simulink model "Controller_torque_cbf_m22"  (R2022b)
settings: Solver=ode4  StartTime=0.0  StopTime=Inf  FixedStep=1e-3  RelTol=1e-3
values from neighbouring files (symbols this model uses):
  Dn = 20 * ones(7,1)    [init_torque_cbf.m]
  H_0_cy = H_0_pr * H_pr_cy    [init_torque_cbf.m]
  H_home = getTransform(Franka_robot, q_home, 'panda_link8', 'panda_link0')    [init_torque_cbf.m]
  Kn = 0 * ones(7,1)    [init_torque_cbf.m]
  q_home = q_init    [init_torque_cbf.m]
  q_init = [0 0  0  -(2/4)*pi  0  pi/2  -pi/4]'    [init_torque_cbf.m]
undefined symbols (not defined in the file or in its folder): cbf_torque_params, DiscIntNeverNeededParam, Fext_mag, T_final, X, Y, Z
libraries: sm_lib x162, nesl_utility x44, matrix_library x3, Robotics_lib x1
(part 11 of 12)

== matlab function Controller_torque_cbf_m22/Dynamic Parameters/Coriolis Matrix1 ==
  data: q_state input; C output; q_state_dot input
function C = Franka_CoriolisMatrix(q_state, q_state_dot)
% Author: TU Wien, ACIN Robotics group
% Optimized and generated from Maple
  C = zeros(7,7);

  t1877 = q_state(2);
  t1856 = sin(t1877);
  t3747 = 0.1e1 * t1856;
  t1878 = q_state(1);
  t1864 = cos(t1878);
  t2794 = 0.1225946e1 * t1864;
  t1875 = q_state(4);
  t1861 = cos(t1875);
  t1801 = 0.345563e0 * t1861;
  t1874 = q_state(5);
  t1853 = sin(t1874);
  t1860 = cos(t1874);
  t2249 = 0.41065e-1 * t1853 + 0.11953e-1 * t1860;
  t1522 = t2249 + 0.825e-1;
  t1854 = sin(t1875);
  t3244 = t1522 * t1854;
  t1128 = t1801 - t3244;
  t1101 = 0.316e0 + t1128;
  t1863 = cos(t1877);
  t2864 = 0.41065e-1 * t1860;
  t1538 = 0.11953e-1 * t1853 - t2864;
  t1876 = q_state(3);
  t1855 = sin(t1876);
  t1370 = t1538 * t1855;
  t1797 = 0.345563e0 * t1854;
  t2889 = -t1797 + 0.825e-1;
  t3243 = t1522 * t1861;
  t1104 = -t3243 + t2889;
  t1862 = cos(t1876);
  t3688 = t1104 * t1862;
  t3541 = t3688 + t1370;
  t3413 = t1856 * t3541;
  t604 = -t1101 * t1863 + t3413;
  t3746 = t2794 * t604;
  t1857 = sin(t1878);
  t1873 = q_state(6);
  t1852 = sin(t1873);
  t1859 = cos(t1873);
  t1312 = 0.60149000000000000000e-1 * t1859 + 0.14117000000000000000e-1 * t1852;
  t1010 = -t1312 * t1853 - 0.10517000000000000000e-1 * t1860;
  t1537 = 0.60149e-1 * t1852 - 0.14117e-1 * t1859;
  t1520 = t1537 + 0.384e0;
  t1329 = t1520 * t1854;
  t3484 = 0.825e-1 - t1329;
  t1541 = 0.60149e-1 * t1859 + 0.14117e-1 * t1852;
  t1809 = 0.10517e-1 * t1853;
  t2802 = -t1541 * t1860 + t1809;
  t3647 = t2802 + 0.825e-1;
  t3678 = t3647 * t1861;
  t847 = -t3678 + t3484;
  t3731 = t847 * t1862;
  t577 = t1010 * t1855 + t3731;
  t3745 = t1857 * t577;
  t1872 = q_state(7);
  t1858 = cos(t1872);
  t2521 = 0.12763550042100000000e-2 * t1858;
  t1851 = sin(t1872);
  t2596 = 0.51602752476000000000e-3 * t1851;
  t3101 = -t2596 - t2521;
  t2339 = -0.27219646194675000000e-1 + t3101;
  t2578 = 0.48418875570424600020e-2 * t1851;
  t1377 = 0.55042935974400000000e-3 + t2578;
  t2589 = 0.13614453378240000000e-2 * t1851;
  t1410 = 0.5826996021941340000e-3 - t2589;
  t1844 = t1858 ^ 2;
  t1622 = 0.15804348732630079999e-2 * t1844;
  t2146 = t1622 - t1410;
  t888 = t1377 * t1858 - t2146;
  t685 = t1853 * t888 - t2339;
  t3397 = t685 * t1852;
  t658 = t685 * t1859;
  t2866 = 0.10517e-1 * t1860;
  t2331 = t1541 * t1853 + t2866;
  t3627 = t2331 * t1855;
  t3637 = -t3731 + t3627;
  t3744 = t1856 * t3637;
  t3628 = t1863 * t3637;
  t1845 = t1859 ^ 2;
  t2577 = 0.66899306471351120000e-2 * t1851;
  t3094 = -0.21934364256329279998e-2 * t1858 - t2577;
  t1201 = t3094 * t1845;
  t2582 = 0.33449653235675560000e-2 * t1851;
  t3096 = -0.10967182128164639999e-2 * t1858 - t2582;
  t2101 = t1201 - t3096;
  t1646 = 0.59408523832320000000e-2 * t1851;
  t1729 = 0.24018735697920000000e-2 * t1858;
  t1283 = t1646 - t1729;
  t2587 = 0.15804348732630079999e-2 * t1851;
  t1383 = -0.27228906756480000000e-2 + t2587;
  t2524 = 0.11008587194880000000e-2 * t1858;
  t2576 = 0.96837751140849200040e-2 * t1851;
  t3136 = t1858 * t2576 - t1622;
  t826 = t1383 * t1851 + t2524 + t3136;
  t3718 = t1852 * t826 - t1283;
  t3398 = t1859 * t3718;
  t3743 = (t2101 - t3398) * t1860;
  t1846 = t1860 ^ 2;
  t2603 = 0.24890000000000000000e-2 * t1844;
  t3212 = t1851 * t1858;
  t2104 = t2603 + 0.85600000000000000000e-3 * t3212;
  t1041 = 0.27050000000000000000e-2 - t2104;
  t1040 = t2104 + 0.28220000000000000000e-2;
  t3353 = t1040 * t1845;
  t2282 = -t3353 + t1041;
  t2588 = 0.14820000000000000000e-2 * t1851;
  t1384 = -0.21800000000000000000e-3 + t2588;
  t1730 = 0.23920000000000000000e-2 * t1858;
  t1142 = t1384 - t1730;
  t3208 = t1852 * t1859;
  t3002 = t1142 * t3208;
  t560 = t3002 - t2282;
  t3401 = t560 * t1846;
  t3604 = t2603 + 0.85599999999999999997e-3 * t3212;
  t1042 = 0.28220000000000000000e-2 + t3604;
  t2382 = 0.17120000000000000000e-2 * t3212;
  t2601 = 0.49780000000000000000e-2 * t1844;
  t2102 = t2382 + t2601;
  t2346 = 0.33106000000000000000e-1 - t2102;
  t2007 = -t3002 - t2346;
  t562 = -t1042 * t1845 + t2007;
  t3570 = t562 - t3401;
  t3732 = t1855 * t847;
  t3736 = t1010 * t1862 - t3732;
  t3742 = t1864 * t3736;
  t3153 = t1864 * t1863;
  t3741 = t3153 * t3736;
  t3168 = t1860 * t1853;
  t3075 = -0.2e1 * t3168;
  t3739 = t3075 * t560;
  t3197 = t1854 * t1862;
  t2987 = t1853 * t3197;
  t2772 = t1860 * t2987;
  t3738 = t560 * t2772;
  t3193 = t1855 * t1854;
  t3010 = t1846 * t3193;
  t3737 = t560 * t3010;
  t3375 = t888 * t1859;
  t680 = -t1853 * t2339 + t888;
  t1620 = 0.17120000000000000000e-2 * t1844;
  t1837 = t1851 ^ 2;
  t2379 = 0.99560000000000000000e-2 * t3212;
  t2107 = 0.17120000000000000000e-2 * t1837 + t2379;
  t2898 = t1620 - t2107;
  t2520 = 0.14820000000000000000e-2 * t1858;
  t2585 = 0.23920000000000000000e-2 * t1851;
  t1308 = t2520 + t2585;
  t2998 = t1308 * t3208;
  t2754 = -t2998 + t2898;
  t1445 = 0.49780000000000000000e-2 * t3212;
  t994 = -t1445 - 0.85599999999999999997e-3 * t1837 + 0.85599999999999999997e-3 * t1844;
  t2330 = -t1845 * t994 + t2754;
  t1476 = t1852 * t1730;
  t1096 = t1852 * t2588 - t1476;
  t2106 = 0.49780000000000000000e-2 * t1837 - 0.34240000000000000000e-2 * t3212;
  t997 = -t2106 + t2601;
  t3638 = t1859 * t997 + t1096;
  t2605 = 0.85600000000000000000e-3 * t1844;
  t999 = -t1445 - 0.85600000000000000000e-3 * t1837 + t2605;
  t3366 = t999 * t1845;
  t548 = t999 + t2998 + t3366;
  t3700 = t548 * t1846;
  t3427 = -t3168 * t3638 - t3700;
  t3735 = -t3427 - t2330;
  t1162 = -t3096 + 0.18713819462921000000e-3;
  t3311 = t1162 * t1859;
  t1407 = 0.4841887557042460002e-2 * t1851 + 0.55042935974400000000e-3;
  t890 = -t1407 * t1858 + t2146;
  t3733 = -t1852 * t890 + t3311;
  t3726 = t826 * t1845;
  t991 = 0.15804348732630079999e-2 * t1837 + t3136;
  t3578 = t3726 + t991;
  t1657 = 0.12763550042100000000e-2 * t1851;
  t1311 = -t1657 + 0.51602752476000000000e-3 * t1858;
  t2336 = 0.11198654185125000000e-1 + t1311;
  t1056 = t2336 * t1853;
  t1700 = 0.11357396418885000000e-1 * t1852;
  t1393 = t1700 - 0.24178658687700000000e-2;
  t3305 = t2339 * t1859;
  t899 = t1393 - t3305;
  t859 = t899 * t1860;
  t3730 = t859 - t1056;
  t2328 = t1857 * t3541;
  t820 = t1863 * t3541;
  t3706 = t1329 + t3678;
  t3729 = t3706 * t1856;
  t1286 = 0.10967182128164640000e-2 * t1858 + t2582;
  t1192 = 0.187138194629210e-3 + t1286;
  t2579 = 0.48418875570424600000e-2 * t1851;
  t1378 = 0.55042935974400000000e-3 + t2579;
  t3257 = t1378 * t1858;
  t1621 = 0.15804348732630080000e-2 * t1844;
  t3705 = t1410 - t1621;
  t889 = t3257 + t3705;
  t3727 = t1852 * t889;
  t3728 = t1192 * t1859 + t3727;
  t1161 = t1286 + 0.18713819462921000000e-3;
  t3314 = t1161 * t1852;
  t3725 = t889 * t1859;
  t628 = t3725 - t3314 - 0.54375110533459400000e-2;
  t3480 = t3314 + 0.5437511053345940e-2;
  t633 = t3725 - t3480;
  t2592 = 0.79021743663150400000e-3 * t1851;
  t1385 = -0.13614453378240000000e-2 + t2592;
  t1734 = 0.55042935974400000000e-3 * t1858;
  t1447 = t1858 * t2579;
  t1623 = 0.79021743663150400000e-3 * t1844;
  t3130 = -t1447 + t1623;
  t2903 = t1734 - t3130;
  t828 = t1385 * t1851 + t2903;
  t779 = t828 * t1852;
  t2103 = t1445 - t1620;
  t1044 = 0.14600000000000000000e-2 - t2103;
  t3724 = t1044 * t1852;
  t3723 = t1044 * t1859;
  t3162 = t1861 * t1862;
  t1260 = t1538 * t3162;
  t2199 = t2249 * t1855;
  t2157 = t1260 + t2199;
  t3722 = t1856 * t2157;
  t3671 = -t1520 * t1861 + t1854 * t3647;
  t3721 = t1863 * t3671;
  t3720 = t3671 * t1856;
  t1648 = 0.29704261916160000000e-2 * t1851;
  t1379 = t1648 - 0.23898270415101870000e-1;
  t2522 = 0.12009367848960000000e-2 * t1858;
  t1160 = t2522 - t1379;
  t2532 = 0.54835910640823200000e-3 * t1858;
  t2586 = 0.16724826617837780000e-2 * t1851;
  t3097 = -t2586 - t2532;
  t1185 = -t3097 + 0.9356909731460500000e-4;
  t1089 = t1185 * t1859;
  t1380 = 0.24209437785212300000e-2 * t1851 + 0.27521467987200000000e-3;
  t1263 = t1380 * t1858;
  t1663 = 0.68072266891200000000e-3 * t1851;
  t1403 = 0.29134980109706700000e-3 - t1663;
  t882 = t1623 - t1403 - t1263;
  t3698 = t882 * t1852;
  t3707 = -t1089 + t3698;
  t2091 = t1160 - t3707;
  t1534 = -t2588 + 0.21800e-3;
  t1248 = t1730 + t1534;
  t2999 = t1248 * t3208;
  t575 = t2282 + t2999;
  t1658 = 0.12009367848960000000e-2 * t1851;
  t1727 = 0.29704261916160000000e-2 * t1858;
  t1295 = t1658 + t1727;
  t2518 = 0.15804348732630080000e-2 * t1858;
  t1449 = t1851 * t2518;
  t1617 = 0.24209437785212300000e-2 * t1844;
  t2530 = 0.68072266891200000000e-3 * t1858;
  t2135 = t2530 - t1617;
  t3256 = t1380 * t1851;
  t830 = t1449 - t3256 - t2135;
  t3699 = t830 * t1852;
  t2848 = t1295 - t3699;
  t1732 = 0.16724826617837780000e-2 * t1858;
  t2595 = 0.54835910640823200000e-3 * t1851;
  t3100 = -t2595 + t1732;
  t3269 = t3100 * t1859;
  t3596 = t2848 - t3269;
  t2863 = 0.61597e-1 * t1860;
  t1562 = t1852 * t2863;
  t2887 = 0.4252e-2 * t1851;
  t1544 = 0.10517e-1 * t1858 + t2887;
  t1524 = t1544 + 0.88e-1;
  t3173 = t1859 * t1860;
  t3031 = t1524 * t3173;
  t3116 = -t1562 - t3031;
  t1543 = 0.10517e-1 * t1851 - 0.4252e-2 * t1858;
  t3230 = t1543 * t1853;
  t844 = -0.825e-1 + t3230 - t3116;
  t3385 = t844 * t1854;
  t3241 = t1524 * t1852;
  t2867 = 0.61597e-1 * t1859;
  t3646 = 0.384e0 - t2867;
  t3620 = t3241 + t3646;
  t3682 = t3620 * t1861;
  t3719 = t3682 + t3385;
  t1660 = 0.10967182128164640000e-2 * t1851;
  t2512 = 0.33449653235675560000e-2 * t1858;
  t2127 = t2512 - t1660;
  t1154 = t2127 + 0.11022068765350630000e-1;
  t3166 = t1860 * t1861;
  t1598 = 0.13297872941088000000e-4 * t1837;
  t1733 = 0.13614453378240000000e-2 * t1858;
  t1664 = 0.55042935974400000000e-3 * t1851;
  t2465 = t1664 + 0.69751885789075550000e-2;
  t2258 = t1733 + 0.81354094419858e-4 * t1844 + t2465;
  t911 = t1598 + t2258;
  t609 = t1154 * t3166 - t1854 * t911;
  t3036 = t1286 * t3208;
  t3358 = t1845 * t828 - t3036;
  t1376 = 0.11008587194880000000e-2 + t2576;
  t1270 = t1376 * t1858;
  t1615 = 0.31608697465260159998e-2 * t1844;
  t1650 = 0.27228906756480000000e-2 * t1851;
  t3108 = t1615 + t1650;
  t881 = t3108 - t1270 - 0.11653992043882680000e-2;
  t3377 = t881 * t1859;
  t3717 = t3377 + 0.10875022106691880000e-1;
  t1085 = t2339 * t1852;
  t3716 = 0.1e1 * t1085;
  t3715 = 0.1e1 * t3162;
  t3714 = 0.1e1 * t3723;
  t3713 = t1852 * t881;
  t2885 = 0.5317e-1 * t1854;
  t1790 = -0.316e0 + t2885;
  t2837 = 0.104419e0 * t1861;
  t2845 = 0.104419e0 * t1854;
  t2248 = 0.5317e-1 * t1861 + t2845;
  t1523 = t2248 - 0.825e-1;
  t2870 = 0.27454e-1 * t1855;
  t1134 = t1523 * t1862 - t2870;
  t3635 = t1134 * t1863;
  t824 = t3635 + t1856 * (t1790 - t2837);
  t3712 = t1857 * t824;
  t3711 = t1864 * t824;
  t3384 = t844 * t1861;
  t2048 = t2867 - t3241;
  t2014 = 0.384e0 - t2048;
  t3710 = t1854 * t2014;
  t3709 = t1863 * t3682;
  t3237 = t1538 * t1862;
  t3689 = t1104 * t1855;
  t2652 = t3237 - t3689;
  t2326 = t2652 * t1864;
  t1088 = t1185 * t1852;
  t3696 = t882 * t1859;
  t3708 = -t1088 - t3696;
  t1194 = t1286 * t1845;
  t2806 = -t3097 - t1194;
  t1302 = -t1648 + t2522;
  t668 = t1302 + t779;
  t480 = t1859 * t668 - t2806;
  t3271 = t3100 * t1852;
  t3575 = t1859 * t830;
  t3567 = t3271 - t3575;
  t1303 = -0.41065000000000000000e-1 * t1860 + 0.11953000000000000000e-1 * t1853;
  t787 = t1303 * t1855 + t3688;
  t2381 = 0.24890000000000000000e-2 * t3212;
  t2105 = t2381 - t2605;
  t3642 = t2105 - 0.73000000000000000000e-3;
  t3355 = t3642 * t1852;
  t3704 = 0.22900e-3 - t3355;
  t1832 = 0.316e0 * t1856;
  t3703 = t1856 * t3682 + t1832;
  t3702 = 0.1e1 * t3698;
  t1736 = 0.25801376238000000000e-3 * t1858;
  t2594 = 0.63817750210500000000e-3 * t1851;
  t3099 = t1736 - t2594;
  t1197 = t3099 * t1854;
  t3701 = 0.1e1 * t1197;
  t3379 = t1860 * t882;
  t1503 = t1859 * t2520;
  t1532 = 0.68200e-3 + t2585;
  t3123 = t1532 * t1859 + t1503;
  t725 = t3123 - t3724;
  t688 = t725 * t3168;
  t3381 = t882 * t1853;
  t3697 = t882 * t1855;
  t3695 = t882 * t1862;
  t3169 = t1860 * t1852;
  t3694 = t882 * t3169;
  t3172 = t1859 * t1861;
  t3693 = t882 * t3172;
  t3207 = t1852 * t1861;
  t3692 = t882 * t3207;
  t1806 = 0.61597e-1 * t1852;
  t1554 = t1853 * t1806;
  t3229 = t1543 * t1860;
  t3140 = t3229 - t1554;
  t3202 = t1853 * t1859;
  t2441 = -t1524 * t3202 + t3140;
  t3662 = t2441 * t1855;
  t1280 = 0.10517000000000000000e-1 * t1851 - 0.42520000000000000000e-2 * t1858;
  t1202 = t1280 * t1853;
  t1306 = 0.10517000000000000000e-1 * t1858 + 0.42520000000000000000e-2 * t1851;
  t1173 = t1306 + 0.88000000000000000000e-1;
  t3046 = t1173 * t3173;
  t3150 = -t3046 - t1202;
  t2333 = 0.82500000000000000000e-1 + t3150;
  t2265 = -t1562 + t2333;
  t663 = t2265 * t1861;
  t1082 = t1173 * t1852;
  t2466 = t1082 + 0.38400000000000000000e0;
  t918 = -t2867 + t2466;
  t879 = t918 * t1854;
  t871 = -0.825e-1 + t879;
  t469 = t663 + t871;
  t377 = t1862 * t469 - t3662;
  t2737 = t1082 + t3646;
  t482 = t1854 * t2737 + t663 - 0.825e-1;
  t384 = t1862 * t482 - t3662;
  t3157 = t1863 * t1862;
  t3687 = t1128 * t3157;
  t3183 = t1856 * t1862;
  t3686 = t1128 * t3183;
  t3260 = t1311 * t1852;
  t1035 = t1854 * t3620;
  t2591 = 0.98827089590400000000e-3 * t1851;
  t1404 = -0.52129746651620000000e-1 - t2591;
  t2515 = 0.24444132201840000000e-2 * t1858;
  t3615 = t1404 - t2515;
  t3649 = -0.56786982094425000000e-2 * t1860 + t3615;
  t3685 = t1854 * t3649;
  t3194 = t1855 * t1853;
  t3191 = t1855 * t1860;
  t3240 = t1524 * t1859;
  t3516 = t1806 + t3240;
  t1972 = t1853 * t3516 - t3229;
  t3684 = t1972 * t1855;
  t3683 = t1972 * t1862;
  t3187 = t1856 * t1854;
  t3681 = t3620 * t3187;
  t3679 = t3642 * t1859;
  t1843 = t1857 ^ 2;
  t1850 = t1864 ^ 2;
  t3515 = t1850 + t1843;
  t2529 = 0.74100000000000000000e-3 * t1858;
  t2590 = 0.11960000000000000000e-2 * t1851;
  t2132 = t2529 + t2590;
  t3677 = -t3208 * t999 - t2132;
  t1596 = 0.81354094419858000000e-4 * t1837;
  t1838 = t1852 ^ 2;
  t1607 = 0.11947109539798930000e-2 * t1838;
  t3608 = t1607 - t1596;
  t2344 = 0.25565950283854690000e-2 + t3608;
  t1451 = t1858 * t2592;
  t3526 = t1451 + 0.25022978729410880000e-2 * t1844;
  t858 = t2344 - t3526;
  t2598 = 0.25801376238000000000e-3 * t1851;
  t1402 = 0.13609823097337500000e-1 + t2598;
  t2531 = 0.63817750210500000000e-3 * t1858;
  t2340 = -t2531 - t1402;
  t2583 = 0.31608697465260159998e-2 * t1851;
  t1448 = t1858 * t2583;
  t3134 = t1448 - t1733;
  t3676 = -0.4841887557042460002e-2 * t1844 - t3134;
  t1611 = 0.48418875570424600020e-2 * t1844;
  t2439 = -t1377 * t1851 + t1611 + t3134;
  t1540 = 0.39252e-1 * t1862 + 0.27518e-1 * t1855;
  t3236 = t1540 * t1857;
  t2247 = 0.39252e-1 * t1855 - 0.27518e-1 * t1862;
  t3583 = -t1863 * t2247 + 0.249498e0 * t1856;
  t3346 = t3583 * t1864;
  t3675 = -t3236 + t3346;
  t1156 = 0.47796540830203740000e-1 - t1283;
  t1065 = t1156 * t1853;
  t2467 = t1065 + 0.27752814537092170000e0;
  t965 = -t1162 * t1853 + 0.11357396418885000000e-1;
  t3409 = t1859 * t965;
  t3674 = t3409 - t2467;
  t3661 = t2441 * t1862;
  t383 = t1855 * t482 + t3661;
  t376 = t1855 * t469 + t3661;
  t3673 = (-0.1e1 * t2605 + t2381) * t1862;
  t3672 = -0.1e1 * t1850 - 0.1e1 * t1843;
  t2593 = 0.79021743663150399997e-3 * t1851;
  t1386 = -0.13614453378240000000e-2 + t2593;
  t3035 = t3096 * t3208;
  t1446 = t1858 * t2578;
  t1624 = 0.79021743663150399997e-3 * t1844;
  t3135 = t1446 - t1624;
  t3362 = -(t1386 * t1851 + t1734 + t3135) * t1845 - t3035;
  t2345 = -0.48082828567067140000e-2 - t3608;
  t3670 = 0.1e1 * t2898;
  t3669 = t1861 - 0.1e1;
  t2511 = 0.47840000000000000000e-2 * t1858;
  t2584 = 0.29640000000000000000e-2 * t1851;
  t2125 = t2511 - t2584;
  t1247 = t2125 + 0.43600e-3;
  t1125 = t1247 * t1845;
  t1530 = -0.829200e-2 + t2588;
  t1045 = t2102 + 0.5644000000000000000e-2;
  t3003 = t1045 * t3208;
  t631 = t1530 - t1730 + t1125 + t3003;
  t3668 = t631 * t1853;
  t3666 = t965 * t1852;
  t3091 = -0.60149000000000000000e-1 * t1852 + 0.14117000000000000000e-1 * t1859;
  t2335 = -0.38400000000000000000e0 + t3091;
  t1208 = t1312 * t1860;
  t2562 = 0.10517000000000000000e-1 * t1853;
  t2229 = t2562 - t1208;
  t2348 = -0.82500000000000000000e-1 - t2229;
  t673 = t1854 * t2335 + t1861 * t2348 + 0.825e-1;
  t519 = t1862 * t673 - t3627;
  t2736 = -0.384e0 + t3091;
  t971 = -0.825e-1 - t2229;
  t3369 = t971 * t1861;
  t718 = t1854 * t2736 + t3369 + 0.825e-1;
  t540 = t1862 * t718 - t3627;
  t3190 = t1855 * t1861;
  t3007 = t1846 * t3190;
  t3343 = t1855 * t2802;
  t3665 = t1856 * t2248;
  t1390 = -t1658 - 0.63347540234880000000e-1;
  t3616 = t1390 - t1727;
  t3664 = t1860 * t3616;
  t3663 = t2048 * t3194;
  t2170 = 0.56786982094425000000e-2 * t1852 - 0.12089329343850000000e-2;
  t3248 = t2170 * t1854;
  t2198 = t2249 * t1862;
  t2470 = 0.16143020000000000000e1 * t1864;
  t3585 = t1856 * t2247 + 0.249498e0 * t1863;
  t3660 = t2470 * t3585;
  t1839 = t1853 ^ 2;
  t2611 = 0.79021743663150400000e-3 * t1837;
  t2306 = -t1623 + t2611;
  t993 = t1447 + t2306;
  t3498 = -t1845 * t993 + t3036;
  t3659 = t3498 * t1839;
  t3658 = (t1543 * t1855 + t3162 * t3516) * t1853;
  t3560 = t3583 * t1857;
  t937 = t3585 * t1857;
  t3001 = t1154 * t3208;
  t2722 = t858 + t3001;
  t1619 = 0.24076459055801420000e-2 * t1844;
  t3113 = t1598 - t1619;
  t3251 = t1385 * t1858;
  t801 = -t3251 + t2465 + t3113;
  t3598 = t1845 * t801 + t2722;
  t3657 = t3598 * t1853;
  t1652 = 0.24444132201840000000e-2 * t1851;
  t2527 = 0.98827089590400000000e-3 * t1858;
  t3600 = -t2527 + t1652;
  t2088 = t3600 * t1854;
  t3137 = t3600 * t1855;
  t3281 = t3600 * t1861;
  t1198 = t3099 * t1861;
  t3655 = -t1198 + t1311;
  t1300 = t2531 + t2598;
  t490 = t993 + t3358;
  t3654 = t1853 * t490 + t1300;
  t1482 = 0.23894219079597860000e-2 * t3208;
  t3222 = t1845 * t1154;
  t3228 = t1838 * t1154;
  t2815 = t3222 - t3228;
  t2679 = -t1482 - t2815;
  t1381 = 0.68200000000000000000e-3 + t2585;
  t3255 = t1381 * t1859;
  t3653 = t1503 + t3255;
  t1369 = -0.24972970685027959000e-1 - t1596;
  t1788 = 0.13297872941088e-4 * t1844;
  t1132 = t1788 - t1369;
  t1189 = 0.11022068765350630e-1 + t2127;
  t1699 = 0.26431758938496000000e-1 * t1852;
  t3650 = t1189 * t1845 - 0.4484246605646421e-2 - t1699 - t3100;
  t3626 = t2331 * t1862;
  t541 = t1855 * t718 + t3626;
  t520 = t1855 * t673 + t3626;
  t3648 = -0.1e1 * t1837 + t1844;
  t1477 = t1852 * t2520;
  t3239 = t1532 * t1852;
  t3126 = -t1477 - t3239;
  t3645 = t3126 - 0.15700e-2;
  t3204 = t1853 * t1852;
  t2377 = 0.17120000000000000000e-2 * t3204;
  t1337 = t1844 * t2377;
  t2375 = 0.49780000000000000000e-2 * t3204;
  t3144 = -t2375 * t3212 + t1337;
  t3644 = 0.155920e-1 - t3144;
  t1046 = t2102 - 0.5410000000000000000e-2;
  t3643 = 0.13611244295754000000e-3 * t1851;
  t2503 = 0.52863517876992000000e-1 * t1859;
  t1157 = 0.44842466056464210000e-2 + t3100;
  t1075 = t1157 * t1861;
  t2556 = 0.12089329343850000000e-2 * t1854;
  t3088 = -t2556 - t1075;
  t897 = -0.46305794820080000000e-2 - t3088;
  t1293 = -t1730 + t2588;
  t1176 = 0.82920000000000000000e-2 - t1293;
  t2341 = -0.21447119530300000000e-1 + t3600;
  t3641 = -0.2e1 * t1860;
  t3639 = t631 * t1860;
  t3636 = t1134 * t1856;
  t2385 = t1858 * t3643;
  t3634 = t1854 * t3516;
  t3192 = t1855 * t1859;
  t3633 = t1855 * t3516;
  t2056 = t1856 * t2802;
  t1662 = 0.74100000000000000000e-3 * t1851;
  t2523 = 0.11960000000000000000e-2 * t1858;
  t2131 = -t2523 + t1662;
  t3630 = t1859 * t2131;
  t3160 = t1863 * t1854;
  t3625 = t2331 * t3160;
  t3624 = t2331 * t3162;
  t3041 = t2331 * t3187;
  t1526 = 0.825e-1 - t1562;
  t707 = t1526 + t3150;
  t3408 = t1861 * t707;
  t3622 = (t871 + t3408) * t1862;
  t1661 = 0.10967182128164639999e-2 * t1851;
  t2612 = -t2512 - 0.8968493211292842000e-2;
  t1186 = t1661 + t2612;
  t1697 = 0.52863517876992000000e-1 * t1852;
  t3621 = t1186 - t1697;
  t1653 = 0.24018735697920000000e-2 * t1851;
  t1725 = 0.59408523832320000000e-2 * t1858;
  t1289 = t1653 + t1725;
  t2128 = t2512 - t1661;
  t3619 = -t1859 * t2128 + t1289;
  t1822 = 0.27454e-1 * t1862;
  t1559 = t1857 * t1822;
  t2485 = 0.53170000000000000000e-1 * t1861;
  t3181 = t1857 * t1855;
  t3618 = t2485 * t3181 + t1559;
  t2550 = 0.82500000000000000000e-1 * t1854;
  t1399 = 0.38400000000000000000e0 - t2550;
  t2747 = 0.7735484874e-2 * t1858;
  t3617 = -t1399 * t2747 + t1390;
  t1450 = t1858 * t2587;
  t3614 = -t1450 - t1611;
  t3613 = 0.81354094419858e-4 * t1837 - t3001 + t3526 - 0.25565950283854690000e-2;
  t1153 = t2128 + 0.11022068765350630000e-1;
  t1021 = t1153 * t3208;
  t1452 = t1858 * t2593;
  t3612 = -t1452 - 0.25022978729410880010e-2 * t1844 + t1021;
  t3611 = t1452 + 0.24209437785212300010e-2 * t1844;
  t3610 = -t3724 + t3653;
  t2477 = 0.53170000000000000000e-1 * t1864;
  t2890 = 0.825e-1 * t1864;
  t3609 = t1862 * t2890 - t2477 * t3162;
  t3102 = t1664 + t1733;
  t1612 = 0.48418875570424600000e-2 * t1844;
  t3607 = t1733 - t1612;
  t1777 = 0.12089329343850000000e-2 * t1861;
  t2554 = 0.46305794820080000000e-2 * t1854;
  t3606 = -t1777 - t2554;
  t1272 = t1402 * t1854;
  t1396 = -0.31600000000000000000e0 + t2550;
  t2040 = -t1396 * t2747 - t1404;
  t3605 = t2040 - t1272;
  t3128 = -0.96837751140849200000e-2 * t3212 + t1621;
  t2471 = 0.83327750000000000000e0 * t1864;
  t2537 = 0.83327750000000000000e0 * t1857;
  t594 = -t3626 - t3732;
  t3412 = t1857 * t594;
  t3184 = t1856 * t1861;
  t3146 = t1520 * t3184 + t1832;
  t2911 = -t3187 * t3647 + t3146;
  t421 = t2911 - t3628;
  t294 = t1864 * t421 + t3412;
  t3406 = t1864 * t594;
  t422 = -t1832 + t3628 + t3720;
  t297 = t1857 * t422 + t3406;
  t3603 = t2471 * t297 + t2537 * t294;
  t1588 = t1855 * t2890;
  t3180 = t1857 * t1856;
  t2251 = -t3662 + t3622;
  t357 = t2251 * t1857;
  t3156 = t1864 * t1855;
  t502 = t3156 * t707 - t3180 * t3620;
  t3395 = t707 * t1854;
  t664 = -0.316e0 + t3395;
  t169 = t664 * t3180 + t1861 * t502 + t1863 * t357 - t1588 + (t3193 * t918 + t3661) * t1864;
  t2895 = 0.825e-1 * t1855;
  t1582 = t1857 * t2895;
  t2985 = t1854 * t3181;
  t3155 = t1864 * t1856;
  t2888 = 0.825e-1 - t1035;
  t3047 = t1173 * t3202;
  t748 = -t3047 + t3140;
  t730 = t748 * t1855;
  t2733 = t1862 * t2888 + t3162 * t844 + t730;
  t395 = t2733 * t1864;
  t568 = t3155 * t3620 - t3181 * t844;
  t3179 = t1857 * t1862;
  t714 = t748 * t3179;
  t770 = 0.316e0 + t3385;
  t181 = t1861 * t568 + t1863 * t395 + t2985 * t3620 + t3155 * t770 - t1582 + t714;
  t2475 = 0.36776100000000000000e0 * t1864;
  t2541 = 0.36776100000000000000e0 * t1857;
  t3602 = t169 * t2475 + t181 * t2541;
  t1002 = -t1162 + 0.11357396418885000000e-1 * t1853;
  t2566 = 0.24178658687700000000e-2 * t1853;
  t823 = -t2566 + t1002 * t1852 - 0.13248221105898140000e-1;
  t3098 = -t2589 + t1734;
  t1301 = -t2591 - t2515;
  t2749 = 0.7735484874e-2 * t1851;
  t3599 = t1396 * t2749 + t2527;
  t1834 = 0.316e0 * t1863;
  t2833 = 0.345563e0 * t1863;
  t3117 = t1861 * t2833 + t1834;
  t1971 = t1860 * t3516 + t3230;
  t1966 = 0.825e-1 - t1971;
  t1938 = t1854 * t1966 - t1861 * t2014;
  t2876 = -0.735522e0 * t1834 + 0.735522e0 * t1938 * t1863 + 0.735522e0 * (-t3684 + (0.825e-1 - t3710 + (-0.825e-1 + t1971) * t1861) * t1862) * t1856;
  t3506 = t3515 * t2876;
  t3323 = t1153 * t1845;
  t2812 = t1153 * t1838 - t3323;
  t3597 = t2812 - t1482;
  t2508 = 0.66899306471351120000e-2 * t1858;
  t1290 = 0.21934364256329279998e-2 * t1851 - t2508;
  t1150 = -t1290 + 0.22044137530701260000e-1;
  t3326 = t1150 * t1845;
  t3593 = t3326 - t1697;
  t3333 = t1142 * t1845;
  t3494 = t1142 * t1838 - t3333;
  t1776 = 0.46305794820080000000e-2 * t1861;
  t3592 = t1776 - 0.44842466056464210000e-2 - t2556;
  t3591 = -t1797 - 0.1e1 * t3243;
  t3590 = t3673 * t1853;
  t3221 = t1845 * t1853;
  t3354 = t1040 * t1838;
  t3589 = t1040 * t3221 - 0.1e1 * t1853 * t3354;
  t3588 = -0.1e1 * t971 * t1854 + t2736 * t1861;
  t3090 = -0.41065000000000000000e-1 * t1853 - 0.11953000000000000000e-1 * t1860;
  t2738 = -0.825e-1 + t3090;
  t3587 = -0.1e1 * t2738 * t1854 - 0.1e1 * t1801;
  t2894 = 0.825e-1 * t1861;
  t1792 = 0.825e-1 - t2894;
  t2210 = 0.41065e-1 * t3162 - 0.11953e-1 * t1855;
  t2842 = 0.345563e0 * t1856;
  t2693 = t1862 * t2842;
  t2727 = 0.11953e-1 * t3162;
  t2892 = 0.825e-1 * t1863;
  t2741 = t1854 * t2892;
  t3185 = t1856 * t1860;
  t3186 = t1856 * t1855;
  t3203 = t1853 * t1856;
  t418 = -t1792 * t3183 + t1854 * t2693 + t2210 * t3203 - t2249 * t3160 + t2727 * t3185 + t2864 * t3186 - t2741 + t3117;
  t3487 = 0.1225946e1 * t3672 * t418;
  t276 = -t1834 + t3721 - t3744;
  t3486 = 0.1666555e1 * t3672 * t276;
  t3586 = t1450 + 0.16270818883971600000e-3 * t1837 - 0.23894219079597860000e-2 * t1838;
  t2803 = t1523 * t1855 + t1822;
  t2417 = t1134 * t1857 + t2803 * t3153;
  t2413 = t1543 * t3173 - t1544 * t1853;
  t3209 = t1852 * t1854;
  t3022 = t1543 * t3209;
  t3584 = t1861 * t2413 - t3022;
  t3581 = 0.9457555763200000000e-3 - t1451;
  t1539 = -t2837 + t2885;
  t3023 = t1539 * t3157;
  t3580 = (-0.1e1 * t3665 + t3023) * t1864 - 0.1e1 * t1539 * t3181;
  t3463 = 0.2e1 * t1852;
  t3579 = t1845 / 0.2e1;
  t3312 = t1162 * t1852;
  t2664 = t3312 - t3375;
  t627 = t2664 + 0.54375110533459400000e-2;
  t3577 = t1846 * t627;
  t850 = t1280 * t3173 - t1306 * t1853;
  t3576 = t1854 * t850;
  t2469 = 0.17939475000000000000e1 * t1864;
  t1521 = t1539 - 0.316e0;
  t868 = t1521 * t1863 - t3636;
  t2395 = t868 * t2469;
  t3092 = -t1700 + t3305;
  t900 = 0.24178658687700000000e-2 + t3092;
  t3574 = t900 * t1853;
  t1992 = t997 * t1852;
  t998 = -0.24890000000000000000e-2 * t1837 + t2382 + t2603;
  t3573 = t998 * t1852;
  t3572 = t1648 - t779;
  t3072 = t575 * t3168;
  t2854 = t1477 + 0.42340e-2;
  t996 = t3239 + t2854;
  t716 = t3723 + t996;
  t696 = t716 * t1846;
  t3571 = -t3072 + t696;
  t976 = t1088 + 0.6624110552949070e-2;
  t3569 = t1846 * t633 + t976;
  t1166 = -0.12669508046976000000e0 - t1289;
  t1656 = 0.15804348732630080000e-2 * t1851;
  t1382 = t1656 - 0.27228906756480000000e-2;
  t1597 = 0.26595745882176000000e-4 * t1837;
  t1659 = 0.11008587194880000000e-2 * t1851;
  t3110 = -t1597 - t1659;
  t796 = 0.48152918111602840000e-2 * t1844 + t1382 * t1858 - 0.11560955249855324000e-1 + t3110;
  t636 = t1852 * t796 + t1166;
  t3568 = t1859 * t636 - t1697;
  t2373 = t1852 * t2529;
  t3562 = t3679 - t2373;
  t3084 = t1839 - t1846;
  t3561 = t1044 * t3084;
  t1716 = 0.56786982094425000000e-2 * t1854;
  t2461 = t1716 - 0.21751134959804000000e-1;
  t2486 = 0.26431758938496000000e-1 * t1861;
  t1168 = t2486 - t2461;
  t3559 = t1168 * t1852;
  t2147 = t1524 * t1854;
  t2883 = 0.4252e-2 * t1860;
  t3557 = t1851 * (t1809 * t1859 + t2883);
  t2862 = 0.14117e-1 * t1861;
  t2873 = 0.60149e-1 * t1854;
  t3556 = t1852 * (t1860 * t2873 - t2862);
  t3199 = t1854 * t1853;
  t3555 = t1855 * t2248;
  t2886 = 0.4252e-2 * t1853;
  t3554 = t1858 * (t1859 * t2886 - t2866);
  t3174 = t1859 * t1854;
  t2861 = 0.60149e-1 * t1861;
  t2874 = 0.14117e-1 * t1854;
  t3553 = t1859 * (t1860 * t2874 + t2861);
  t1987 = t1851 * (t1859 * t2866 - t2886) - t1858 * (t1859 * t2883 + t1809);
  t3552 = t1861 * t1987;
  t2238 = -0.825e-1 + t2485;
  t2117 = t2238 + t2845;
  t3551 = t1862 * t2117;
  t1545 = 0.2872e-1 * t1856 - 0.3141e-2 * t1863;
  t1939 = t1861 * t1966 + t3710;
  t165 = -t1832 + t1938 * t1856 + (t3684 + (-0.825e-1 + t1939) * t1862) * t1863;
  t1870 = q_state_dot(2);
  t2800 = 0.3228604e1 * t3583;
  t2826 = 0.3587895e1 * t1539 * t1856 - 0.3587895e1 * t1832 + 0.3587895e1 * t3635;
  t2041 = t1797 + t3243;
  t2242 = t1128 * t1856;
  t2829 = -0.1225946e1 * t1832 - 0.1225946e1 * t2242 + 0.1225946e1 * (-0.1e1 * t1370 + (-0.825e-1 + t2041) * t1862) * t1863;
  t2831 = -0.1666555e1 * t1832 + 0.1666555e1 * t3720 + 0.1666555e1 * (t3627 + (t3678 - 0.1e1 * t3484) * t1862) * t1863;
  t2834 = 0.104419e0 * t1863;
  t1552 = t1861 * t2834;
  t2881 = 0.5317e-1 * t1863;
  t689 = t1854 * t2881 - t1552 - t1834 - t3636;
  t3550 = (t3585 * t2800 + 0.646926e0 * t1545 * (0.2872e-1 * t1863 + 0.3141e-2 * t1856) + t165 * t2876 + t276 * t2831 + t2826 * t689 - t2829 * t418) * t1870;
  t2067 = t2103 * t1852;
  t2137 = t2170 * t1862;
  t1408 = 0.9356909731460500000e-4 + t2586;
  t2308 = t1408 + t2532;
  t3548 = t2308 * t1859;
  t3167 = t1860 * t1854;
  t3029 = t1537 * t3167;
  t3233 = t1541 * t1861;
  t2414 = t3029 - t3233;
  t3545 = t2414 * t1856;
  t3028 = t1537 * t3166;
  t3235 = t1541 * t1854;
  t2415 = t3028 + t3235;
  t3544 = t2415 * t1862;
  t1049 = t2803 * t1864;
  t3523 = t1699 + t1157;
  t2818 = t3523 - t3222;
  t1145 = t1300 + 0.13609823097337500000e-1;
  t2495 = 0.26431758938496000000e-1 * t1860;
  t1003 = t1145 + t2495;
  t1004 = 0.21751134959804000000e-1 * t1860 + t2340;
  t3542 = t1004 * t1861 + t1003;
  t1057 = t2336 * t1860;
  t3372 = t899 * t1853;
  t3540 = -t1057 - t3372;
  t1060 = t3616 * t1854;
  t3330 = t1145 * t1861;
  t3539 = -t1060 + t3330;
  t1112 = t1311 * t3173;
  t1205 = t3101 * t1853;
  t3538 = t1112 - t1205;
  t1070 = t1145 * t1854;
  t1155 = -t1301 + 0.52129746651620000000e-1;
  t3536 = -t1155 + t1070;
  t1207 = t1302 * t1854;
  t3535 = -t1198 - t1207;
  t2908 = -t1198 + t3099;
  t2570 = 0.61597000000000000000e-1 * t1852;
  t1510 = t1860 * t2570;
  t3534 = t1510 - t3150;
  t3531 = -t1852 * t2439 + t3619;
  t2334 = -0.82500000000000000000e-1 + t3090;
  t952 = t1861 * t2334 + t2889;
  t760 = t1862 * t952 + t1370;
  t1411 = -0.2913498010970670000e-3 + t1663;
  t2641 = 0.7902174366315040000e-3 * t1844;
  t3528 = -t1411 - t2641;
  t3121 = t1393 * t1860;
  t3524 = t1619 + t3251;
  t3104 = 0.25527100084200000000e-2 * t1851 - 0.10320550495200000000e-2 * t1858;
  t1359 = 0.2444413220184e-2 * t1862 - 0.54835910640823200000e-3 * t1855;
  t1771 = 0.11357396418885000000e-1 * t1859;
  t3520 = t1771 + t1085;
  t1782 = 0.21751134959804000000e-1 * t1862;
  t3519 = -t1782 + t3697;
  t1361 = -0.16724826617837780000e-2 * t1862 - 0.988270895904e-3 * t1855;
  t2090 = t1853 * t3091;
  t2255 = t2415 * t1855;
  t3514 = -t1862 * t2090 + t2255;
  t2600 = 0.50045957458821760020e-2 * t1844;
  t2126 = -0.21934364256329279999e-2 * t1851 + t2508;
  t1151 = t2126 + 0.22044137530701260000e-1;
  t3051 = t1151 * t3208;
  t1613 = 0.48152918111602840020e-2 * t1844;
  t3114 = t1597 - t1613;
  t3253 = t1383 * t1858;
  t2753 = t1659 - t3253 + t3114;
  t805 = 0.13950377157815110002e-1 + t2753;
  t3513 = t1845 * t805 - t2600 + t3051 - t3586;
  t2484 = 0.49096519673609460000e-2 * t1862;
  t2350 = t1861 * t2484;
  t2565 = 0.49096519673609460000e-2 * t1853;
  t3512 = t1855 * t2565 - t1860 * t2350;
  t3510 = -0.51131900567709380000e-2 + t3586;
  t3078 = -0.2e1 * t3208;
  t2297 = -t1042 * t3078 + t3494;
  t3005 = t1040 * t3208;
  t935 = 0.2e1 * t3005;
  t2716 = t935 + t3494;
  t3509 = t1846 * t2716 + t2297;
  t3507 = 0.3587895e1 * t3515 * t689;
  t2750 = 0.3127439544e-2 * t1851;
  t3505 = t2747 + t2750;
  t3504 = t3269 / 0.2e1 + t3699 / 0.2e1;
  t1374 = t1544 * t1860;
  t3501 = -t1543 * t3202 - t1374;
  t3500 = t3031 + t3230;
  t3497 = 0.1644487577369270e-2 * t1854 + t3693;
  t2660 = -t1855 * t952 + t3237;
  t1146 = 0.55993270925625000000e-2 + t3099;
  t1059 = t1146 * t1861;
  t3303 = t2341 * t1854;
  t3496 = -t3303 + t1059;
  t3315 = t1160 * t1861;
  t3329 = t1146 * t1854;
  t3495 = t3315 - t3329;
  t1387 = t1662 - 0.41460000000000000000e-2;
  t3493 = t1387 - 0.1e1 * t3333;
  t1388 = -0.55993270925625000000e-2 + t2594;
  t3492 = t1388 - 0.1e1 * t1736;
  t2285 = t1730 - 0.1e1 * t1530;
  t3491 = -0.15637197720000000000e-2 * t1858 + 0.38677424370000000000e-2 * t1851;
  t3490 = t2522 - 0.1e1 * t1379;
  t1847 = t1861 ^ 2;
  t665 = t716 * t3168;
  t284 = t665 + t3570;
  t3000 = t1247 * t3208;
  t3198 = t1854 * t1861;
  t1249 = t1308 + 0.68200e-3;
  t2575 = 0.14600000000000000000e-2 * t1852;
  t1535 = 0.45800e-3 + t2575;
  t2442 = -t1535 * t1853 + t3644;
  t388 = t1249 * t3202 + t2442 + t3639;
  t987 = t1045 * t1845;
  t3489 = -0.1e1 * t3000 + t575 * t1846 + t284 * t1847 + t3198 * t388 + t665 + t987 + 0.31784000000000000000e-1 - t3604;
  t3488 = 0.1e1 * t3732 + t3626;
  t3485 = t1308 * t3221 - t1853 * t2132;
  t3483 = t3573 - t3630;
  t3482 = -t1146 + t3657;
  t2528 = 0.83624133089188900000e-3 * t1858;
  t2597 = 0.27417955320411600000e-3 * t1851;
  t3481 = (t2528 - t2597) * t1859 + 0.50000000000000000000e0 * t3699;
  t2175 = t1623 - 0.1e1 * t1263 - 0.1e1 * t1403;
  t1769 = 0.26431758938496000000e-1 * t1859;
  t3107 = -t1619 + t1664;
  t2259 = 0.57804776249276620000e-2 - t3251 + t3107;
  t802 = t1598 + t2259;
  t757 = t802 * t1845;
  t3361 = t1769 + t757;
  t756 = t802 * t1852;
  t638 = t756 + 0.63347540234880000000e-1 + t1295;
  t2322 = (-t1852 * t638 + 0.2e1 * t3001 + t3361) * t1853;
  t2504 = 0.56786982094425000000e-2 * t1859;
  t3331 = t1145 * t1852;
  t2809 = -t2504 + t3331;
  t3440 = t1860 / 0.2e1;
  t3446 = t1854 / 0.2e1;
  t452 = t3078 * t801 - t2679;
  t3313 = t1161 * t1859;
  t657 = -t3313 - t3727;
  t3479 = ((t1860 * t452 + t2809) * t1853 + t657 * t1846 - t3707) * t3446 + (t2322 / 0.2e1 + t3708 * t3440) * t1861;
  t3478 = t1853 * (0.41065e-1 * t1855 + t2727) - t1860 * t2210;
  t3476 = 0.50000000000000000000e0 * t1860;
  t3475 = 0.50000000000000000000e0 * t3198;
  t3473 = t1729 + 0.47796540830203740000e-1;
  t931 = t3113 + t3581;
  t2246 = t931 * t1845 + t3001 - 0.22516878283212450000e-2;
  t2195 = t2246 * t1839;
  t3471 = t2195 - 0.65338343552314821500e0;
  t1698 = 0.43502269919608000000e-1 * t1852;
  t3468 = 0.92611589640160000000e-2 - t1698;
  t3105 = 0.11881704766464000000e-1 * t1858 + 0.48037471395840000000e-2 * t1851;
  t1179 = -0.25339016093952000000e0 - t3105;
  t3467 = -t1860 * t3483 - t3485;
  t3321 = t1155 * t1852;
  t3466 = -0.1e1 * t3321 - 0.50330438027992300000e0;
  t632 = -0.31476782229750000000e-1 + t3730;
  t2288 = t1736 - 0.1e1 * t1388;
  t1401 = 0.21447119530300000000e-1 - t1652;
  t2310 = t1401 + t2527;
  t3465 = t1854 * t2310 + t1861 * t2288 - t2336;
  t3462 = -0.2e1 * t1859;
  t3461 = -t1295 / 0.2e1;
  t1840 = t1854 ^ 2;
  t3460 = -t1840 / 0.2e1;
  t3459 = t1840 / 0.2e1;
  t1841 = t1855 ^ 2;
  t3458 = -t1841 / 0.2e1;
  t3457 = t1841 / 0.2e1;
  t1842 = t1856 ^ 2;
  t3456 = t1842 / 0.2e1;
  t3454 = t1846 / 0.2e1;
  t3453 = t1847 / 0.2e1;
  t1848 = t1862 ^ 2;
  t3452 = t1848 / 0.2e1;
  t1849 = t1863 ^ 2;
  t3451 = t1849 / 0.2e1;
  t3450 = -t1852 / 0.2e1;
  t3449 = -t1853 / 0.2e1;
  t3448 = t1853 / 0.2e1;
  t3447 = -t1854 / 0.2e1;
  t3445 = -t1855 / 0.2e1;
  t3444 = t1855 / 0.2e1;
  t3443 = -t1856 / 0.2e1;
  t3442 = t1856 / 0.2e1;
  t3441 = t1859 / 0.2e1;
  t3439 = t1861 / 0.2e1;
  t3438 = -t1862 / 0.2e1;
  t3437 = t1862 / 0.2e1;
  t3436 = -t1863 / 0.2e1;
  t3435 = t1863 / 0.2e1;
  t1871 = q_state_dot(1);
  t1284 = 0.48888264403680000000e-2 * t1851 - 0.19765417918080000000e-2 * t1858;
  t1141 = t1284 - 0.42894239060600000000e-1;
  t1054 = t1141 * t1853;
  t1148 = 0.22397308370250000000e-1 - t3104;
  t1728 = 0.27228906756480000000e-2 * t1858;
  t1178 = -0.12058866005175110000e-1 - t1728 - t1659;
  t1610 = 0.96837751140849200040e-2 * t1844;
  t440 = 0.96165657134134280000e-2 + t3513;
  t933 = -t1450 - 0.4979107553197859979e-3 + t3114;
  t2435 = t933 * t1845 + t440 * t1846 + t1178 * t1838 + t1179 * t1852 + 0.45033756566424900000e-2 * t1839 + t1148 * t1853 + t1610 + t1448 - 0.10872259100413549980e1;
  t1307 = 0.48888264403680000000e-2 * t1858 + 0.19765417918080000000e-2 * t1851;
  t1172 = t1307 + 0.10425949330324000000e0;
  t3086 = -0.25527100084200000000e-2 * t1858 - 0.10320550495200000000e-2 * t1851;
  t2337 = -0.54439292389350000000e-1 + t3086;
  t1409 = -0.9683775114084920003e-2 * t1851 - 0.11008587194880000000e-2;
  t2343 = -0.11653992043882679999e-2 + t3108;
  t885 = t1409 * t1858 + t2343;
  t682 = t1853 * t885 + t2337;
  t532 = t1854 * t682 + t1172;
  t1281 = 0.21934364256329279999e-2 * t1858 + t2577;
  t1183 = t1281 + 0.3742763892584200000e-3;
  t968 = t1183 * t1853 - 0.22714792837770000000e-1;
  t807 = t968 * t1852 + 0.10875022106691880e-1 * t1853 + 0.48357317375400000000e-2;
  t379 = t1854 * t807 + t1859 * t532 - t3468;
  t962 = t1151 * t1852 + 0.10572703575398400000e0;
  t876 = t962 * t1854 - 0.11357396418885000000e-1;
  t155 = t379 * t1860 + t876 * t1859 - t1085 + t1054 - 0.25817947234305000000e-1 + t2435 * t1854;
  t1768 = 0.43502269919608000000e-1 * t1859;
  t3149 = -t1056 - 0.22516878283212450000e-2 * t1839;
  t1266 = t1386 * t1858;
  t1618 = 0.24076459055801420010e-2 * t1844;
  t3111 = -t1598 - t1664;
  t2756 = t1266 + t1618 + t3111;
  t797 = -0.57804776249276620010e-2 + t2756;
  t3359 = t1845 * t797 - t1021;
  t798 = -0.69751885789075550010e-2 + t2756;
  t436 = t1845 * t798 + t2345 - t3612;
  t2564 = 0.54375110533459400000e-2 * t1853;
  t455 = -t2564 + t658 - 0.24178658687700000000e-2 + t3666;
  t194 = t436 * t1846 + t455 * t1860 + 0.37693495392476464200e0 + t3149 + t3359 + t3614;
  t1079 = t1166 * t1852;
  t1163 = -0.60294330025875550000e-2 - t3102;
  t3112 = t1598 - t1618;
  t803 = t1664 + t3112 + 0.69751885789075550010e-2 - t1266;
  t439 = t1845 * t803 + t2344 + t3612;
  t433 = t439 * t1846;
  t3430 = t3168 * t627 + t433;
  t932 = -t1452 - 0.2489553776598929990e-3 + t3112;
  t963 = t1153 * t1852 + 0.52863517876992000000e-1;
  t204 = -0.55383746372816285700e0 + t932 * t1845 + t963 * t1859 + t1163 * t1838 + t1079 + t3430 - t3614;
  t2108 = 0.51131900567709380000e-2 + t3513;
  t381 = t1853 * t2108 - t2336;
  t1164 = -0.37427638925842000000e-3 + t3094;
  t624 = t1164 * t1852 - t3717;
  t207 = t1846 * t624 - t1859 * t680 + t1860 * t381 - t823;
  t2488 = 0.56786982094425000000e-2 * t1861;
  t2353 = t1859 * t2488;
  t2423 = t899 * t3166;
  t2237 = t1186 + t3593;
  t1642 = 0.4815291811160284002e-2 * t1844;
  t2907 = t3253 + t3110;
  t2263 = -0.11560955249855324002e-1 + t2907;
  t808 = t1642 + t2263;
  t640 = t1852 * t808 + t1166;
  t3399 = t640 * t1859;
  t429 = t2237 + t3399;
  t687 = -t1853 * t890 - t2339;
  t2433 = t1852 * t687 + t1860 * t429 - t3674;
  t804 = 0.11560955249855324002e-1 + t2753;
  t639 = t1852 * t804 - t1166;
  t427 = t639 * t1859 + t2128 - t3593 + 0.8968493211292842000e-2;
  t2434 = t1860 * t427 - t3397 + t3674;
  t250 = 0.49386463087500000000e-1 + t2434 * t1854;
  t251 = -0.67903019910400000000e0 + t2433 * t1854;
  t2510 = 0.48037471395840000000e-2 * t1858;
  t3106 = 0.11881704766464000000e-1 * t1851 - t2510;
  t1165 = -0.95593081660407480000e-1 + t3106;
  t1167 = -0.13379861294270224000e-1 * t1858 + 0.43868728512658559996e-2 * t1851 - 0.44088275061402520000e-1;
  t1391 = -t2583 + 0.54457813512960000000e-2;
  t810 = -0.9630583622320568004e-2 * t1844 + t1391 * t1858 + 0.53191491764352000000e-4 * t1837 + 0.22017174389760000000e-2 * t1851 + 0.23121910499710648004e-1;
  t641 = t1852 * t810 - t1179;
  t428 = t1167 * t1845 + t641 * t1859 + 0.10572703575398400000e0 * t1852 + 0.17936986422585684000e-1 - t1290;
  t880 = -t1270 + t2343;
  t676 = t1853 * t880 + t2337;
  t1184 = -t3094 + 0.3742763892584200000e-3;
  t3298 = t1184 * t1853;
  t969 = 0.22714792837770000000e-1 - t3298;
  t255 = t428 * t1860 + t969 * t1859 + t676 * t1852 + t1165 * t1853 - 0.55505629074184340000e0;
  t2665 = t3326 + t3399;
  t3148 = t3621 * t1853;
  t534 = -t1156 - t3733;
  t281 = t534 * t1860 + 0.3288975154738540e-2 + t2665 * t1853 + t3148;
  t3182 = t1856 * t1863;
  t2930 = t3182 / 0.2e1;
  t2976 = t1855 * t3166;
  t3076 = 0.2e1 * t3198;
  t3077 = -0.2e1 * t3198;
  t3189 = t1855 * t1862;
  t2262 = -0.13950377157815110002e-1 + t2907;
  t809 = t1642 + t2262;
  t3425 = t1845 * t809;
  t3299 = t1184 * t1852;
  t625 = t3299 + t3717;
  t794 = t1613 + t2263;
  t635 = t1852 * t794 + t1166;
  t2319 = 0.5004595745882176002e-2 * t1844 + t3510;
  t650 = t1853 * t2319 + t2336;
  t3376 = t888 * t1852;
  t683 = -t1156 - t3376;
  t3308 = t1172 * t1852;
  t727 = -t3308 - t1056 - 0.11683352511943460000e1;
  t2896 = -t1079 + t3102;
  t822 = 0.17270743409850041200e0 + t2896;
  t745 = -t2503 + t822;
  t866 = 0.3288975154738540000e-2 + t3148;
  t2808 = t1768 - t3308;
  t895 = 0.40844180677309600000e0 - t2808;
  t1081 = t1172 * t1859;
  t898 = t1081 - t3468;
  t960 = t1054 - 0.12056561435880000000e0;
  t961 = -t1056 - 0.12476196535806603000e-1;
  t967 = t1085 - 0.10663433246449500000e0;
  t21 = ((-0.1e1 * t250 * t1854 + (-0.2e1 * t194 * t1854 + 0.17727845388000000000e0 + t2434 * t1861) * t1861) * t1848 + (-t207 * t1854 + ((t683 - t3311) * t1860 + t866 + (t1859 * t635 + t3326) * t1853) * t1861) * t3189 - t895 * t1854 + t898 * t3166 + t960 * t1861) * t3456 + ((t255 * t3077 + ((t1859 * t682 + t807) * t1860 + t962 * t1859 + t2435) * t1847 - t155 * t1854 + t2423 + (t1768 + t727) * t1861) * t1862 - t281 * t3193 + t625 * t3007 + (t650 + (-t3051 + t3425) * t1853) * t2976 + t1855 * t680 * t3172 + t823 * t3190) * t2930 + ((t967 * t1861 + t822 * t3076 + 0.11357396418885000000e-1 * t3172) * t1848 + t204 * t3077 + t2433 * t1847 + t961 * t3076 + 0.18916511922000000000e0 * t1861 + ((-0.1e1 * t632 - 0.10572703575398400000e0 * t3172) * t1848 - 0.1e1 * t251 + 0.2e1 * t2423) * t1854) * t3451 - t745 * t1848 * t3198 + (0.62964373601650000000e0 + t632 * t1841) * t3447 + t1841 * t2353 + (-0.36644357310000000000e0 + (t3716 - 0.10663433246449500000e0) * t1841) * t3439;
  t3434 = t21 * t1871;
  t1066 = t1156 * t1860;
  t2290 = -0.1e1 * t3299 - 0.10875022106691880000e-1;
  t2986 = t1853 * t3193;
  t2773 = t1860 * t2986;
  t2684 = -0.2e1 * t2773;
  t3070 = t439 * t3168;
  t2735 = -t1839 * t627 - 0.2e1 * t3070 + t3577;
  t2971 = t1859 * t3167;
  t2777 = t1852 * t2971;
  t2819 = t1854 * t3075;
  t2950 = t1841 * t3439;
  t3163 = t1861 * t1853;
  t2989 = t1854 * t3163;
  t3013 = t1845 * t3167;
  t3120 = t3621 * t1860;
  t3297 = t1184 * t1859;
  t3306 = t2339 * t1854;
  t340 = (t650 + (-0.1e1 * t3051 + t3425) * t1853) * t1854 + t1141;
  t505 = t640 - t3306;
  t351 = t1393 * t1854 + t1859 * t505 + t2237;
  t655 = -t1840 * t2339 - t1853 * t881;
  t432 = t1393 * t1840 + t1853 * t2290 + t1859 * t655;
  t3052 = t1150 * t3208;
  t795 = t1613 + t2262;
  t435 = t1845 * t795 + t2600 - t3052 + t3510;
  t451 = (-0.1e1 * t3311 + t683) * t1854 + t2336;
  t501 = t1854 * t635 - t2339;
  t3223 = t1841 * t1853;
  t659 = -t3223 * t888 + t2339;
  t928 = t1162 * t3223 - 0.11357396418885000000e-1;
  t23 = (((-0.1e1 * t455 * t1853 - t1057) * t1847 - 0.1e1 * t427 * t2989 + ((-0.1e1 * t3311 - t3376 - 0.1e1 * t1156) * t3198 + ((t3375 - 0.1e1 * t3312 - 0.54375110533459400000e-2) * t1860 + (-0.2e1 * t436 - 0.45033756566424900000e-2) * t1853) * t1847) * t1860) * t1848 + ((0.1e1 * t2339 * t3173 + t1846 * t2108 - 0.1e1 * t381 * t1853 + t3075 * t624 - 0.1e1 * t3121) * t1861 - 0.1e1 * t451 * t1853 + t1150 * t3013 + t501 * t3173 + t3120 * t1854 + t3121) * t3189 - 0.1e1 * t898 * t3199 + t1141 * t3167) * t3456 + ((t1861 * t3540 + t2735) * t1848 + t2735 * t1847 + (-0.1e1 * t429 * t1853 + t1066 + t3733 * t1860) * t3198 + t435 * t3075 + (t2290 - t3377) * t1846 - 0.1e1 * t432 * t1853 - t1840 * t1057) * t3451 + t3540 * t2950 - 0.1e1 * t1841 * t3070 + t3457 * t3577 + (t1841 * t2564 + t928 * t1852 + t659 * t1859 + 0.24178658687700000000e-2) * t3449 + 0.50000000000000000000e0 * t1057 + (((-0.1e1 * t1853 * t428 + (t1852 * t880 + t1165 - 0.1e1 * t3297) * t1860) * t1847 + (t440 * t2819 - 0.1e1 * t379 * t1853 + (0.90067513132849800000e-2 * t1853 + t1148) * t3167 + (t885 * t2971 + (t1183 * t1852 + 0.10875022106691880e-1) * t3167 + t1141) * t1860) * t1861 - 0.1e1 * t351 * t1853 + t1162 * t3173 - t2336 * t3167 + t888 * t3169 + t1066) * t1862 + (-0.1e1 * t1853 * t534 + t1860 * t2665 + t3120) * t3190 + t625 * t2684 - 0.1e1 * t340 * t3194 + t1855 * (-0.1e1 * t1172 - t3306) * t3173 + t3121 * t3193 + (-0.1e1 * t1151 * t2777 + t2319 * t3167 + t3013 * t809 - 0.1e1 * t1698 + 0.92611589640160000000e-2) * t3191) * t2930;
  t3433 = t23 * t1871;
  t1080 = t1166 * t1859;
  t1715 = 0.11357396418885000000e-1 * t1854;
  t1278 = t1715 - 0.52863517876992000000e-1 * t1840;
  t1397 = t1715 - 0.52863517876992000000e-1;
  t3080 = t1845 - 0.1e1 * t1838;
  t2094 = (-0.2e1 * t805 + 0.47788438159195720000e-2) * t3208 + t3080 * t1151;
  t2994 = t1852 * t3174;
  t2775 = t1853 * t2994;
  t2685 = -0.2e1 * t2775;
  t2715 = t3078 * t797 + t2812;
  t3062 = t3520 * t3166;
  t2785 = t3062 / 0.2e1;
  t2820 = -0.2e1 * t2994;
  t2928 = -t3174 / 0.2e1;
  t2945 = t1847 * t3452;
  t2951 = t1841 * t3450;
  t2952 = t1841 * t3454;
  t2978 = t1855 * t3174;
  t3014 = t1845 * t3199;
  t762 = t808 * t1845;
  t3058 = -0.2e1 * t3052 - t2503 + t762;
  t3079 = -0.1e1 * t1845 + t1838;
  t3093 = t1697 - t1080;
  t3195 = t1855 * t1852;
  t3217 = t1846 * t1854;
  t3220 = t1845 * t1854;
  t3325 = t1150 * t1859;
  t3327 = t1150 * t1838;
  t453 = t3078 * t803 - t3597;
  t3429 = t453 * t1846 + (t3311 + t3376) * t3168;
  t518 = -t1172 * t1853 + t1854 * t680;
  t758 = t804 * t1845;
  t894 = 0.43502269919608000000e-1 * t1854 - t965;
  t25 = ((((t3078 * t798 + t3597) * t1846 + (-0.1e1 * t3397 + t3409) * t1860 + t2715) * t1847 + ((t758 + t2503) * t1860 - t658 + ((0.2e1 * t3325 - 0.1e1 * t639) * t1860 - 0.1e1 * t965) * t1852) * t3198 + t804 * t3078 + t3326 - 0.1e1 * t3327) * t1848 + (((t1164 * t1859 + 0.1e1 * t3713) * t1846 + 0.1e1 * t680 * t1852 - 0.1e1 * t1002 * t1859 + t2094 * t3168) * t1861 + t2664 * t3167 + t1150 * t2685 + t794 * t3014 - 0.1e1 * t501 * t3204 - 0.1e1 * t2503 * t3199 + t1853 * t1771) * t3189 + (t1698 + t1081) * t1861 + t2808 * t3167 + t2715) * t3456 + ((((t810 * t1845 + 0.10572703575398400000e0 * t1859) * t1860 + t676 * t1859 + ((-0.2e1 * t1167 * t1859 - 0.1e1 * t641) * t1860 - 0.1e1 * t969) * t1852) * t1847 + (t2094 * t3217 + (-0.1e1 * t1852 * t532 + t3174 * t968 + t1768) * t1860 + t933 * t2820 + t1151 * t3220 - 0.1e1 * t876 * t1852 + (t1178 * t3463 + t1179) * t3174 - t3305) * t1861 + (t1771 * t1854 - 0.1e1 * t505 * t1852 + t3058) * t1860 - 0.1e1 * t894 * t1852 - 0.1e1 * t1172 * t3174 + t658) * t1862 + ((t1859 * t890 + t3312) * t1860 + (t762 - 0.1e1 * t2503 + (-0.2e1 * t3325 - 0.1e1 * t640) * t1852) * t1853) * t3190 + (-0.1e1 * t3713 + t3297) * t3010 + ((-0.2e1 * t809 - 0.47788438159195720000e-2) * t3208 + t3079 * t1151) * t2773 - 0.1e1 * t518 * t3195 + t1002 * t2978 - 0.1e1 * t1768 * t3194) * t2930 + ((t3062 - 0.1e1 * t1278 * t1852 + (-0.1e1 * t1166 * t1840 + 0.1e1 * t3306) * t1859 + t3429) * t1848 + (t1080 + t3323 + (-0.1e1 * t963 + 0.2e1 * (t1163 - 0.1e1 * t932) * t1859) * t1852 + t3429) * t1847 + ((-0.1e1 * t1852 * t640 + t3058) * t1860 + t3666 + t687 * t1859) * t3198 + (t3327 - 0.1e1 * t3326 + (-0.2e1 * t795 - 0.47788438159195720000e-2) * t3208) * t1846 + (-0.1e1 * t655 * t1852 + (0.11357396418885000000e-1 * t1840 - 0.1e1 * t3298) * t1859) * t1860) * t3451 + t3093 * t2945 + t453 * t2952 + (-0.1e1 * t1852 * t659 + t1859 * t928) * t3440 + t1397 * t2951 + t1080 * t3458 + (-t2339 * t2928 + t2785) * t1841;
  t3432 = t25 * t1871;
  t1196 = t3098 * t1838;
  t1200 = t1289 * t1853;
  t1204 = t1283 * t1852;
  t2507 = 0.19367550228169840008e-1 * t1858;
  t2850 = t1852 * t2128 - t1859 * t2439;
  t1594 = 0.79021743663150399997e-3 * t1837;
  t3109 = -t1594 + t1624;
  t2900 = -t1446 + t3109;
  t2904 = t1594 + t3135;
  t2942 = -t3209 / 0.2e1;
  t2995 = t1852 * t3193;
  t3033 = t2128 * t3202;
  t3034 = t2128 * t3204;
  t3037 = t3094 * t3208;
  t3038 = t1281 * t3208;
  t2509 = 0.63217394930520319996e-2 * t1858;
  t3129 = -t1851 * t2509 + t1728;
  t3224 = t1840 * t1853;
  t3246 = t1407 * t1851;
  t3280 = t1290 * t1852;
  t489 = t2904 - t3362;
  t3428 = t1846 * t489 + t2850 * t3168;
  t670 = t1853 * t2439 + t1311;
  t827 = t1610 - t1728 + (t2509 - 0.1e1 * t1376) * t1851;
  t835 = t1376 * t1851 - t1610 + t3129;
  t916 = -t1204 + t3098;
  t28 = ((((t2900 + t3362) * t1846 + (t1859 * t670 - t3034) * t1860 - t1205 + t991 + t3362) * t1847 + (t1853 * t3531 - t3260 - t3743) * t3198 + t3726 + 0.1e1 * t3037 + t2900) * t1848 + (((t1859 * t827 + t3280) * t1846 - t3101 * t1860 + ((-0.1e1 * t3038 + t3578) * t1860 - 0.1e1 * t1311 * t1859) * t1853 + t2850) * t1861 + (t1854 * t3531 + t3101) * t1860 + 0.1e1 * t3094 * t3014 + (-t1854 * t3718 + t1311) * t3202 - t3096 * t3199) * t3189 + t1307 * t3199 + t3362 + (-0.1e1 * t3207 - 0.1e1 * t2971) * t1284) * t3456 + (((((0.13379861294270224000e-1 * t1851 + 0.43868728512658559996e-2 * t1858) * t1845 + ((-t1615 + 0.22017174389760000000e-2 * t1858) * t1852 + t2510 + ((t2507 - 0.1e1 * t1391) * t1852 - 0.11881704766464000000e-1) * t1851) * t1859 + t3094) * t1860 + t1290 * t3202 + (t1853 * t835 + t3104) * t1852 + t3105 * t1853) * t1847 + (-t1284 * t3173 + t3260 + t1307 * t1853 + (t3578 * t1846 + ((-0.9683775114084920003e-2 * t1844 - 0.1e1 * t1409 * t1851 + t3129) * t1853 + t3104) * t3173 + t991 * t1845 + (t1650 - t2524) * t1838 + t3086 * t1853 - t1851 * t2507 + t1615 - 0.31608697465260159998e-2 * t1837 + (t2126 * t3168 + (-0.1e1 * t1846 - 0.1e1) * t1859 * t1281 + t3106) * t1852) * t1854) * t1861 + ((t1311 * t1854 - t3718) * t1859 + t2101) * t1860 + t3033 + (t1284 * t1852 - t1205) * t1854 + t670 * t1852 - t1200) * t1862 + (((t3246 + t3676) * t1852 + t3619) * t1860 + (0.1e1 * t1201 - t3398 - t3096) * t1853) * t3190 + (t1859 * t835 - t3280) * t3010 + (((-t3726 + t3038 - 0.1e1 * t991) * t1853 + t3101) * t1854 + t1307) * t3191 + ((t1311 * t1853 + t2439) * t1854 + t1284 * t1853) * t3192 - t2128 * t2995) * t2930 + ((-t1311 * t3209 + t1840 * t916 + t1861 * t3538 + t3428) * t1848 + (t1845 * t2904 - t1196 + t1204 + t3035 + t3428 - t991) * t1847 + (t3743 + 0.1e1 * t3033 + ((-0.1e1 * t3246 - t3676) * t1853 + t1311) * t1852 - t1200) * t3198 + (-t3037 - t3578) * t1846 + ((t1311 * t1840 + t1853 * t827) * t1859 + t1290 * t3204) * t1860 - t3101 * t3224 + t2904) * t3451 + t916 * t2945 + t3538 * t2950 + t489 * t2952 + ((-t2439 * t3223 - t1311) * t1859 + t1841 * t3034) * t3440 + t1311 * t1841 * t2942 + t1283 * t2951 + t1205 / 0.2e1 - t3098 * t3458;
  t3431 = t28 * t1871;
  t2666 = t1035 - t3384;
  t607 = t2666 - 0.825e-1;
  t399 = t3181 * t607 + t714;
  t3154 = t1864 * t1862;
  t715 = t748 * t3154;
  t3426 = t3156 * t607 + t715;
  t3422 = t1847 * t388;
  t3264 = t1303 * t1862;
  t759 = t3264 - t3689;
  t3411 = t1857 * t759;
  t3405 = t1864 * t759;
  t1126 = t1845 * t1248;
  t1531 = t1662 - 0.414600e-2;
  t2190 = -t2523 + t3005;
  t2097 = t1531 + t2190 + t1126;
  t1250 = t2132 + 0.34100e-3;
  t3284 = t1250 * t1859;
  t711 = -0.1e1 * t3284 + t3704;
  t387 = t1853 * t2097 + t711 * t1860 - 0.86410e-2;
  t3404 = t387 * t1861;
  t3400 = t638 * t1859;
  t686 = t1853 * t889 - t2339;
  t3396 = t686 * t1859;
  t3394 = t748 * t1862;
  t2790 = 0.8676525e-3 * t1853;
  t1643 = -0.374176e-3 + t2790;
  t2844 = 0.735522e0 * t1854;
  t2702 = t1643 * t2844;
  t2703 = 0.2970426191616e-2 * t1862;
  t771 = t1862 * t2702 + (-t1861 * t2703 - 0.1e1 * t1359) * t1853;
  t3393 = t771 * t1859;
  t2548 = 0.16724826617837780000e-2 * t1855;
  t2156 = -0.988270895904e-3 * t1862 + t2548;
  t1246 = t2156 * t1853;
  t1795 = 0.3507900e-3 * t1853;
  t1644 = -0.925496e-3 - t1795;
  t2701 = t1644 * t2844;
  t2708 = 0.1200936784896e-2 * t1861;
  t772 = -t1246 + (t1853 * t2708 + t2701) * t1862;
  t3392 = t772 * t1859;
  t2261 = -t2465 + t3524;
  t799 = -t1598 + t2261;
  t3391 = t799 * t1845;
  t2757 = t3111 + t3524;
  t800 = -0.57804776249276620000e-2 + t2757;
  t3390 = t800 * t1845;
  t755 = t800 * t1852;
  t2513 = 0.31608697465260160000e-2 * t1858;
  t3388 = ((t1378 - t2513) * t1851 + t3607) * t1859;
  t3378 = t882 * t1861;
  t2502 = 0.61597000000000000000e-1 * t1859;
  t896 = t2466 - t2502;
  t3374 = t896 * t1854;
  t3373 = t896 * t1861;
  t3371 = t918 * t1861;
  t989 = t1861 * t2738 + t2889;
  t3368 = t989 * t1862;
  t3365 = t999 * t1846;
  t3364 = t3209 * t800 + t1060;
  t1061 = t3616 * t1861;
  t3363 = t3207 * t800 + t1061;
  t614 = t638 * t1861;
  t3360 = t614 - t1070;
  t2545 = 0.21751134959804000000e-1 * t1855;
  t751 = -t3695 - t2545;
  t3352 = t1040 * t1846;
  t3351 = t1041 * t1846;
  t1052 = t1451 + 0.1194710953979893e-2 + t2603;
  t3348 = t1052 * t1838;
  t3342 = t2802 * t1862;
  t3338 = t2803 * t1857;
  t1144 = t2132 + 0.34100000000000000000e-3;
  t3332 = t1144 * t1852;
  t3328 = t3616 * t1853;
  t3322 = t1154 * t1852;
  t3320 = t1155 * t1854;
  t3319 = t1155 * t1860;
  t1087 = t1155 * t1861;
  t3318 = t1157 * t1854;
  t1158 = t1308 + 0.68200000000000000000e-3;
  t3317 = t1158 * t1852;
  t3316 = t1158 * t1859;
  t1398 = -t2488 + 0.56786982094425000000e-2;
  t2551 = 0.26431758938496000000e-1 * t1854;
  t1169 = t1398 - t2551;
  t3310 = t1169 * t1852;
  t3309 = t1169 * t1859;
  t1083 = t1173 * t1859;
  t3304 = t2341 * t1853;
  t3302 = t2341 * t1861;
  t1177 = 0.43600000000000000000e-3 + t2125;
  t3301 = t1177 * t1845;
  t2549 = 0.82500000000000000002e-1 * t1854;
  t1180 = -0.31600000000000000000e0 * t1861 + t2549 - 0.38400000000000000000e0;
  t3300 = t1180 * t1860;
  t3296 = t1185 * t1853;
  t3295 = t1185 * t1854;
  t3294 = t1185 * t1855;
  t1091 = t1185 * t1862;
  t3293 = t1189 * t1859;
  t1190 = 0.6029433002587555e-2 + t3102;
  t3292 = t1190 * t1838;
  t3291 = t1190 * t1845;
  t3290 = t1192 * t1852;
  t3287 = t1249 * t1852;
  t3286 = t1249 * t1859;
  t3285 = t1250 * t1852;
  t1251 = t1537 * t1853;
  t3283 = t1251 * t1855;
  t1203 = t1280 * t1860;
  t2514 = 0.29640000000000000000e-2 * t1858;
  t2580 = 0.47840000000000000000e-2 * t1851;
  t1285 = t2514 + t2580;
  t3282 = t1285 * t1845;
  t3279 = t3097 * t1860;
  t3278 = t1293 * t1859;
  t3277 = t3098 * t1845;
  t3276 = t2127 * t1852;
  t3274 = t3099 * t1852;
  t3273 = t3099 * t1855;
  t3272 = t3099 * t1859;
  t3270 = t3100 * t1853;
  t3268 = t3100 * t1860;
  t3267 = t3100 * t1862;
  t3266 = t1301 * t1861;
  t3263 = t1308 * t1845;
  t3262 = t1308 * t1846;
  t1274 = t1381 * t1852;
  t3249 = t1388 * t1854;
  t3247 = t1398 * t1852;
  t1372 = t1540 * t1864;
  t3231 = t2247 * t1857;
  t3227 = t1838 * t1854;
  t3226 = t1838 * t1861;
  t3225 = t1839 * t1855;
  t3219 = t1845 * t1860;
  t3218 = t1845 * t1861;
  t3216 = t1846 * t1861;
  t3215 = t1846 * t1862;
  t3214 = t1847 * t1862;
  t3213 = t1848 * t1856;
  t3211 = t1851 * t1862;
  t3210 = t1851 * t1863;
  t3206 = t1852 * t1862;
  t3205 = t1852 * t1863;
  t3201 = t1853 * t1862;
  t3200 = t1853 * t1863;
  t3196 = t1855 * t1838;
  t3188 = t1856 * t1852;
  t3178 = t1857 * t1863;
  t3176 = t1858 * t1856;
  t3175 = t1858 * t1863;
  t3171 = t1859 * t1862;
  t3170 = t1859 * t1863;
  t3165 = t1860 * t1862;
  t3164 = t1860 * t1863;
  t3161 = t1862 * t1838;
  t3159 = t1863 * t1855;
  t3158 = t1863 * t1861;
  t3145 = t1520 * t3158 + t1834;
  t1275 = t1404 * t1855;
  t1495 = t1855 * t2515;
  t3143 = t1275 - t1495;
  t3142 = t3615 * t1862;
  t2478 = 0.39252000000000000000e-1 * t1863;
  t2479 = 0.27518000000000000000e-1 * t1863;
  t3141 = -t2478 * t3179 - t2479 * t3181;
  t1584 = t1855 * t2892;
  t2740 = t1861 * t2892;
  t3139 = -t1855 * t2740 + t1584;
  t1580 = t1856 * t2894;
  t3138 = -t1862 * t2741 + t1580;
  t2546 = 0.56786982094425000000e-2 * t1855;
  t1488 = t1852 * t2546;
  t1720 = 0.12089329343850000000e-2 * t1855;
  t3125 = -t1488 + t1720;
  t1273 = t1402 * t1861;
  t3124 = t1861 * t2531 + t1273;
  t3119 = t1643 * t1861 - t2790;
  t3118 = t1644 * t1861 + t1795;
  t2857 = 0.39252e-1 * t1864;
  t2858 = 0.27518e-1 * t1864;
  t3115 = -t1855 * t2857 + t1862 * t2858;
  t3089 = t1716 - t2486;
  t3083 = -t1845 + t1838;
  t3082 = t1847 - t1840;
  t3081 = -0.1e1 * t1839 + t1846;
  t3074 = t2898 * t3208;
  t3071 = t997 * t3168;
  t2682 = -t1203 + t3047;
  t719 = t1554 + t2682;
  t3069 = t719 * t3190;
  t3068 = t748 * t3181;
  t3067 = t802 * t3207;
  t3066 = t882 * t3174;
  t2991 = t1280 * t3202;
  t901 = t1374 + t2991;
  t3064 = t901 * t3179;
  t1558 = t1853 * t2867;
  t902 = t1173 * t3204 - t1558;
  t3063 = t902 * t3179;
  t3061 = t480 * t3448;
  t992 = t1445 + t2306;
  t3059 = -t992 * t1838 / 0.2e1;
  t3057 = -t3330 + t3364;
  t3056 = t1041 * t3168;
  t3055 = t1044 * t3168;
  t3054 = t1052 * t3227;
  t3053 = t2803 * t3178;
  t3050 = t1154 * t3220;
  t3049 = t1154 * t3209;
  t3048 = t1154 * t3167;
  t1018 = t1154 * t3218;
  t1017 = t1154 * t3207;
  t3045 = t1177 * t3208;
  t3044 = t1185 * t3199;
  t1024 = t1185 * t3163;
  t3043 = t1189 * t3208;
  t3042 = t1190 * t3208;
  t3039 = t2331 * t3190;
  t1226 = t1522 * t3160;
  t3030 = t1537 * t3194;
  t3027 = t1538 * t3160;
  t3026 = t1538 * t3190;
  t3025 = t1538 * t3187;
  t3021 = t1543 * t3188;
  t3020 = t1543 * t3207;
  t3017 = t1838 * t3199;
  t3016 = t1854 * t3161;
  t3012 = t1845 * t3197;
  t3011 = t1845 * t3162;
  t3009 = t1846 * t3197;
  t3008 = t1846 * t3160;
  t3006 = t1848 * t3168;
  t1043 = 0.56440000000000000000e-2 + t2102;
  t3004 = t1043 * t3208;
  t2997 = t1852 * t3202;
  t2996 = t1852 * t3168;
  t2993 = t1852 * t3160;
  t2992 = t1096 * t3168;
  t2988 = t1286 * t3209;
  t2984 = t1854 * t3179;
  t2983 = t1854 * t3158;
  t2982 = t1854 * t3156;
  t2981 = t1855 * t3333;
  t2980 = t1852 * t3192;
  t2979 = t1853 * t3192;
  t2977 = t1855 * t3171;
  t2975 = t1853 * t3186;
  t2974 = t1854 * t3180;
  t2973 = t1857 * t3159;
  t2972 = t1852 * t3172;
  t2970 = t1853 * t3171;
  t2969 = t1859 * t3162;
  t2968 = t1859 * t3160;
  t2967 = t1854 * t3166;
  t2966 = t1860 * t3162;
  t2965 = t1860 * t3160;
  t2964 = t1052 * t3226;
  t2963 = t1185 * t3172;
  t2962 = t1861 * t3181;
  t2961 = t1857 * t3162;
  t2960 = t1861 * t3156;
  t2959 = t1144 * t3171;
  t2958 = t1166 * t3206;
  t2957 = t1853 * t3162;
  t2956 = t1854 * t3155;
  t2953 = t1840 * t3436;
  t2949 = -t3221 / 0.2e1;
  t2948 = t1845 * t3435;
  t2947 = t3215 / 0.2e1;
  t2946 = t1847 * t3436;
  t2944 = t3213 / 0.2e1;
  t2943 = t3210 / 0.2e1;
  t2941 = -t3206 / 0.2e1;
  t2940 = -t3205 / 0.2e1;
  t2939 = -t3203 / 0.2e1;
  t2938 = t3201 / 0.2e1;
  t2937 = t3200 / 0.2e1;
  t2936 = t3197 / 0.2e1;
  t2935 = t3189 / 0.2e1;
  t2933 = t1859 * t3443;
  t2932 = -t3185 / 0.2e1;
  t2931 = -t3184 / 0.2e1;
  t2929 = t3175 / 0.2e1;
  t2927 = t3174 / 0.2e1;
  t2926 = -t3173 / 0.2e1;
  t2925 = t3171 / 0.2e1;
  t2924 = t3170 / 0.2e1;
  t2923 = t3169 / 0.2e1;
  t2922 = -t3165 / 0.2e1;
  t2921 = t3165 / 0.2e1;
  t2920 = -t3164 / 0.2e1;
  t2919 = t3164 / 0.2e1;
  t2918 = t3163 / 0.2e1;
  t2917 = t3162 / 0.2e1;
  t2916 = -t3160 / 0.2e1;
  t2915 = t3160 / 0.2e1;
  t2914 = -t3159 / 0.2e1;
  t2913 = t3159 / 0.2e1;
  t2910 = -t3160 * t3647 + t3145;
  t2891 = 0.384e0 * t1863;
  t2906 = -t2891 * t3193 + t3139;
  t2901 = -t2611 + t3130;
  t2897 = -t1522 * t3187 + t1801 * t1856 + t1832;
  t2893 = 0.825e-1 * t1862;
  t2884 = 0.5317e-1 * t1856;
  t2880 = -t1839 * t716 + t696;
  t667 = t2333 - t1510;
  t2878 = t1861 * t667 + t3374 - 0.82500000000000000000e-1;
  t2877 = 0.735522e0 * t165;
  t2872 = 0.61597e-1 * t1854;
  t2869 = 0.27518e-1 * t1857;
  t2868 = 0.39252e-1 * t1857;
  t2860 = 0.61597e-1 * t1861;
  t2859 = 0.27454e-1 * t1864;
  t2856 = (t1845 * t796 - t2503) * t1860;
  t2855 = t799 * t3078;
  t2853 = -0.73000000000000000000e-3 * t1852 - 0.22900e-3;
  t2852 = t664 - t3682;
  t2851 = t770 + t3682;
  t2849 = (t2901 - t3358) * t1846 - t1204;
  t2847 = 0.735522e0 * t1851;
  t2846 = 0.735522e0 * t1852;
  t2841 = 0.735522e0 * t1858;
  t2840 = 0.735522e0 * t1859;
  t2839 = 0.735522e0 * t1860;
  t2838 = t1860 * t3091;
  t2836 = 0.735522e0 * t1861;
  t2835 = 0.104419e0 * t1862;
  t2816 = -t1521 * t1856 - t3635;
  t643 = t1864 * t2816 + t3338;
  t2828 = 0.3587895e1 * t643;
  t734 = -t1134 * t1864 + t3053;
  t2825 = 0.3587895e1 * t734;
  t767 = t1372 + t3560;
  t2824 = 0.3228604e1 * t767;
  t2154 = t1864 * t2478 + t2869;
  t2155 = t1864 * t2479 - t2868;
  t788 = t1855 * t2155 + t1862 * t2154;
  t2823 = 0.3228604e1 * t788;
  t2822 = 0.2e1 * t3042;
  t2821 = -0.2e1 * t2996;
  t2354 = t1859 * t2529;
  t2817 = -t2354 - t3355;
  t2814 = t1160 * t1854 + t1059;
  t2810 = t1142 * t1846 + t1384;
  t2807 = t1248 * t1846 + t2584 - 0.43600e-3;
  t2801 = -t1562 - t3230;
  t2799 = 0.1632768e-2 * t1854;
  t2798 = 0.4038528e-2 * t1854;
  t2797 = 0.1225946e1 * t1857;
  t2796 = 0.1666555e1 * t1857;
  t2795 = 0.3587895e1 * t1857;
  t2793 = 0.1666555e1 * t1864;
  t2792 = 0.3228604e1 * t1864;
  t2791 = 0.3587895e1 * t1864;
  t2789 = t3657 - 0.1e1 * t1146;
  t2788 = t3699 - 0.1e1 * t1295;
  t699 = t2854 + t3723 + t1274;
  t2787 = t699 * t3009;
  t2786 = t882 * t2942;
  t2784 = t1861 * t3059;
  t2783 = -0.1e1 * t3316 + t1535;
  t2782 = t1052 * t2972;
  t2781 = t1862 * t1017;
  t2780 = t3164 * t3224;
  t2779 = t1852 * t2979;
  t2778 = t1852 * t2970;
  t2776 = t1040 * t2980;
  t2774 = t1248 * t2997;
  t2771 = t1853 * t2965;
  t2770 = t1855 * t2983;
  t2769 = -t3054 / 0.2e1;
  t2768 = t1846 * t2936;
  t2767 = t1846 * t2915;
  t2766 = t1847 * t2913;
  t2765 = t1852 * t2937;
  t2764 = t1852 * t2916;
  t2763 = t1861 * t2916;
  t2762 = t1853 * t2925;
  t2761 = t1859 * t2915;
  t2760 = t1853 * t2914;
  t2759 = t1860 * t2913;
  t2758 = t1538 * t3159 + t2897;
  t2755 = t2891 * t3162 + t3138 + 0.384e0 * t3187;
  t1794 = 0.88e-1 * t1852 + 0.384e0;
  t2752 = 0.3127439544e-2 * t1794;
  t2751 = 0.7735484874e-2 * t1794;
  t2748 = 0.3127439544e-2 * t1858;
  t2746 = 0.3127439544e-2 * t1859;
  t2745 = 0.7735484874e-2 * t1859;
  t2744 = 0.3127439544e-2 * t1861;
  t2743 = 0.7735484874e-2 * t1861;
  t2742 = t1856 * t2895;
  t2739 = -0.7850e-3 + t3562;
  t2734 = t3179 * t607 - t3068;
  t2732 = 0.275214679872e-3 * t1859;
  t2731 = 0.680722668912e-3 * t1859;
  t2728 = t1860 * t2860;
  t2725 = t1863 * t2859;
  t1191 = t1853 * t2853 + 0.19192000000000000000e-1;
  t1257 = -t1306 - 0.88e-1;
  t2296 = t1257 * t3173 - t1202 + t1526;
  t2228 = t2296 * t1856;
  t254 = t1854 * t2228 + t1863 * t384 - t3703;
  t171 = t1857 * t254 + t1864 * t383;
  t2295 = -t1526 + t3500;
  t2227 = t2295 * t1856;
  t606 = t2888 + t3384;
  t409 = t1862 * t606 + t730;
  t282 = t1854 * t2227 + t1863 * t409 + t3703;
  t191 = t1864 * t282 + t399;
  t1977 = -0.1e1 * t1144 * t1859 + t3704;
  t1962 = t1855 * t1977 + t2987 * t699;
  t2364 = t1855 * t2523;
  t1935 = t1387 * t3194 - 0.86410e-2 * t1855 + t1860 * t1962 - t3009 * t560 + t3197 * t562 + (-t2364 + t2776 - t2981) * t1853;
  t2019 = t3004 + t3301 - t1176;
  t1969 = t1158 * t3202 + t1860 * t2019 + t2442;
  t1995 = t560 * t2986 + (t2190 + t3493) * t1862;
  t2073 = 0.10441900000000000000e0 * t1854 + t2238;
  t2123 = 0.39252000000000000000e-1 * t1862 + 0.27518000000000000000e-1 * t1855;
  t2086 = t2123 * t1864;
  t2122 = -t1790 + 0.10441900000000000000e0 * t1861;
  t215 = t1857 * t377 + t3153 * t376;
  t2151 = 0.61297300000000000000e0 * t1856 * t2652;
  t922 = -0.42340000000000000000e-2 - t1477 - t1274;
  t2281 = -t3723 + t922;
  t2188 = t2281 * t3460;
  t2298 = -t1226 + t3117;
  t2360 = t1856 * t2469;
  t2535 = 0.17939475000000000000e1 * t1857;
  t2361 = t1856 * t2535;
  t2536 = 0.16143020000000000000e1 * t1857;
  t2362 = t1856 * t2536;
  t247 = t1863 * t399 + t1864 * t409;
  t2474 = 0.61297300000000000000e0 * t1864;
  t2540 = 0.61297300000000000000e0 * t1857;
  t2543 = 0.36776100000000000000e0 * t1856;
  t390 = t1863 * t540 + t3187 * t971 + t3146;
  t272 = t1857 * t390 + t1864 * t541;
  t407 = t1863 * t577 + t2911;
  t291 = t1857 * t3736 + t1864 * t407;
  t324 = t1857 * t519 + t3153 * t520;
  t349 = t1864 * t577 + t3178 * t3736;
  t2092 = -0.1e1 * t3301 - 0.1e1 * t3004 + t1176;
  t370 = t1853 * t2783 + t1860 * t2092 - t3644;
  t2659 = -t1855 * t989 + t3237;
  t539 = t3157 * t989 + t2758;
  t398 = t1857 * t539 - t1864 * t2659;
  t2085 = t2122 * t1856;
  t410 = (-t1855 * t2117 - t1822) * t1864 + (t2085 + (t2870 - t3551) * t1863) * t1857;
  t2327 = t2652 * t1857;
  t571 = t1104 * t3157 + t2758;
  t413 = t1864 * t571 + t2327;
  t445 = t1857 * t760 - t2660 * t3153;
  t474 = (-t1857 * t2073 - t2725) * t1862 + (-t2073 * t3153 + 0.27454e-1 * t1857) * t1855;
  t493 = t1863 * t2327 + t1864 * t3541;
  t561 = t2007 - t3353;
  t2457 = -0.34100000000000000000e-3 - t2590;
  t701 = t1852 * t2457 + t2739;
  t769 = -t1857 * t2123 + t3346;
  t840 = -t1864 * t2247 + t3141;
  t1882 = ((-0.1e1 * t3368 - 0.1e1 * t1370) * t1856 + t2298) * t445 * t2540 + t1854 * t1969 * t2931 + t474 * (t2122 * t1863 + (t3551 - 0.1e1 * t2870) * t1856) * t2535 + (-0.1e1 * t384 * t1856 - t3709 + t2296 * t3160 - 0.1e1 * t1834) * t215 * t2541 - 0.1e1 * t734 * t2395 + 0.12445000000000000000e-2 * t1844 * t1856 - 0.1e1 * t413 * t1857 * t2151 - 0.1e1 * t643 * t2803 * t2361 + t840 * t3660 + (t1191 * t1862 + t1852 * t3590 + t1853 * t2959 - 0.12805000000000000000e-1 * t1855 + t1860 * t1995 + t1861 * t1935 + t3010 * t699 + t3193 * t701 + t3214 * t370) * t3435 - 0.42053000000000000000e-1 * t1856 + t769 * t2123 * t2362 + t1856 * t2188 * t3168 + (t1855 * t2073 + t1822) * t410 * t2360 - 0.1e1 * t399 * t191 * t2543 + 0.42800000000000000000e-3 * t1851 * t3176 + (t1840 * t3401 + t1847 * t561) * t3443 + (-0.1e1 * t291 * t3736 * t1856 + (-0.1e1 * t1856 * t540 + t3160 * t971 + t3145) * t324) * t2537 + (-0.1e1 * t171 * t376 * t1856 + t247 * (-0.1e1 * t409 * t1856 + t3709 + t2295 * t3160 + t1834)) * t2475 + (t398 * t2660 * t1856 + ((-0.1e1 * t3688 - 0.1e1 * t1370) * t1856 + t2298) * t493) * t2474 + (-0.1e1 * t272 * t520 * t1856 + (-0.1e1 * t1856 * t577 + t2910) * t349) * t2471 - 0.16143020000000000000e1 * t767 * t1856 * t2086 + 0.16143020000000000000e1 * t937 * t788;
  t712 = -0.1e1 * t3286 + 0.45800e-3 + t3724;
  t2020 = t712 * t1860 + t3668 - 0.172820e-1;
  t582 = t3000 - t987 - t1046;
  t1038 = t2379 - 0.29200000000000000000e-2 - 0.34240000000000000000e-2 * t1844;
  t1529 = t2580 + 0.136400e-2;
  t2284 = -t2514 - 0.1e1 * t1529;
  t713 = t1038 * t1859 + t1852 * t2284 - 0.84680e-2;
  t306 = t1846 * t713 + t3168 * t582 - t3645 + t3723;
  t190 = 0.95220000000000000000e-2 + t306 * t1861 + t2020 * t1854;
  t1979 = 0.83327750000000000000e0 * t1856 * t3488;
  t1985 = t1855 * t3489;
  t1533 = -t2590 - 0.34100e-3;
  t1365 = t1533 * t1852;
  t1277 = -0.7850e-3 + t1365;
  t2034 = t1277 + t3562 + t3571;
  t706 = t1853 * t2570 + t2682;
  t2081 = (-t1855 * t2878 + t1862 * t706) * t2543;
  t2318 = t1853 * t3704 - 0.19192000000000000000e-1;
  t2396 = t604 * t2474;
  t846 = 0.316e0 - t3671;
  t414 = t1863 * t846 + t3744;
  t2397 = t414 * t2471;
  t2252 = t1855 * t706 + t1862 * t2878;
  t666 = -0.82500000000000000000e-1 + t3534;
  t449 = t666 * t1854 + t3373 + 0.31600000000000000000e0;
  t225 = t1856 * t2252 + t1863 * t449;
  t2401 = t225 * t2475;
  t2402 = t868 * t2535;
  t2403 = t604 * t2540;
  t2404 = t414 * t2537;
  t550 = t1863 * t787 + t2897;
  t394 = t1864 * t550 + t3411;
  t2405 = t394 * t2540;
  t2408 = t225 * t2541;
  t717 = -t3723 - 0.42340e-2 + t3126;
  t285 = t3168 * t717 - t3570;
  t591 = -t820 - t1832 - t2242;
  t404 = t1857 * t591 + t3405;
  t595 = t1523 * t3181 + t1559 - t3711;
  t615 = t1049 + t3712;
  t629 = -t1126 - t2131 + 0.414600e-2 - t3005;
  t1883 = t1863 * t1250 * t2762 + t1862 * t285 * t2763 - t3585 * (-0.1e1 * t1540 * t3153 + t3231) * t2536 - 0.1e1 * ((t1863 * t2868 - 0.1e1 * t2858) * t1862 + (t1863 * t2869 + t2857) * t1855) * t3660 - 0.1e1 * t1857 * t181 * t2081 - 0.1e1 * t294 * t1857 * t1979 - 0.1e1 * t1540 * t3675 * t2362 + t2417 * t2402 + (t1854 * t2034 + t3404 - 0.12805000000000000000e-1) * t1863 * t3444 - 0.1e1 * t3053 * t2395 + ((t3264 - 0.1e1 * t3689) * t3153 - t787 * t1857) * t2403 - 0.50000000000000000000e0 * t3489 * t3213 - 0.1e1 * ((-0.1e1 * t3626 - 0.1e1 * t3732) * t3153 + t3637 * t1857) * t2404 - 0.1e1 * ((t3394 + (-0.1e1 * t3384 - 0.825e-1 + 0.1e1 * t1035) * t1855) * t3153 - t844 * t2961 - 0.1e1 * t3068 + t3620 * t2984 - 0.1e1 * t1857 * t2893) * t2408 + t190 * t1855 * t3183 + (-t2652 * t2396 - 0.1e1 * t3488 * t2397 - 0.1e1 * (-t3661 + (-0.1e1 * t3408 - 0.1e1 * t871) * t1855) * t2401) * t3178 + (-0.1e1 * t787 * t2396 + t404 * t2151 + t1134 * t2395 - 0.1e1 * t169 * t2081 - 0.1e1 * t297 * t1979 - 0.1e1 * t3637 * t2397 - 0.1e1 * (-0.1e1 * t3662 + t3622) * t2401) * t1864 + (t1985 * t3444 + (-0.1e1 * t3689 + t3237) * t2405 + t767 * t1540 * t2470) * t1856 + (t2360 * t615 + t2361 * t595) * t2803 - (t1860 * t629 + t2318 + t3422) * t3157 / 0.2e1;
  t1 = t1882 + t1883;
  t1253 = t1540 * t1863;
  t2055 = t2802 * t1861;
  t906 = -t1535 + t2067;
  t2668 = t906 * t1860 + 0.172820e-1;
  t527 = t1852 * t2810 - t1476 - t3055;
  t2286 = -t2520 - 0.1e1 * t1381;
  t693 = -0.1e1 * t1043 * t3169 + t2286 * t1853;
  t360 = t1847 * t527 + t3198 * t693;
  t556 = -t1038 * t1846 - t1247 * t2996 - t1044;
  t1339 = t1844 * t2375;
  t660 = t1249 * t1860 - t1339 + (-0.5644000000000000000e-2 - t2382) * t3204;
  t372 = t1854 * t660 + t1861 * t556;
  t500 = t3168 * t922 + t2346 - t3351;
  t1475 = t1852 * t2514;
  t988 = t1529 * t1852 + t1475 + 0.84680e-2;
  t514 = t1046 * t3168 + t1846 * t988 + t3645;
  t731 = t1042 + t3352;
  t526 = -t1177 * t2967 + t1847 * t731;
  t1481 = t1852 * t2511;
  t549 = t1852 * t2807 - t1481 + t3055;
  t564 = -0.15592000000000000000e-1 + t1176 * t1860 + (0.45800000000000000000e-3 + t2575) * t1853 + t3144;
  t729 = t1045 * t3166 - t1247 * t1854;
  t733 = t1045 - t3352;
  t14 = -0.1e1 * t1253 * t2800 + (t1584 + (-0.1e1 * t3555 - 0.1e1 * t1822) * t1863) * t2826 + ((-0.1e1 * t3237 + (-0.1e1 * t2249 * t1861 - 0.1e1 * t1797) * t1855) * t1863 + t3139) * t2829 + ((t3626 + (-0.1e1 * t1537 * t1854 - t2055) * t1855) * t1863 + t2906) * t2831 + ((t3683 + (t1854 * t2048 + t1861 * t1971) * t1855) * t1863 + t2906) * t2877 - 0.1e1 * t549 * t2977 + t3507 * (-t2742 + (t1822 + t3555) * t1856) + t3487 * (-t2742 + (t1855 * t2041 + t3237) * t1856) + t3486 * (-t1855 * t1580 + t2742 + (t3626 + (-t2055 - t1329) * t1855) * t1856) + 0.3228604e1 * t3515 * t3585 * t1540 * t1856 + t3506 * (-t2742 + (t1855 * t1939 - t3683) * t1856) + (t3458 + t3452) * (t729 * t3221 + t372 * t1859 + t514 * t1861 - 0.95220e-2 + (t1853 * t2285 + t2668) * t1854) + (t500 * t1847 + t360 * t1859 + t3198 * t564 + t2104 - 0.1e1 * t3168 * t996 - 0.1e1 * t3351 - 0.31784000000000000000e-1 + (t526 - 0.1e1 * t733) * t1845) * t3189;
  t2723 = -t1 * t1871 + t14 * t1870;
  t2721 = -t1185 * t3207 - t3693;
  t1547 = t1854 * t2842;
  t2054 = t2802 * t1863;
  t2440 = -t3023 + t3665;
  t17 = t2440 * t2826 + (t1547 - 0.1e1 * t2249 * t1854 * t3157 + (t1856 * t2249 + t1862 * t2833) * t1861 + t3138) * t2829 + ((t1537 * t3157 + t2056) * t1861 + (t1537 * t1856 - t1862 * t2054) * t1854 + t2755) * t2831 + ((-t1856 * t1971 - t2048 * t3157) * t1861 + (-t1856 * t2048 + t1971 * t3157) * t1854 + t2755) * t2877 + ((-0.1e1 * t1177 * t1860 * t3082 + t3077 * t731) * t1845 + (t3077 * t527 + t3082 * t693) * t1859 + t500 * t3077 + t3082 * t564) * t3457 + ((-0.1e1 * t556 * t1859 - 0.1e1 * t514) * t1854 + (t1859 * t660 + t2668) * t1861 + (-0.1e1 * t1045 * t3013 + (-0.1e1 * t1125 + t2285) * t1861) * t1853) * t2935 + t3507 * ((-t1856 * t2835 + t2881) * t1861 + (t1862 * t2884 + t2834) * t1854) + t3487 * ((t1522 * t1863 - t2693) * t1861 + (t1522 * t3183 + t2833) * t1854) + t3486 * (-t2893 * t3187 - t2740 + (t1520 * t3183 - t2054) * t1861 + (-t1520 * t1863 - t1862 * t2056) * t1854) + t3506 * ((t1863 * t1966 - t2014 * t3183) * t1861 + (t1863 * t2014 + t1966 * t3183) * t1854);
  t2186 = t2523 - 0.1e1 * t3005;
  t2110 = -0.1e1 * t1126 + t2186;
  t710 = t1852 * t2105 + t2853 + t3284;
  t2011 = t710 * t1860 + 0.86410e-2 + (-t1531 + t2110) * t1853;
  t2329 = t1862 * t3671;
  t2031 = (t1863 * t2329 - t3729) * t1864;
  t2233 = t3591 * t1856;
  t2074 = (t2233 - t3687) * t1864;
  t2234 = t1855 * (-0.1e1 * t3244 + t1801);
  t2390 = t1862 * t3719;
  t2278 = t1863 * t2390;
  t2325 = t3671 * t1855;
  t2398 = t404 * t2474;
  t307 = t1365 + t2739 + t3571;
  t1888 = (t3620 * t2962 - 0.1e1 * t568 * t1854 + (t3184 * t844 - t2278) * t1864) * t2408 + (t918 * t2960 - 0.1e1 * t502 * t1854 + (t707 * t3184 + (t3371 - 0.1e1 * t3395) * t3157) * t1857) * t2401 + (t1863 * t3591 + t3686) * t2398 + ((-t3157 * t3671 + t3729) * t1857 - t1864 * t2325) * t2397 + (-t1857 * t2325 + t2031) * t2404 - ((t1522 * t3184 + t1547 + t3687) * t1857 + t1864 * t2234) * t2396 - 0.1e1 * t388 * t2770 + (-0.1e1 * t307 * t1854 + t2011 * t1861) * t3442 + ((-0.2e1 * t284 * t3198 + (t1847 - 0.1e1 * t1840) * t388) * t3186 + (-0.1e1 * t387 * t1854 + t2034 * t1861) * t1863) * t3437 + (-0.1e1 * t306 * t1854 + t2020 * t1861) * t2944 - 0.1e1 * (t1863 * t2041 - t3686) * t2405 - 0.1e1 * (t1857 * t2234 + t2074) * t2403 - 0.1e1 * t3580 * t2402 - 0.1e1 * (-0.1e1 * t1539 * t3156 + t1857 * t2440) * t2395 + (-0.1e1 * t595 * t2535 - 0.1e1 * t615 * t2469) * (t1539 * t3183 + t1863 * t2248) + t3603 * (-t1863 * t3706 - t3183 * t3671) + (t1840 * t2914 + t2766) * t285 + t3602 * ((t1861 * t666 - t3374) * t1863 + (-t1854 * t667 + t3373) * t3183);
  t1415 = 0.4841887557042460e-2 * t1851 + 0.55042935974400000000e-3;
  t2189 = t1415 * t1858 + t3705;
  t2033 = -0.1e1 * t2781 + t2189 * t1855;
  t1952 = -t1192 * t3195 + t1859 * t2033 + t3011 * t799 - t3162 * t858 - 0.5437511053345940e-2 * t1855;
  t2547 = 0.46305794820080000000e-2 * t1855;
  t2153 = t1160 * t1862 + t1852 * t751 + t2547;
  t1400 = 0.27219646194675000000e-1 + t2596;
  t1490 = t1855 * t2521;
  t737 = t3143 + t1091;
  t2206 = t1854 * t737 + t1490 + (t1400 - t3330) * t1855;
  t1930 = t1952 * t1853 + t2206 * t1859 + (t1146 * t1862 + t3125) * t1861 + t2153 * t1854 + t1393 * t1855;
  t488 = t1854 * t638 + t3330;
  t1936 = -t1154 * t3012 + t1855 * t3465 + t1861 * t2137 + t3171 * t488 + t3197 * t3523;
  t1976 = -0.1e1 * t3291 + 0.2502297872941088000e-2 * t1844 + 0.790217436631504e-3 * t3212 + t2345;
  t1953 = t1855 * t1976 - t3162 * t633;
  t1983 = t1854 * t2789 + t1861 * t2091;
  t2313 = 0.29682175996164750000e0 + t3331;
  t2059 = t1855 * t2313 - 0.16444875773692700000e-2 * t1862;
  t750 = -t3695 + t2545;
  t2061 = t750 * t1861 + (0.52863517876992000000e-1 - t1716) * t1855;
  t738 = -t1091 + t3143;
  t2069 = t738 * t1852 - 0.50330438027992300000e0 * t1855 - 0.66241105529490700000e-2 * t1862;
  t2120 = t1859 * t3360 + t1861 * t2818 - t3248;
  t2599 = 0.11947109539798930000e-2 * t1845;
  t1889 = 0.82224378868463500000e-3 * t3184 + t1983 * t2932 + t2120 * t2939 + t882 * t1856 * t2928 - 0.50000000000000000000e0 * t3569 * t3187 + (t1163 * t3196 + t1166 * t3195 + t1846 * t1953 + t1853 * t1936 + t1854 * t2059 + t1859 * t2061 + t1860 * t1930 + t1861 * t2069 + (-0.1e1 * t2599 + t3471) * t1855) * t3435;
  t3 = t1888 - t1889;
  t2720 = t17 * t1870 + t1871 * t3;
  t1956 = (t1541 * t1855 + 0.10517e-1 * t3162) * t1860 + (t1541 * t3162 - 0.10517e-1 * t1855) * t1853;
  t1968 = t1854 * t1972;
  t2004 = t1045 * t1854;
  t2200 = t1538 * t1854;
  t2203 = t1861 * t1543;
  t20 = (-0.1e1 * t1856 * t2200 - 0.1e1 * t1863 * t3478) * t2829 + (t1863 * t1956 + t3041) * t2831 + (t1856 * t1968 + ((-0.1e1 * t1543 * t3162 + t3633) * t1860 + t3658) * t1863) * t2877 + ((t1040 * t1847 * t3641 + t1177 * t3198) * t3221 + ((t1142 * t2821 + t3561) * t1847 + (t1043 * t3204 + t1860 * t2286) * t3198) * t1859 + (-0.1e1 * t3084 * t922 + 0.2e1 * t3056) * t1847 + (-0.1e1 * t1176 * t1853 + (0.45800000000000000000e-3 + 0.1e1 * t3724) * t1860) * t3198) * t3457 + (t729 * t3219 - 0.1e1 * t1839 * t1045 * t3218 + ((0.2e1 * t1038 * t3166 - 0.1e1 * t1854 * t1249) * t1853 + ((t1839 - 0.1e1 * t1846) * t1861 * t1247 - 0.1e1 * t1860 * t2004) * t1852) * t1859 + (-0.1e1 * t1046 * t3084 + t3075 * t988) * t1861 - 0.1e1 * t906 * t3199 + t2285 * t3167) * t2935 + t3006 * t3353 + (t1248 * t2821 - 0.1e1 * t3561) * t1848 * t3441 + (-0.1e1 * t3084 * t996 - 0.2e1 * t3056) * t3452 + t3487 * (t1856 * t3478 - t1863 * t2200) + t3486 * (t1856 * t1956 - t3625) + t3506 * (t1863 * t1968 + ((t1862 * t2203 - t3633) * t1860 - t3658) * t1856);
  t2143 = (t719 * t3162 + (t1562 + t3500) * t1855) * t1857;
  t2111 = t1863 * t2143;
  t2241 = t2441 * t3190;
  t749 = -t3046 + t2801;
  t2112 = (t1862 * t749 - t2241) * t1857;
  t2432 = t1855 * t749 + t2441 * t3162;
  t2293 = t2432 * t1863;
  t2416 = -t1862 * t3090 - t3026;
  t2418 = t3039 + t3342;
  t2424 = (-t3031 + t2801) * t1862;
  t2656 = t2770 / 0.2e1;
  t2038 = t2067 - 0.1e1 * t1535;
  t392 = -0.1e1 * t3668 + (t2038 + t3286) * t1860;
  t1887 = (t2112 + (t2441 * t3187 + t2293) * t1864) * t2408 + (t1864 * t2424 + t2111 + (t2960 + t2974) * t719) * t2401 + (t3027 - t3722) * t2398 + (((t3624 - t3343) * t1863 + t3041) * t1857 + t2418 * t1864) * t2397 + (((-0.1e1 * t3624 + t3343) * t1863 - 0.1e1 * t3041) * t1864 + t2418 * t1857) * t2404 - ((-t1863 * t2157 - 0.1e1 * t3025) * t1857 + t2416 * t1864) * t2396 + ((-0.2e1 * t665 - t3081 * t575) * t1861 + (-0.1e1 * t710 * t1853 + (-0.1e1 * t1531 + t2110) * t1860) * t1854) * t3442 + (((t2880 - t3739) * t1847 + t392 * t3198 + t575 * t3075 + t2880) * t3186 + (-0.1e1 * t711 * t1853 + t2097 * t1860) * t3158 - 0.2e1 * t716 * t2771 - (t3008 - 0.1e1 * t1839 * t3160) * t575) * t3437 + ((-0.2e1 * t713 * t3168 + t3081 * t582) * t1861 + (-0.1e1 * t712 * t1853 + t3639) * t1854) * t2944 + t392 * t2766 + t629 * t2760 + t3704 * t2759 - 0.1e1 * (t3722 - 0.1e1 * t3027) * t2405 - 0.1e1 * (((-t1855 * t3090 + t1260) * t1863 + t3025) * t1864 + t2416 * t1857) * t2403 + (t3739 - 0.1e1 * t3084 * t717) * t2656 + t1250 * t2914 * t3173 + t3603 * (t3624 * t1856 - 0.1e1 * t3625 - t1855 * t2056) + t3602 * ((t1203 + (-0.1e1 * t1083 - t2570) * t1853) * t3160 + t706 * t1856 * t3162 + t3534 * t3186);
  t1494 = t1855 * t1732;
  t2100 = t2595 + t3592;
  t646 = t2341 - t3495;
  t2008 = t1855 * t2100 + t1862 * t646 - t1494;
  t2057 = t1388 - t1736 + t2814;
  t1493 = t1855 * t2522;
  t618 = t1168 * t1862 + t3697;
  t2077 = t1852 * t618 + t1862 * t897 - t1493 + (t1379 + t3302 + t3329) * t1855;
  t2412 = t2966 - t3194;
  t2141 = -t1154 * t2412 + t3197 * t911;
  t2458 = t1777 - 0.12089329343850000000e-2;
  t2166 = t2458 + t3310 - t3318;
  t2429 = t1861 * t911 + t3048;
  t2280 = t2429 * t1845;
  t1491 = t1855 * t2532;
  t647 = -t1061 - t3536;
  t369 = -t1408 * t1855 - t1491 + (t647 + t3067) * t1862;
  t2185 = -0.1e1 * t1087 + t3616;
  t459 = -0.1e1 * t1185 * t3162 + (t2185 + t1070) * t1855;
  t563 = t1154 * t3197 + t3194 * t800;
  t2294 = t1852 * t563 + t1853 * t459 + t1860 * t369;
  t821 = -t3330 + t1145;
  t434 = t821 + t3364;
  t2303 = t1860 * t434 + t1017 + t3044;
  t1489 = t1854 * t2546;
  t2487 = 0.21751134959804000000e-1 * t1861;
  t2168 = -0.26431758938496000000e-1 - t2487;
  t600 = t1855 * t2168 + t3162 * t882 + t1489;
  t1918 = (t1052 * t3016 + t1132 * t3197 + t1845 * t2141 + t1853 * t2008 + t1859 * t2294 + t1860 * t2077 + t3204 * t600) * t3435 + t2280 * t3443 + t2303 * t2933 + t2166 * t2932 + t2057 * t2939 - t2786 * t3203 + (t1132 + t3348) * t2931;
  t7 = t1887 - t1918;
  t2719 = t1870 * t20 + t1871 * t7;
  t2148 = t1524 * t1861;
  t1950 = (-t1854 * t2863 - t2148) * t1859 + (t1860 * t2147 - t2860) * t1852;
  t1954 = -t3030 + ((-t1860 * t2862 + t2873) * t1859 + (t1860 * t2861 + t2874) * t1852) * t1862;
  t24 = ((t3556 - 0.1e1 * t3553) * t1856 + t1954 * t1863) * t2831 + (t1950 * t1856 + (t3663 + ((t2147 - 0.1e1 * t2728) * t1859 + (t1524 * t3166 + t2872) * t1852) * t1862) * t1863) * t2877 + (t526 * t3078 + ((-0.1e1 * t1730 + t2810) * t1847 - 0.1e1 * t1043 * t2967) * t1845 - 0.1e1 * t360 * t1852 + (-t1503 - 0.1e1 * t3255) * t1847 * t3168 + t3723 * t2989) * t3457 + (-0.2e1 * t729 * t2997 + (-0.1e1 * t1247 * t3166 - t2004) * t3221 - 0.1e1 * t372 * t1852 + ((t1529 + t2514) * t1859 * t1846 - t3123) * t1861 - t3723 * t3167) * t2935 - 0.1e1 * (t1848 * t733 - t1040) * t3208 + ((-0.1e1 * t2511 + t2807) * t1848 + t1248) * t3579 + (t1534 * t1852 + t1848 * t549 + t1476) * t3450 + 0.50000000000000000000e0 * t3123 * t3006 + t3486 * ((t3553 - t3556) * t1863 + t1954 * t1856) + t3506 * (t1950 * t1863 + (-t3663 + ((t2728 - t2147) * t1859 + (-t1860 * t2148 - t2872) * t1852) * t1862) * t1856);
  t2321 = -0.1e1 * t3241 + t2867;
  t1011 = t2321 * t1860;
  t2191 = (t1011 * t1861 - t3634) * t1862 + t902 * t1855;
  t2152 = t2191 * t1864;
  t2194 = t2321 * t3194;
  t2214 = -0.1e1 * t1082 + t2502;
  t2425 = (t1524 * t3204 - t1558) * t1862;
  t934 = -0.2e1 * t3005;
  t2717 = t934 - t3494;
  t2431 = t2717 * t1846;
  t2655 = t1859 * t2760;
  t1561 = t1859 * t2863;
  t2681 = t1524 * t3169 - t1561;
  t373 = (-0.2e1 * t3000 - 0.1e1 * t1838 * t1045 + t987) * t1860 + (-0.1e1 * t3287 - t3723) * t1853;
  t601 = t1248 * t1838 - t1126 + t934;
  t903 = t1173 * t3169 - t1561;
  t938 = t1083 + t2570;
  t970 = t1806 + t1083;
  t1884 = (t1863 * t2152 + (t2681 * t3181 + t3155 * t3516) * t1861 + t1011 * t2956 + t3063 + t3516 * t2985) * t2408 + ((t1857 * t2194 + t2961 * t903 + t2984 * t970) * t1863 + (-0.1e1 * t3516 * t3180 + t3156 * t903) * t1861 + t1864 * t2425 + t903 * t2974 + t970 * t2982) * t2401 + (((t3544 - 0.1e1 * t3283) * t1863 + t3545) * t1857 + (t1251 * t1862 + t2255) * t1864) * t2397 + (((-0.1e1 * t3544 + t3283) * t1863 - 0.1e1 * t3545) * t1864 + t1251 * t3179 + t1537 * t1860 * t2962 + t1541 * t2985) * t2404 + ((t1533 * t1859 + t1846 * t725 + t3168 * t601 + t2817) * t1861 + (-0.1e1 * t3285 + t3679) * t3167 + 0.2e1 * t1854 * t2774 + (-0.1e1 * t3014 + t3017) * t1040) * t3442 + (((t688 + t3509) * t1847 + t373 * t3198 + (-0.1e1 * t1248 * t3083 + t935) * t1846 + t688 - 0.2e1 * t3003 + t3083 * t1247) * t3186 + ((-0.1e1 * t3679 + t3285) * t1860 - 0.2e1 * t2774 + t3589) * t3158 + t725 * t3008 + t601 * t2771 - 0.1e1 * t3642 * t2993 - 0.1e1 * t2354 * t3160 + t1533 * t2968) * t3437 + (((-0.1e1 * t1038 * t1852 + t2284 * t1859) * t1846 + (-0.1e1 * t1838 * t1247 + t1125 + 0.2e1 * t3003) * t3168 + t725) * t1861 + (t3714 + t3287) * t3167 + t1247 * t2685 + (t3014 - 0.1e1 * t3017) * t1045) * t2944 + t373 * t2766 + (0.2e1 * t2999 - 0.1e1 * t3353 + t3354) * t2759 + t1250 * t1855 * t2765 + (t2431 - t688 - 0.1e1 * t2297) * t2656 + t3642 * t2655 + t3603 * ((t3544 - t3030) * t1856 - t2414 * t1863) + t3602 * ((t1861 * t938 + t2214 * t3167) * t1863 + (-t2502 + t1082) * t1856 * t2966 + t938 * t1854 * t3183 + t2214 * t2975);
  t919 = -t1860 * t2340 - 0.21751134959804000000e-1;
  t2078 = t1855 * t919 - t3695;
  t1412 = 0.935690973146050000e-4 + t2586;
  t920 = t1860 * t3615 - 0.56786982094425000000e-2;
  t2113 = t920 * t1855 + (t1412 + t2532) * t3165;
  t1016 = t1145 * t3197;
  t2204 = t3162 * t3616 + t1016 + t3142 - t3294;
  t921 = 0.56786982094425000000e-2 + t3664;
  t1942 = t1853 * t2204 + t1854 * t2078 + t1855 * t921 + t1861 * t2113;
  t2150 = t1860 * (-0.1e1 * t1263 - t3528);
  t1957 = (t1004 * t1855 + t1862 * t2150) * t1861 + (t1855 * t3649 + t1862 * t2308) * t1854 + t1003 * t1855;
  t2180 = t2340 + t3539;
  t2411 = -0.935690973146050000e-4 + t3097;
  t2253 = t1860 * t2411;
  t1982 = t1853 * t2180 + t1854 * t2253 - t3378;
  t2026 = t1263 + t3528;
  t2006 = t1860 * t2026;
  t1984 = t1185 * t1861 + t1854 * t2006;
  t1487 = t1862 * t1716;
  t2144 = t1862 * t2486 - t1487 - t3519;
  t806 = -0.32797153116247448000e-1 + t2757;
  t2029 = t1859 * t2144 + t3162 * t806;
  t2260 = t1598 + 0.32797153116247448000e-1 + t3107;
  t2230 = -t3251 + t2260;
  t2182 = t2230 * t1854;
  t2098 = t2182 + t3309;
  t1906 = (t1852 * t1942 + t1853 * t2029 + t1859 * t1957 + t3191 * t806) * t3435 + t2098 * t2939 + t1984 * t2933 - t1982 * t3188 / 0.2e1;
  t9 = t1884 - t1906;
  t2718 = t1870 * t24 + t1871 * t9;
  t2714 = 0.2580137623800e-3 * t1854;
  t2713 = 0.6381775021050e-3 * t1854;
  t2712 = 0.2580137623800e-3 * t1855;
  t2711 = 0.6381775021050e-3 * t1855;
  t2710 = 0.2580137623800e-3 * t1861;
  t2709 = 0.6381775021050e-3 * t1861;
  t2707 = 0.2970426191616e-2 * t1861;
  t2706 = 0.2580137623800e-3 * t1862;
  t2705 = 0.6381775021050e-3 * t1862;
  t2694 = 0.104419e0 * t3181;
  t2690 = t1859 * t2839;
  t2688 = t1862 * t2834;
  t2687 = t414 * t2793;
  t2686 = t868 * t2791;
  t2683 = t1024 - t3049;
  t2428 = -t1280 * t3209 + t1861 * t850;
  t2279 = t2428 * t1862;
  t2018 = (t1855 * t3501 + t2279) * t1857;
  t2005 = t1863 * t2018;
  t2089 = t2131 * t1852;
  t2039 = t1859 * t998 + t2089;
  t2043 = t1308 * t3199;
  t2171 = t1855 * t901 - t1862 * t3584;
  t2138 = t2171 * t1864;
  t2426 = t3501 * t1862;
  t2427 = t1285 * t3208 + t1845 * t2898;
  t396 = (-0.1e1 * t3282 + 0.1e1 * t3074 + t1308) * t1860 + (-0.1e1 * t3278 + t1992) * t1853;
  t995 = -0.68480000000000000000e-2 * t3212 - 0.99560000000000000000e-2 * t1844 + 0.99560000000000000000e-2 * t1837;
  t1885 = (t1863 * t2138 + (-t1864 * t3021 + t2413 * t3181) * t1861 - t2413 * t2956 + t3064 - t1543 * t1852 * t2985) * t2408 + (t2005 + (t1857 * t3021 + t3156 * t850) * t1861 - t1864 * t2426 + t850 * t2974 - t1280 * t1852 * t2982) * t2401 + ((-t1846 * t3638 + t3168 * t548 + t2039) * t1861 + t3483 * t3167 - t999 * t2775 + t3485 * t1854) * t3442 + ((-t1847 * t3735 + t3198 * t396 + t2427 + t3427 - t994) * t3186 + (t2997 * t999 + t3467) * t3158 - t3638 * t3008 + t548 * t2771 + t998 * t2968 + t2131 * t2993) * t3437 + (((t1852 * t2584 - t1859 * t995 - t1481) * t1846 + (-t2427 - t2898) * t3168 - t3638) * t1861 + (t3278 - t1992) * t3167 - t1285 * t3014 + t2898 * t2775 + t2043) * t2944 + t396 * t2766 + (t3263 + t3677) * t2759 - t2131 * t2655 + t3735 * t2656 + t2760 * t3573 + t3602 * ((-t1280 * t3207 - t3576) * t1863 + ((-t1306 * t1860 - t2991) * t1855 + t2279) * t1856);
  t1032 = -t1853 * t2799 + t3118;
  t2225 = -0.6381775021050e-3 + t2709;
  t2505 = 0.16724826617837780000e-2 * t1859;
  t1989 = (-t2505 + t2751) * t1854 + t2225;
  t2490 = 0.16724826617837780000e-2 * t1861;
  t2371 = t1852 * t2490;
  t2558 = 0.54835910640823200000e-3 * t1854;
  t2076 = t1853 * t2558 + t2371;
  t1945 = t1032 * t2840 + t1860 * t1989 - t2076;
  t1031 = t1853 * t2798 + t3119;
  t2226 = -0.2580137623800e-3 + t2710;
  t2506 = 0.54835910640823200000e-3 * t1859;
  t1990 = (t2506 + t2752) * t1854 + t2226;
  t2492 = 0.54835910640823200000e-3 * t1861;
  t2372 = t1852 * t2492;
  t2555 = 0.16724826617837780000e-2 * t1854;
  t2075 = t1853 * t2555 - t2372;
  t1946 = t1031 * t2840 + t1860 * t1990 - t2075;
  t2646 = t1794 * t2744;
  t2158 = t2646 - t2714;
  t2072 = -t2158 - 0.988270895904e-3;
  t1360 = 0.2444413220184e-2 * t1855 + 0.54835910640823200000e-3 * t1862;
  t915 = -0.1e1 * t1360 * t1861 + (-0.2970426191616e-2 + t2713) * t1855;
  t1978 = t1859 * t915 + t1862 * t2072 + t2548;
  t1997 = t1360 * t1852 - t1853 * t2712;
  t1998 = t1361 * t1852 - t1853 * t2711;
  t1527 = t1854 * t2705;
  t2448 = t1854 * t2712;
  t917 = -t1361 * t1861 + 0.1200936784896e-2 * t1855 - t2448;
  t2453 = t1859 * t917 - t1359 + t1527;
  t2644 = t1862 * t2751;
  t2115 = -t1861 * t2644 + t2453;
  t2449 = t1852 * t2711;
  t2224 = -t1361 * t1853 + t2449;
  t1244 = t1360 * t1853;
  t2450 = t1852 * t2712;
  t2299 = t1244 - t2450;
  t2553 = 0.49096519673609460000e-2 * t1854;
  t2356 = t1859 * t2553;
  t2544 = 0.24548259836804730000e-2 * t1856;
  t2647 = t1855 * t2751;
  t2648 = t1855 * t2752;
  t1892 = t2544 * t3172 + ((t1853 * t2647 + t1854 * t1998 + t1860 * t2115 + t1861 * t2299 + t2450 + t3392) * t1858 + (t1853 * t2648 + t1854 * t1997 + t1860 * t1978 + t1861 * t2224 - t2449 + t3393) * t1851 - t1862 * t2356) * t3435 + t1946 * t1851 * t3443 - t1945 * t3176 / 0.2e1 + (-t2544 * t3167 + t3435 * t3512) * t1852;
  t18 = t1885 - t1892;
  t1955 = t1852 * t2203 + t1854 * t1987;
  t2068 = t2106 * t1852;
  t29 = (t1955 * t1856 + ((-0.1e1 * t3557 + t3554) * t1855 + (t3552 - 0.1e1 * t3022) * t1862) * t1863) * t2877 + (((t3365 + t994) * t1847 + t1285 * t2967) * t1845 + ((t3071 + t1477 + (t2585 + t3262) * t1852) * t1847 + (-t2898 * t3169 + (-0.1e1 * t1730 + t2588) * t1853) * t3198) * t1859 + (t3365 - t2898 + t2992) * t1847 + (-0.1e1 * t1308 * t1860 - t1339 + t1853 * t2068) * t3198 + t999) * t3457 + ((t1285 * t1854 + t3166 * t3670) * t3221 + ((t1285 * t2996 + t1846 * t995 + t997) * t1861 + t1854 * (-0.1e1 * t1293 * t1860 - t1337 + t2107 * t3204)) * t1859 + (t1846 * t1852 * t2125 + t3168 * t3670 + t1096) * t1861 + t1992 * t3167 - 0.1e1 * t2043) * t2935 + ((-0.1e1 * t3365 + t2898) * t1848 - t999) * t3579 + ((-0.1e1 * t3071 + t1475) * t1848 - t1477 + ((-0.1e1 * t3262 + t2580) * t1848 - 0.1e1 * t2585) * t1852) * t3441 + (-0.1e1 * t3365 - 0.1e1 * t2992) * t3452 + t3506 * (t1955 * t1863 + ((-t3554 + t3557) * t1855 + (t3022 - t3552) * t1862) * t1856);
  t2680 = t18 * t1871 + t1870 * t29;
  t1785 = 0.13297872941088e-4 * t1837;
  t2677 = t3585 * t2792;
  t2673 = t1854 * t970 + t1861 * t903;
  t829 = (t2513 - 0.1e1 * t1378) * t1851 - t3607;
  t651 = t1859 * t829 - t3276;
  t2658 = 0.735522e0 * t3119;
  t2657 = 0.735522e0 * t3118;
  t2654 = t1853 * t2761;
  t1304 = t2488 + t2551;
  t2650 = -t1304 * t1852 - t3318;
  t2645 = t1794 * t2743;
  t2643 = 0.36776100000000000000e0 * t171;
  t2642 = 0.73552200000000000000e0 * t171;
  t2639 = 0.36776100000000000000e0 * t191;
  t2638 = 0.73552200000000000000e0 * t191;
  t2637 = 0.36776100000000000000e0 * t215;
  t2636 = 0.73552200000000000000e0 * t215;
  t2635 = 0.36776100000000000000e0 * t247;
  t2634 = 0.73552200000000000000e0 * t247;
  t2633 = 0.83327750000000000000e0 * t272;
  t2632 = 0.16665550000000000000e1 * t272;
  t2631 = 0.83327750000000000000e0 * t291;
  t2630 = 0.16665550000000000000e1 * t291;
  t2629 = 0.83327750000000000000e0 * t324;
  t2628 = 0.16665550000000000000e1 * t324;
  t2627 = 0.83327750000000000000e0 * t349;
  t2626 = 0.16665550000000000000e1 * t349;
  t2625 = 0.61297300000000000000e0 * t398;
  t2624 = 0.12259460000000000000e1 * t398;
  t2623 = 0.35878950000000000000e1 * t410;
  t2622 = 0.61297300000000000000e0 * t413;
  t2621 = 0.12259460000000000000e1 * t413;
  t2620 = 0.61297300000000000000e0 * t445;
  t2619 = 0.12259460000000000000e1 * t445;
  t2618 = 0.35878950000000000000e1 * t474;
  t2617 = 0.61297300000000000000e0 * t493;
  t2616 = 0.12259460000000000000e1 * t493;
  t2615 = 0.32286040000000000000e1 * t769;
  t2613 = 0.32286040000000000000e1 * t840;
  t2608 = 0.50000000000000000000e0 * t1839;
  t2607 = 0.39510871831575200000e-3 * t1844;
  t2574 = 0.49096519673609460000e-2 * t1852;
  t2572 = 0.21751134959804000000e-1 * t1852;
  t2569 = 0.88000000000000000000e-1 * t1852;
  t2568 = 0.54835910640823200000e-3 * t1853;
  t2567 = 0.16724826617837780000e-2 * t1853;
  t2563 = 0.56786982094425000000e-2 * t1853;
  t2560 = 0.36776100000000000000e0 * t1853;
  t2559 = 0.25801376238000000001e-3 * t1854;
  t2557 = 0.63817750210500000002e-3 * t1854;
  t2552 = 0.21751134959804000000e-1 * t1854;
  t2542 = 0.10441900000000000000e0 * t1857;
  t2538 = 0.73552200000000000000e0 * t1857;
  t2534 = 0.32286040000000000000e1 * t1857;
  t2516 = 0.24209437785212300000e-2 * t1858;
  t2501 = 0.28244044800000000000e0 * t1859;
  t2500 = 0.54835910640823200000e-3 * t1860;
  t2499 = 0.16724826617837780000e-2 * t1860;
  t2494 = 0.36776100000000000000e0 * t1860;
  t2493 = 0.25801376238000000001e-3 * t1861;
  t2491 = 0.63817750210500000002e-3 * t1861;
  t2489 = 0.49096519673609460000e-2 * t1861;
  t2483 = 0.10875567479902000000e-1 * t1862;
  t2482 = 0.53170000000000000000e-1 * t1862;
  t2480 = 0.24548259836804730000e-2 * t1863;
  t2476 = 0.10441900000000000000e0 * t1864;
  t2472 = 0.73552200000000000000e0 * t1864;
  t2468 = 0.32286040000000000000e1 * t1864;
  t2460 = -t2552 + 0.56786982094425000000e-2;
  t2459 = -t2552 + 0.11357396418885000000e-1;
  t2455 = t3281 + t3701;
  t2452 = t1852 * t2706;
  t2451 = t1852 * t2705;
  t2447 = t1854 * t2711;
  t2446 = t1855 * t2710;
  t2445 = t1855 * t2709;
  t1193 = -0.93569097314605e-4 + t3097;
  t2231 = t2345 + t3526;
  t437 = -t3001 + t2231 + t3391;
  t930 = t1452 + 0.2489553776598930000e-3 - t3113;
  t2436 = t930 * t1845 + t437 * t1846 + t3292 - t1079 - t1612 - t1449 + 0.54361295502067749900e0 + t3149;
  t2422 = -t1584 * t1857 + t1855 * t2859 + t1863 * t3618 + t3609;
  t2421 = t1855 * t2725 + t1863 * t3609 - t1582 + t3618;
  t2420 = 0.384e0 * t1859 - 0.61597e-1;
  t2407 = t225 * t2538;
  t2400 = t225 * t2472;
  t2393 = t3698 + t1379;
  t2378 = t1851 * t2500;
  t2376 = 0.24890000000000000000e-2 * t3204;
  t2374 = t1852 * t2558;
  t1473 = t1852 * t2555;
  t2370 = t1852 * t2484;
  t2368 = t1853 * t2532;
  t2366 = t1853 * t2501;
  t2365 = t1854 * t2480;
  t2363 = t1855 * t2488;
  t2359 = t1855 * t2542;
  t2358 = t1854 * t2531;
  t2357 = t1858 * t2499;
  t2355 = t1854 * t2504;
  t2352 = t1860 * t2574;
  t2351 = t1860 * t2489;
  t2349 = t1862 * t2476;
  t1869 = q_state_dot(3);
  t1271 = t2170 * t1861;
  t1993 = -t3330 - t2339 - t3320;
  t1943 = t1852 * t2459 + t633 * t1853 + t1859 * t1993 - t1271 + t2554 - 0.24178658687700000000e-2;
  t1996 = -t1854 * t2091 + t1861 * t3482;
  t1999 = t1166 + t1070;
  t2289 = -t1699 - 0.1e1 * t1157;
  t2012 = t3057 * t1859 - t1271 + (t2289 + t3222) * t1854;
  t2124 = -t2487 + t1716;
  t2035 = -t2124 + 0.52863517876992000000e-1;
  t2179 = -t2336 + t3496;
  t2217 = t1861 * t633;
  t661 = t2231 - t3291;
  t1902 = (t1846 * t2217 + t1853 * t2012 + t1860 * t1996 + t1861 * t976 + t3497) * t3438 + 0.50000000000000000000e0 * t1943 * t3191 + (t2179 * t1853 - 0.1194710953979893e-2 * t1845 + t2035 * t1859 + t3466 * t1861 - 0.1e1 * t3292 + t1999 * t1852 + 0.29682175996164750000e0 * t1854 + t661 * t1846 + t3471) * t3444;
  t533 = t1854 * t686 + t3615;
  t2109 = t533 * t1859 - t2572 + 0.46305794820080000000e-2;
  t975 = t1192 * t1853 - 0.11357396418885000000e-1;
  t812 = -t975 * t1852 - 0.5437511053345940e-2 * t1853 - 0.24178658687700000000e-2;
  t966 = -0.52863517876992000000e-1 - t3322;
  t877 = t966 * t1854 + 0.56786982094425000000e-2;
  t156 = t2109 * t1860 + t877 * t1859 - 0.1e1 * t3331 - t3304 + 0.12908973617152500000e-1 + (t1860 * t812 + t2436) * t1854;
  t2305 = -0.21934364256329280000e-2 * t1851 + t2508;
  t1188 = 0.22044137530701260e-1 + t2305;
  t2167 = t1188 * t1845 - t2127 - 0.8968493211292842e-2 + t3568;
  t257 = t1852 * t686 + t1859 * t975 + t1860 * t2167 + t2467;
  t637 = t755 + t3616;
  t1975 = t1859 * t637 + t3650;
  t2184 = t1193 * t1859 + t2393 - t2522;
  t283 = t1853 * t1975 + t1860 * t2184 + 0.1644487577369270e-2;
  t642 = -t3725 + 0.5437511053345940e-2 + t3290;
  t649 = -t1853 * t858 + t1146;
  t675 = t1145 * t1853 - t882;
  t726 = t3321 + t1146 * t1853 + 0.58416762559717300000e0;
  t1029 = t1193 + t2563;
  t842 = t1029 * t1852 - 0.12089329343850000000e-2 * t1853 - 0.6624110552949070e-2;
  t1932 = (t257 * t3077 + ((t812 + t3396) * t1860 + t966 * t1859 + t2436) * t1847 - t156 * t1854 + (-t1145 * t3172 - t1271) * t1860 - t1859 * t2487 + t726 * t1861) * t3444 - t283 * t3197 / 0.2e1 + (t842 + t1846 * t642 + t675 * t1859 + (t649 + (-t3043 + t3391) * t1853) * t1860) * t2917;
  t30 = t1902 + t1932;
  t2207 = t2265 * t1854;
  t2047 = t1861 * t2737 - t2207;
  t2216 = t1863 * t2281;
  t2277 = t3719 * t3181;
  t1880 = -0.1e1 * t1853 * t2216 * t2967 + (t1853 * t560 * t2976 - 0.1e1 * t1935 * t1854 + t699 * t3007 + t701 * t3190 + (t370 * t3077 + (t3168 * t699 + t3570) * t1847) * t1862) * t3443 - 0.1e1 * ((t1861 * t2227 - 0.1e1 * t3681 - t2278) * t1864 + t2277) * t2635 - 0.1e1 * (t1864 * t2329 - t2973 * t3671) * t2631 - 0.1e1 * t2074 * t2617 - 0.1e1 * ((t3588 * t3157 + (-0.1e1 * t1329 + t3369) * t1856) * t1857 + t3588 * t3156) * t2629 - 0.1e1 * ((t3157 * t3587 + t2233) * t1857 + t3587 * t3156) * t2620 - 0.1e1 * (-t3181 * t3671 + t2031) * t2627 - 0.1e1 * ((t1861 * t2228 + t2047 * t3157 + 0.1e1 * t3681) * t1857 + t2047 * t3156) * t2637 - 0.1e1 * (t1863 * t2277 - t1864 * t2390) * t2639 + (t561 - 0.1e1 * t3401) * t2983 + (-0.50000000000000000000e0 * t1847 + t3459) * t1863 * t1969 + (-0.1e1 * t2643 * (-0.1e1 * t2207 + t3371) - 0.1e1 * t2633 * (-0.1e1 * t1854 * t2348 + t1861 * t2335) - 0.1e1 * t2625 * (-0.1e1 * t1854 * t2334 - 0.1e1 * t1801)) * (t1855 * t3153 + t3179) - 0.17939475000000000000e1 * t474 * ((0.53170000000000000000e-1 * t1854 - 0.1e1 * t2837) * t3156 + ((-0.1e1 * t2688 - 0.1e1 * t2884) * t1861 + (-0.10441900000000000000e0 * t1856 + t1863 * t2482) * t1854) * t1857) - 0.17939475000000000000e1 * t3580 * t734 - 0.17939475000000000000e1 * ((-0.1e1 * t1862 * t2542 - 0.1e1 * t2476 * t3159) * t1861 + (t1857 * t2482 + t2477 * t3159) * t1854) * t410 - 0.17939475000000000000e1 * t643 * (-0.1e1 * t2973 + t3154) * t1539 + (-0.1e1 * (t2973 - 0.1e1 * t3154) * t2622 - 0.1e1 * t3181 * t2617) * t1128;
  t1891 = ((0.1e1 * t3725 - 0.1e1 * t3480) * t3007 + ((t1017 * t3192 - 0.1e1 * t1192 * t3206 + (-0.1e1 * t3391 + t858) * t3190) * t1853 + (-0.1e1 * t1146 * t1855 - 0.1e1 * t2137) * t1861 + ((-0.1e1 * t3294 + t3142) * t1859 - 0.1e1 * t1160 * t1855 + t1852 * t3519) * t1854) * t1860 + (t3125 * t1861 - 0.1e1 * t488 * t3192 + (t1854 * t2289 + t3050) * t1855) * t1853 + ((t1782 + 0.1e1 * t3697) * t1861 - 0.1e1 * t1487) * t1859 + ((t3142 + t3294) * t1852 + 0.66241105529490700000e-2 * t1855) * t1861 + 0.16444875773692700000e-2 * t3193 + t1163 * t3161 + t2958 + (t1976 * t1846 + ((t2189 * t1859 - 0.5437511053345940e-2) * t1853 + (-0.1e1 * t3330 + t2521 + t1400) * t1859 + t2554 + t1393) * t1860 + t2195 + t3465 * t1853 - 0.1e1 * t2599 + t2503 - 0.50330438027992300000e0 * t1861 + t2313 * t1854 - 0.65338343552314821500e0) * t1862) * t3442;
  t6 = t1880 + t1891;
  t1292 = t1656 + 0.51602752476000000000e-3 * t1853;
  t1152 = t2305 + 0.22044137530701260000e-1;
  t426 = t1152 * t1845 + t1660 + t2612 + t3568;
  t1051 = t1378 * t1853 + 0.12763550042100000000e-2;
  t1395 = -0.18509920000000000000e-2 * t1853 + 0.70158000000000000000e-3;
  t634 = t1051 * t1858 + t1395 * t2847 + 0.27219646194675000000e-1 + (0.5826996021941340000e-3 - t1621) * t1853;
  t912 = t1161 * t1853 - 0.11357396418885000000e-1;
  t248 = 0.27752814537092170000e0 + t426 * t1860 + t912 * t1859 + t634 * t1852 + (-t1646 + t3473) * t1853;
  t813 = -t1785 + t2261;
  t443 = t1845 * t813 - t1607 + t3613;
  t814 = t1785 + t2259;
  t68 = t248 * t3460 + (t248 * t1861 + t1771 + t3716 - 0.28391278634449500000e0) * t3439 + (-0.80863245317250000000e-1 + t3730) * t3447 + (t443 * t1846 + t628 * t3168 - t2503 + 0.54739070019494380900e0 + t2896 - 0.1e1 * t900 * t1860 - 0.1e1 * t814 * t1845 - 0.1e1 * t3001 - 0.1e1 * t1612 - 0.1e1 * t1292 * t1858 - 0.1e1 * (0.11198654185125000000e-1 - 0.1e1 * t1657) * t1853) * t3198;
  t2323 = t1869 * t68 + t1870 * t30 - t1871 * t6;
  t2320 = -t1806 - 0.1e1 * t3240;
  t2030 = t1862 * t2673 + t2194;
  t2060 = (t1855 * t2673 + t2425) * t1864;
  t2254 = -t1312 * t1854 + t1861 * t2838;
  t2063 = (-t1537 * t3201 + t1855 * t2254) * t1864;
  t2066 = t1855 * t2090;
  t2095 = t1862 * t2254 + t3030;
  t2165 = (t1861 * t2681 + t3634) * t1855;
  t1881 = (((t1043 * t3079 + 0.2e1 * t3045) * t1860 + (t3714 + t3317) * t1853) * t3214 + ((-0.1e1 * t3724 + t3653) * t2772 + 0.2e1 * t1142 * t2779 + t3509 * t3197 + ((-0.1e1 * t3679 + t3332) * t1860 + t3589) * t1855) * t1861 + t3610 * t3010 + (t2717 * t2986 + (-0.1e1 * t1040 * t3083 + 0.2e1 * t3002) * t1862) * t1860 + t2817 * t3193 - 0.1e1 * t3201 * t3332 - 0.73000000000000000000e-3 * t2970 + (t2457 * t3193 + t3590) * t1859) * t3443 - (t1857 * t2030 + t1863 * t2060) * t2643 + t2716 * t2946 - ((t1011 * t3187 + t1863 * t2191 + t3184 * t3516) * t1864 + t3063 + t1857 * t2165) * t2635 - (t1857 * t2095 + t1863 * t2063) * t2633 - ((-t3544 - t2066) * t1864 + t3514 * t3178) * t2631 - ((t2095 * t1863 + (t1854 * t2838 + t3233) * t1856) * t1857 + t2063) * t2629 - (t2152 + (t1862 * t902 + t2165) * t3178) * t2639 - ((t2030 * t1863 + t2320 * t3184 + (-0.1e1 * t1257 * t1852 - t2867) * t1856 * t3167) * t1857 + t2060) * t2637 - ((((-0.1e1 * t3028 - 0.1e1 * t3235) * t1862 - t2066) * t1863 + (-0.1e1 * t3029 + t3233) * t1856) * t1864 + t3514 * t1857) * t2627 + ((-0.2e1 * t3045 + t3080 * t1043) * t1860 + (-0.1e1 * t3317 - t3723) * t1853) * t2763 + t2431 * t2953 + t3610 * t2780 / 0.2e1;
  t2149 = t1861 * (-t2641 + t1263 - 0.1e1 * t1411);
  t1924 = (((-t1091 - 0.1e1 * t1275 + (-0.1e1 * t1061 - 0.1e1 * t1070 + t2515) * t1855) * t1853 + (t920 * t1862 + (-t2532 - 0.1e1 * t1412) * t3191) * t1861 + (t1862 * t919 + t3697) * t1854 + t921 * t1862) * t1852 + ((-t1855 * t2486 + t1489 + t751) * t1859 - t806 * t3190) * t1853 + (-t1491 * t1854 + (t3542 + t3685) * t1862 + (-0.1e1 * t1408 * t1854 + t1860 * t2149) * t1855) * t1859 + t806 * t3165) * t3442;
  t16 = t1881 + t1924;
  t1974 = -t3381 + t3542;
  t1090 = t1185 * t1860;
  t1980 = (-0.1e1 * t3328 - t1090) * t1861 + t2040 * t1853;
  t2236 = -0.26431758938496000000e-1 * t1853 - t3379;
  t2015 = t1853 * t2461 + t1861 * t2236;
  t2264 = t1272 + t3617;
  t2058 = t1860 * t2264 + t2460;
  t2093 = -0.1e1 * t1402 * t1853 + t2175;
  t2181 = t2230 * t1861;
  t2287 = -t2532 - 0.1e1 * t1408;
  t1909 = (((-0.56786982094425000000e-2 - t3319) * t1861 - t3296 + t2058) * t1852 + (t1974 + t3685) * t1859 + t806 * t1860) * t3445 + (t1980 * t1852 + t2015 * t1859 + t1853 * t2181 + (t1852 * t2093 + t1859 * t2287) * t1854) * t3437;
  t1071 = t1145 * t1859;
  t499 = -t1070 + t638;
  t516 = -t1155 * t1853 + t1854 * t675;
  t677 = t2340 + t3381;
  t905 = t1193 * t1853 + t2460;
  t1913 = ((t2856 + t3396 + ((t1188 * t3462 - t636) * t1860 - t975) * t1852) * t1847 + ((t2679 + t2855) * t3217 + (-0.1e1 * t533 * t1852 + (-t1854 * t975 - 0.21751134959804000000e-1) * t1859) * t1860 + t930 * t2820 - t3050 - t877 * t1852 + (-t1080 + t2822) * t1854 - t1071) * t1861 + (-t2355 + (-t499 + 0.2e1 * t3293) * t1852 + t3361) * t1860 - t905 * t1852 + t1155 * t3174 + t677 * t1859) * t3444 + t516 * t2941 + ((-0.1e1 * t1193 * t1852 + t3696) * t1860 + (t3390 - t1769 + (-0.2e1 * t3293 - 0.1e1 * t637) * t1852) * t1853) * t2917 + t3728 * t2768 - t2483 * t3202 + t1029 * t1854 * t2925 + ((-0.2e1 * t799 - 0.23894219079597860000e-2) * t3208 + t3079 * t1189) * t2772 / 0.2e1;
  t38 = -t1909 + t1913;
  t97 = ((t3078 * t813 + t2679) * t1846 + t657 * t3168 + t3093) * t3459 + ((t2856 + t634 * t1859 + ((t1152 * t3462 - t636) * t1860 - t912) * t1852) * t1861 + t3092) * t3446 + (-t1860 * t3520 + t3078 * t814 + t2815) * t3453 + t2785;
  t2316 = -t16 * t1871 + t1869 * t97 + t1870 * t38;
  t466 = ((-0.21934364256329280000e-2 * t1858 - t2577) * t1845 + ((-t1382 * t1851 - t2524 + t3128) * t1852 + t1283) * t1859 + t1286) * t1860;
  t100 = (t3168 * t651 + t2849 + t3098) * t3459 + ((t466 + t2127 * t3202 + (t1395 * t2841 - 0.1e1 * t1051 * t1851) * t1852 + ((t1851 * t2513 + t1612) * t1852 - 0.1e1 * t1653 - 0.1e1 * t1725) * t1853) * t1861 - t3260) * t3446 + (-t1292 * t1851 - t1853 * t2521 - t1112 + t3128 + t3358) * t3453 + t3538 * t3439 + t1851 * t2516 - t2607 + 0.39510871831575200000e-3 * t1837;
  t2042 = (t1855 * t2428 - t2426) * t1864;
  t2096 = t3584 * t1855;
  t1886 = (((-t3074 + t3282 - 0.1e1 * t1308) * t1860 - 0.1e1 * t1339 + (t2068 + t3278) * t1853) * t3214 + (-t3638 * t2772 + t999 * t2779 + (-t3700 + t2330) * t3197 + t3467 * t1855) * t1861 - t3638 * t3010 + (t548 * t2986 + (-0.1e1 * t3263 - t3677) * t1862) * t1860 + t2039 * t3193 - 0.1e1 * t2131 * t2970 + t1858 * t2377 * t3211 + t3648 * t1862 * t2376) * t3443 - 0.1e1 * (t1863 * t2042 + t2018) * t2643 + (t2754 - 0.1e1 * t3366) * t2946 - 0.1e1 * ((t2171 * t1863 + (-0.1e1 * t1854 * t2413 - 0.1e1 * t3020) * t1856) * t1864 + t3064 + t1857 * t2096) * t2635 - 0.1e1 * (t2138 + (t1862 * t901 + t2096) * t3178) * t2639 - 0.1e1 * (t2005 + t2042 + (t3020 + t3576) * t3180) * t2637 - 0.1e1 * t1863 * t2381 + t396 * t2763 - t3427 * t2953 + 0.42800000000000000000e-3 * t3648 * t1863;
  t2271 = t1853 * t2370;
  t2273 = t1852 * t2351;
  t1900 = ((((-t2156 * t1861 + (0.1200936784896e-2 - t2714) * t1862) * t1859 + t1855 * t2645 - t2447 + t1360) * t1860 + (-t1855 * t2701 + (-t1855 * t2708 + t1361) * t1853) * t1859 + (t1359 * t1853 - t2452) * t1861 + (t1852 * t2156 - t1853 * t2705) * t1854 + t1853 * t2644 + t2452) * t1858 + (((-t1359 * t1861 + t1527 - t2703) * t1859 + t1855 * t2646 - t2448 - t1361) * t1860 + (t1244 + (t1853 * t2707 - t2702) * t1855) * t1859 + (-t1246 + t2451) * t1861 + (t1359 * t1852 - t1853 * t2706) * t1854 + t2752 * t3201 - t2451) * t1851 + t1855 * t2273 + t1855 * t2356 + t2271) * t3442;
  t27 = t1886 + t1900;
  t1195 = t3097 * t1853;
  t2223 = (-0.1e1 * t993 - t3358) * t1853;
  t652 = t3276 + t3388;
  t669 = t1853 * t829 + t1311;
  t671 = -t2522 + t3572;
  t1905 = ((t1852 * t669 - t1200 + t466) * t1847 + (t3173 * t3600 - t3274) * t1861 + ((-t1197 + t668) * t1859 - t2806) * t1860 - t3274 + (t3266 + (0.1e1 * t2127 * t1847 - t3100) * t1859 + t2848) * t1853 + (((t1859 * t669 - t2127 * t3204) * t1860 + (-t1447 + t3109) * t1845 + t3036 + 0.1e1 * t1196 - t1205 + 0.15804348732630080000e-2 * t1837 + t2849 - t3128) * t1861 - 0.1e1 * t3600 * t1852 - 0.1e1 * t1300 * t1853) * t1854) * t3444 + ((t1853 * t3099 + t830) * t1854 + t3600 * t1853) * t2925 + ((t2223 - t1300) * t1854 - t1301) * t2921 + (t3596 * t1860 - t1195 + (t1859 * t671 - t1194) * t1853) * t2917 + t652 * t2768 - t2936 * t3271;
  t1392 = 0.38400000000000000000e0 + t2569;
  t1508 = t1859 * t2490;
  t2024 = t1392 * t2743 - t1508 - t2557 + 0.24444132201840000000e-2;
  t2244 = -t1853 * t2492 + t1473;
  t1171 = 0.38400000000000000000e0 * t1861 - t2549 + 0.31600000000000000000e0;
  t925 = -t1171 * t2886 + 0.92549600000000000000e-3 * t1854;
  t1959 = t1860 * t2024 + t2840 * t925 + t2244;
  t1507 = t1859 * t2492;
  t2025 = t1392 * t2744 + t1507 - t2559 + 0.98827089590400000000e-3;
  t2243 = -t1853 * t2490 - t2374;
  t923 = t1171 * t1809 + 0.37417600000000000000e-3 * t1854;
  t1960 = t1860 * t2025 + t2840 * t923 + t2243;
  t1406 = 0.31600000000000000000e0 * t1854 - 0.82500000000000000002e-1;
  t2161 = 0.7735484874e-2 * t1406 + t2491;
  t2162 = -0.3127439544e-2 * t1406 - t2493;
  t1006 = -t1180 + t2569;
  t2163 = 0.7735484874e-2 * t1006 - t2505;
  t2164 = 0.3127439544e-2 * t1006 + t2506;
  t2177 = t1180 * t2745 + 0.16724826617837780000e-2;
  t2178 = -t1180 * t2746 + 0.54835910640823200000e-3;
  t1907 = ((t1851 * t2177 + t1858 * t2178) * t1860 + (t1851 * t2164 + t1858 * t2163) * t1853 + (t1851 * t2161 + t1858 * t2162 + t2565) * t1852) * t3445 + (t1851 * t1960 + t1858 * t1959 + t2273 + t2356) * t3437;
  t45 = t1905 - t1907;
  t2304 = t100 * t1869 + t1870 * t45 - t1871 * t27;
  t603 = t1846 * t628;
  t105 = (-0.1e1 * t1839 * t628 + t3075 * t443 + t603) * t3459 + (-0.1e1 * t426 * t1853 + t1161 * t3173) * t3475 - 0.1e1 * t3453 * t3574 - 0.1e1 * t3372 * t3439 + (((-0.1e1 * t1621 - 0.1e1 * t2589 + t3257 + 0.5826996021941340000e-3) * t1852 - 0.1e1 * t1646 + t3473) * t3475 - (-0.1e1 * t3453 + t3439) * t2336) * t1860;
  t2183 = t1861 * t1010;
  t1988 = (t1855 * t2183 - t3342) * t1864;
  t2027 = t1862 * t2183 + t3343;
  t2084 = t1303 * t3162 + t2199;
  t2205 = (t1303 * t3190 - t2198) * t1864;
  t2213 = t2562 - 0.1e1 * t1208;
  t1879 = t560 * t2780 + ((t1387 * t3191 + 0.2e1 * t3738 + t2787) * t1861 + t699 * t2684 + t3737 + t2853 * t3165 + t3673 * t3169 + (-0.1e1 * t2092 * t3214 - 0.1e1 * t1962 * t1861 - 0.1e1 * t1995) * t1853 + ((-0.1e1 * t2067 + t2783) * t3214 + (-0.1e1 * t2364 + t2776 - 0.1e1 * t2981) * t1861 + t2959) * t1860) * t3443 - (t2143 + (t2424 + t3069) * t3153) * t2643 - ((t2293 + (t1853 * t2320 + t3229) * t3187) * t1864 + t749 * t3179 - t1857 * t2241) * t2635 - (t1857 * t2027 + t1863 * t1988) * t2633 - ((t1855 * t2229 - t3624) * t1864 + (t1862 * t2229 + t3039) * t3178) * t2631 - (t1857 * t2084 + t1863 * t2205) * t2625 - (t2157 * t1864 + (t2198 - 0.1e1 * t3026) * t3178) * t2622 - (((-0.1e1 * t3624 + t2213 * t1855) * t1863 - 0.1e1 * t3041) * t1864 + (t1862 * t2213 + t3039) * t1857) * t2627 - ((t1010 * t3187 + t1863 * t2027) * t1857 + t1988) * t2629 - ((t1863 * t2084 + t3025) * t1857 + t2205) * t2620 - (t1863 * t2112 + t1864 * t2432) * t2639 - (t2111 + ((-0.1e1 * t3230 + t3116) * t1862 + t3069) * t1864 + (-0.1e1 * t1203 + (-0.1e1 * t1257 * t1859 + t1806) * t1853) * t2974) * t2637 - (t2199 * t3153 + t1857 * t2198 + ((t1861 * t3157 + t3187) * t1864 - 0.1e1 * t2962) * t1538) * t2617 + t1839 * t2216 * t3459 + t1846 * t1863 * t2188 + (-0.1e1 * t2019 * t1853 + (t2038 + t3316) * t1860) * t2763;
  t2036 = t2124 - 0.26431758938496000000e-1;
  t1911 = ((-t911 * t3193 + (t2976 + t3201) * t1154) * t1845 + (t1016 * t1853 + ((-0.1e1 * t3067 - 0.1e1 * t647) * t1860 - 0.1e1 * t3049 + t1024) * t1855 + (t2287 * t1860 + (t2185 + t755) * t1853) * t1862) * t1859 + (t2341 * t3715 + t1146 * t3197 + (-0.1e1 * t3559 - 0.1e1 * t897) * t1855 + (t2175 * t1852 - 0.1e1 * t2522 + t1379) * t1862) * t1860 - t1855 * t3054 + (-0.1e1 * t882 * t3190 + t2036 * t1862) * t3204 + (-0.1e1 * t646 * t1855 + (t2100 - t1732) * t1862) * t1853 - t1132 * t3193) * t3442;
  t12 = t1911 + t1879;
  t2017 = (t649 + (t3391 - 0.1e1 * t3043) * t1853) * t1854 + t2341;
  t2064 = t1859 * t499 - t3248 - t3650;
  t1895 = t2483 * t3169 + t642 * t2772 + ((-0.1e1 * t2167 * t1853 + t1066 + t3728 * t1860) * t1847 + (t437 * t2819 - 0.1e1 * (t1854 * t812 + t2109) * t1853 + (-0.45033756566424900000e-2 * t3168 - t1057) * t1854 + (t889 * t2971 + (-0.1e1 * t3290 - 0.5437511053345940e-2) * t3167 - t2341) * t1860) * t1861 - 0.1e1 * t2064 * t1853 + t1193 * t3173 + t1146 * t3167 + t3694 - 0.1e1 * t1160 * t1860) * t3445 - 0.23152897410040000000e-2 * t3165 + t2017 * t2938 + (-0.1e1 * t1189 * t2777 - t858 * t3167 + t3013 * t799 + t3536 * t1859) * t2922 - 0.50000000000000000000e0 * (-0.1e1 * t2184 * t1853 + t1975 * t1860) * t3162 - 0.50000000000000000000e0 * t2137 * t3167;
  t423 = t3363 - t3605;
  t337 = t1860 * t423 + t2683;
  t430 = t755 - t1087 + t2264;
  t382 = t1853 * t430 - t1090;
  t441 = -t1396 * t2748 + t1401 + t3249 + t3315 - t3692;
  t446 = -t1399 * t2748 + t2393 - t3249 + t3302;
  t691 = -t3559 - t897;
  t1170 = t1716 + t2168;
  t702 = t1170 * t1852 - t3100 + t3592;
  t1947 = (t609 * t1845 + t441 * t1853 + t337 * t1859 + t691 * t1860 + (-0.1e1 * t3348 - t1132) * t1854) * t3437 + (t1853 * t702 + t1860 * t446) * t3445 - t382 * t3192 / 0.2e1 + t1154 * t1855 * t2949;
  t35 = t1895 + t1947;
  t2302 = t105 * t1869 - t12 * t1871 - t1870 * t35;
  t2301 = 0.3507900e-3 * t3669;
  t2300 = 0.8676525e-3 * t3669;
  t2292 = -0.2e1 * t3322 - 0.26431758938496000000e-1;
  t2291 = -0.1e1 * t3319 - 0.56786982094425000000e-2;
  t2283 = t1727 - 0.1e1 * t1390;
  t2272 = t2480 * t3207;
  t2270 = t1854 * t2370;
  t2269 = t1854 * t2385;
  t2268 = t1859 * t2365;
  t2245 = t3596 * t3440;
  t2218 = t1853 * (-t2531 - 0.1e1 * t1402);
  t2215 = t2287 * t1852;
  t2208 = t1860 * t3598 - t1071 - t2170;
  t1868 = q_state_dot(4);
  t949 = t1619 - t1785 - t3581;
  t198 = 0.1e1 * t628 * t2608 + (-0.1e1 * t1607 + (t949 - 0.1e1 * t1190) * t1845 + t3613) * t3168 + (-t1860 * t628 + t2336) * t3476 - 0.50000000000000000000e0 * t3574;
  t2187 = 0.2e1 * t2246 * t1853;
  t1890 = t633 * t2771 + (t1846 * t1952 - t1853 * t1930 + t1860 * t1936 + t1953 * t3075 + t2187 * t3191) * t3443 + t1983 * t2937 + t2120 * t2920 + t3598 * t1846 * t2916;
  t481 = t1070 + t3363;
  t1912 = (((-0.1e1 * t3330 + (t3616 - 0.1e1 * t756) * t1854) * t3165 + t2781 + (t1145 * t3190 + (t1155 * t1855 + t1091) * t1854) * t1853) * t1859 + t3496 * t3191 + (t2363 + (-0.1e1 * t3695 + t2545) * t1854) * t3204 + t3606 * t3194 + t1132 * t3162 + (t2280 + (t1777 + t2650) * t1860 + t2964 + t2814 * t1853) * t1862) * t3442 + t1132 * t2916 + (t1852 * t3089 + t3088) * t2919 + t609 * t2948 + (t1860 * t481 + t2683) * t2924 + t3495 * t2937 + t1863 * t2769 - t2765 * t3378;
  t33 = t1890 + t1912;
  t1916 = t661 * t1853 * t3165 + (-t1853 * t1996 + t1860 * t2012 + t2217 * t3075 + t3216 * t3598) * t3445 - t633 * t3215 / 0.2e1 + t1943 * t2938 + (t2187 + t2179) * t2922;
  t1305 = t2488 + t2552;
  t1501 = t1861 * t1736;
  t1923 = ((-t1388 * t1861 + t1501 - t3303) * t1860 + (t1305 * t1852 + t3606) * t1853) * t3437 + (-0.1e1 * t3048 * t1845 + ((t3124 - 0.1e1 * t3364) * t1860 - 0.1e1 * t3044 - 0.1e1 * t1017) * t1859 + (-t1777 - 0.1e1 * t2650) * t1860 + (t3702 - 0.1e1 * t1160) * t3199 - 0.1e1 * t2964 + (-t911 * t1845 + t3492 * t1853 - 0.1e1 * t1788 + t1369) * t1861) * t3444 + (t3124 + t3320) * t2762;
  t50 = t1916 + t1923;
  t475 = t1853 * t2308 + t1860 * t637;
  t1934 = (t475 * t1859 + (t3222 - 0.1e1 * t3523) * t1860 + (-t3698 + t3490) * t1853) * t3439 + (t1853 * t2288 + t1132) * t3447 + (t1716 * t1852 - t2556) * t3440 + t2769 - t911 * t3220 / 0.2e1 + (t1145 * t1860 - t3322) * t2927;
  t424 = t3400 + t2818;
  t1944 = (-0.1e1 * t3598 * t1839 + t2208 * t1860 + (t3641 * t628 + t1146) * t1853) * t3447 - t424 * t3166 / 0.2e1 + t2091 * t2918;
  t74 = t1934 + t1944;
  t2202 = t1868 * t198 - t1869 * t74 - t1870 * t50 - t1871 * t33;
  t220 = -0.1e1 * t2815 * t2608 + t1699 + (-0.10000000000000000000e1 * t949 * t1839 - 0.1194710953979893e-2) * t3208 + ((t3313 + 0.1e1 * t3727) * t1853 - 0.1e1 * t3520) * t3476 + (-0.10000000000000000000e1 * t1846 + 0.1e1) * t3042 + 0.50000000000000000000e0 * t1482 * t1846 - 0.50000000000000000000e0 * t1080;
  t2145 = t757 + (0.26431758938496000000e-1 + 0.2e1 * t3322) * t1859;
  t524 = t3078 * t931 + t2815;
  t958 = t1154 * t3011;
  t1901 = ((t1161 * t2969 + (t889 * t3715 + (0.2e1 * t1190 - 0.23894219079597860000e-2) * t3192) * t1852) * t1846 + ((-t1192 * t3192 - t1852 * t2033 - t958 + (-t1482 + t2855) * t3162) * t1853 - t2206 * t1852 + t751 * t3174 + (-t2353 + t1771) * t1855) * t1860 + t524 * t3225 + (-0.1e1 * t488 * t1852 + t2353 + t2145 * t1854) * t3201 + t1855 * t1482 - t2061 * t1852 + t738 * t3172 + t1145 * t2978 + 0.2e1 * t1163 * t2980 + t1166 * t3192) * t3442 + (-0.1e1 * t3360 * t1852 - t2355 + t2145 * t1861) * t2937 + (t3199 * t452 + t2721) * t2919 + t1185 * t2761 + t657 * t2767 + t882 * t2764;
  t1910 = ((-t1854 * t2113 + t1861 * t2078 + t3201 * t3539) * t1852 + (-t1304 * t3171 - t3197 * t806) * t1853 + ((-0.1e1 * t1004 * t1854 + t3649 * t1861) * t1855 + (t2308 * t1861 - 0.1e1 * t1854 * t2150) * t1862) * t1859) * t3442 + (t1861 * t2006 - t3295) * t2924 + (t1859 * t3089 + t2181) * t2937 + ((-t1061 - t1070) * t1853 + t882 * t1854 + t1861 * t2253) * t3205 / 0.2e1;
  t36 = t1901 - t1910;
  t1908 = (t524 * t1839 - 0.1e1 * t2035 * t1852 + (-0.1e1 * t1087 + (0.2389421907959786e-2 - 0.2e1 * t1190) * t1852 + t1999) * t1859) * t3437 + (t657 * t3216 + ((t1018 - 0.1e1 * t1154 * t3226) * t1853 + t3066 + (t3295 + (-0.2e1 * t801 + 0.23894219079597860000e-2) * t1859 * t3163) * t1852) * t1860 + (-0.1e1 * t3057 * t1852 - t2353 + (t1859 * t2292 + t3390) * t1854) * t1853 - t3692 + t2963) * t3444 + (-t1852 * t1993 + t1853 * t657 + t1859 * t2459 - t2353) * t2921 + (-t1482 + t2822) * t2947;
  t1920 = ((-0.1e1 * t2291 * t1854 + t3124 * t1860) * t1852 - 0.1e1 * t1004 * t3174) * t3437 + (-0.1e1 * (-0.1e1 * t1090 - 0.1e1 * t3328) * t3209 - 0.1e1 * t2236 * t3174 - 0.1e1 * t1853 * t2182) * t3444 + ((t1859 * t3649 - 0.1e1 * t2572) * t3437 + ((t2218 + t2175) * t1852 + (t2287 + t2563) * t1859) * t3444) * t1861;
  t54 = t1908 - t1920;
  t2082 = t2260 - t1769;
  t2023 = -0.1e1 * t3616 * t1852 - t3251 + t2082;
  t1937 = (t2023 * t1853 + (-0.1e1 * t1088 - t3696) * t1860) * t3439 + ((-t1272 - t2358) * t1852 + t2355) * t3448 + t1185 * t2928 - t2786;
  t93 = -t1937 + t3479;
  t2201 = t1868 * t220 + t1869 * t93 + t1870 * t54 + t1871 * t36;
  t1994 = t1794 * t3505 + t2574 - t3269;
  t1926 = (-0.8676525e-3 * t1858 - 0.3507900e-3 * t1851) * t1854 * t2494 + (t1280 * t2366 - 0.1e1 * t1851 * t2567 + t1860 * t1994 - 0.1e1 * t2368) * t3439 + (-0.1e1 * t1643 * t2847 - 0.1e1 * t1644 * t2841 + 0.49096519673609460000e-2) * t2927 + (t2528 - 0.1e1 * t2597) * t3209;
  t2016 = ((t1860 * t490 - t3272) * t1853 + t651 * t1846 + t1300 * t1860 + t3567) * t3446;
  t101 = -t1861 * t2245 + t2918 * t480 - t1926 + t2016;
  t253 = t3659 / 0.2e1 + (t1860 * t652 + t3101) * t3448 + (t993 + t3277) * t3454 + t1311 * t2926 + t1196 / 0.2e1 - t1204 / 0.2e1;
  t1893 = t2268 + t1860 * t2272 + ((((t1361 * t1854 - t2446) * t1859 + (t1854 * t2751 + t2709) * t1862) * t1860 + (t1644 * t2836 - 0.1200936784896e-2 * t3199) * t3171 - t2299 * t1854 + t1998 * t1861) * t1858 + (((t1360 * t1854 + t2445) * t1859 + (t1854 * t2752 + t2710) * t1862) * t1860 + (t1643 * t2836 + 0.2970426191616e-2 * t3199) * t3171 - t2224 * t1854 + t1997 * t1861) * t1851 + t1860 * t2270 - t1859 * t2350) * t3442 + ((t1507 + t2158) * t1860 + (-t1643 * t1854 + 0.4038528e-2 * t3163) * t2840 + t2243) * t2943 + ((-t1508 + t2645 - t2713) * t1860 + (-t1644 * t1854 - 0.1632768e-2 * t3163) * t2840 + t2244) * t2929;
  t1897 = (((t3388 + 0.1e1 * t3276) * t3162 + (-0.1e1 * t1447 - 0.1e1 * t3277 + 0.790217436631504e-3 * t3648) * t1855) * t1846 + (t3137 * t3174 + ((t3269 + t2788) * t1854 + (t2223 - 0.1e1 * t1300) * t1861) * t1862 + (((0.4841887557042460e-2 * t1844 - 0.1e1 * t1733 + (t2513 - 0.1e1 * t1415) * t1851) * t1859 - t3276) * t1853 + t3655 * t1859) * t1855) * t1860 - t3498 * t3225 + (t1286 * t3012 + (t1854 * t668 + t1198) * t3171 - t1300 * t3190 + (-t1855 * t2591 + t1862 * t3097 - t1495) * t1854 + t1855 * t2596 + t1490) * t1853 + t830 * t2969 + (t3137 - t3267) * t3207 + t3099 * t2995 - t3098 * t3196 + t1283 * t3195) * t3442 + (-t1197 * t1859 + t1861 * t480) * t2937 + (t1854 * t3654 - t1861 * t3596) * t2919 - t3100 * t2764 + t651 * t2767 - t830 * t2761;
  t40 = -t1893 + t1897;
  t1898 = (((0.63817750210500000002e-3 * t1851 - 0.25801376238000000001e-3 * t1858) * t1861 + t2088) * t3173 + ((-0.24444132201840000000e-2 * t1854 - t2491) * t1858 + (-0.98827089590400000000e-3 * t1854 - t2493) * t1851) * t1853 + ((-0.98827089590400000000e-3 * t1861 + t2559) * t1858 + (0.24444132201840000000e-2 * t1861 - t2557) * t1851) * t1852) * t3437 + (((-t2491 + (-0.7735484874e-2 * t1392 + t2505) * t1854) * t1860 + (0.16327680000000000000e-2 * t3199 + (0.35079000000000000001e-3 * t1853 + 0.92549600000000000000e-3) * t1861) * t2840 + t2076) * t1858 + ((-t2493 + (-0.3127439544e-2 * t1392 - t2506) * t1854) * t1860 + (-0.40385280000000000000e-2 * t3199 + (-0.86765250000000000002e-3 * t1853 + 0.37417600000000000000e-3) * t1861) * t2840 + t2075) * t1851 - t1854 * t2352 + t1859 * t2489) * t3444;
  t1206 = t1300 * t1861;
  t747 = t828 * t3209;
  t1922 = (-t3659 + (t1301 * t1854 - t1206 - t3101) * t1853 - t1196 + (t2455 + t1283) * t1852) * t3437 + (t651 * t3216 + (t1854 * t3596 + t1861 * t3654) * t1860 + ((-t747 + t3535) * t1859 + t2806 * t1854) * t1853 - t830 * t3172 + t3100 * t3207) * t3444 + (t651 * t1853 + (t3655 + t2088) * t1859) * t2921 + (t2901 - t3277) * t2947;
  t60 = -t1898 + t1922;
  t2193 = t101 * t1869 + t1868 * t253 + t1870 * t60 + t1871 * t40;
  t1499 = t1854 * t1736;
  t2173 = t1399 * t2749 + t1499 - t2522 + t3281;
  t2159 = 0.735522e0 * t1543;
  t1405 = 0.82500000000000000000e-1 * t3669;
  t2116 = t1405 * t2747 + t1273 - t1402;
  t1940 = (t2023 * t1860 + (t1088 + 0.1e1 * t3696) * t1853) * t3446 + (t1398 * t1859 + t1852 * t2116) * t3440;
  t1948 = t2782 + t1018 / 0.2e1 - t911 * t2972 + (t800 * t3219 - 0.1e1 * t475 * t1852 + (t1860 * t2292 - t3381) * t1859) * t3446 + (t1860 * t821 + t1017) * t3450 + t1398 * t3173 / 0.2e1;
  t103 = -t1940 + t1948;
  t1149 = -t1385 + 0.29704261916160000000e-2 * t1852;
  t1958 = (t1852 * t2308 + t3696) * t3440 + (t1149 * t1858 - t1390 * t1852 + t2082) * t3449;
  t2045 = -t2322 / 0.2e1 + t1185 * t2923 - t882 * t2926;
  t179 = t1958 + t2045;
  t1867 = q_state_dot(5);
  t1903 = ((t2204 * t1860 + ((t2515 - 0.1e1 * t1404) * t3194 - t1862 * t2368 - t1412 * t3201) * t1861 + t2218 * t3193 + t2283 * t3194) * t1852 + t2029 * t1860 + (t1855 * t2036 + t1862 * t2149) * t3202 - t806 * t3194) * t3443 + t2098 * t2920 + (t1860 * t2180 - t2411 * t3199) * t2940 + t2026 * t2654;
  t1929 = -t2429 * t1852 * t3170 + (-t2294 * t1852 + (-0.2e1 * t2141 * t1852 + t618 * t1860 + t1052 * t3197 * t3463 + t600 * t1853 + (t2966 * t802 + t563) * t1859) * t1859) * t3442 + t2303 * t2940 + t2919 * t3309 - t882 * t2654 + (t2782 + (t1154 * t1861 + t3167 * t800) * t3579) * t1863;
  t43 = t1903 + t1929;
  t431 = -t3222 / 0.2e1 + t3228 / 0.2e1 + (t1785 + t2258 - t1052) * t3208;
  t1921 = ((-t1090 + (t1087 - 0.1e1 * t1272 - t3617) * t1853) * t1852 + (t1853 * t2036 - t3379) * t1859 - t806 * t1853) * t3438 + (((t3296 - t3664) * t1861 + t3605 * t1860) * t1852 + ((-t2495 + t3381) * t1861 + t2461 * t1860) * t1859 + t1860 * t2181) * t3445;
  t1941 = -t1154 * t2778 + (-t337 * t1852 + (-t882 * t3163 - t1168 * t1860 + (-t1154 * t1854 + t3166 * t800) * t1859 + (-t1052 * t1854 - t609) * t3463) * t1859) * t3444 + t382 * t2941 + (t1170 * t1853 + t3379) * t2925 + t2938 * t3390;
  t64 = t1921 + t1941;
  t2140 = t103 * t1869 - t179 * t1868 - t1867 * t431 + t1870 * t64 + t1871 * t43;
  t1030 = -t2385 + t3098;
  t1111 = t1286 * t3207;
  t1925 = (t1860 * t2908 - 0.1e1 * t1111) * t3441 + t3439 * t2385 + (-0.1e1 * t1286 * t3219 + (t1860 * t671 + t3270) * t1859 - t3279 + t830 * t3204) * t3446 + 0.50000000000000000000e0 * t1030 * t3218 + t2784 + (0.12900688119000000000e-3 * t1851 + 0.31908875105250000000e-3 * t1858 + (-0.1e1 * t2531 - t2598) * t3439 - 0.1e1 * t1295 * t3446) * t1853;
  t1927 = (t1203 * t2501 - t1851 * t2499 - t1853 * t1994 - t1858 * t2500) * t3446 + t1544 * t1792 * t2560 + (t1851 * t2300 - t1858 * t2301) * t3441 * t2839;
  t133 = t1925 - t1927;
  t1525 = t1794 - t2867;
  t1931 = (-0.1e1 * t1525 * t1544 - 0.128686793e-3 * t1852) * t2494 - t2132 * t3449 + (-0.48150000000000000000e-2 * t1852 - 0.1e1 * t3630) * t3440 - t3491 * t1853 * t2420;
  t208 = t1860 * t3461 + t2923 * t830 - t2926 * t3100 - t1931 + t3061;
  t494 = (-0.136112442957540e-3 * t3212 + t3098) * t3579 - t3036 / 0.2e1 + t3059 + 0.68056221478770e-4 * t3212;
  t1991 = (t1380 - t2518) * t1851 + t2135;
  t1894 = 0.68056221478770000000e-4 * t3158 * t3212 + ((t1030 * t3197 + t1286 * t2412) * t1845 + (-t1493 * t1853 - t1494 * t1860 + ((-t1197 - t3600) * t1860 - 0.1e1 * t2988 + (t1860 * t668 - t3270) * t1861) * t1862 + (t2378 + (t2455 + t3572) * t1853) * t1855) * t1859 + (t1295 * t1855 - t1300 * t3193 - t1301 * t3190 + t1991 * t3195 + t3097 * t3162) * t1860 - t992 * t3016 - t2957 * t3699 + ((t1295 * t1861 - 0.1e1 * t1300 * t1854 - t1301) * t1862 - t3097 * t1855) * t1853 + t1862 * t2269) * t3442 + ((-t747 - t1207 + t2908) * t1860 - t1111 + t3100 * t3199) * t2924 + (t1030 * t1861 - t1286 * t3167) * t2948 + (-t1295 * t1854 - t1206 + t1300) * t2937 - t2915 * t3279 + t1863 * t2784 + t830 * t1854 * t2765;
  t1896 = ((-0.1e1 * t2115 * t1853 + (-t2156 + (t2708 - 0.1e1 * t2714) * t1862) * t3173 + t1360 * t3166) * t1858 + (-0.1e1 * t1978 * t1853 + (-0.1e1 * t1359 + (-0.1e1 * t2707 + t2713) * t1862) * t3173 - 0.1e1 * t1361 * t3166) * t1851 + t1861 * t2271 + t1855 * t2352 + ((-0.1e1 * t2447 + t2647) * t1858 + (-0.1e1 * t2448 + t2648) * t1851) * t1860) * t3442 + (-t1990 * t1853 + (t2300 + t2798) * t2690 - t1854 * t2499) * t2943 + (-t1989 * t1853 + (-t2301 - t2799) * t2690 - t1854 * t2500) * t2929 - t2365 * t3204;
  t51 = t1894 - t1896;
  t1915 = ((t1399 * t2750 + t1727 - t2358 - t3266 - t3699) * t1860 - t1195) * t3437 + ((-0.1e1 * t1286 * t3166 + (t2589 + (-0.55042935974400000000e-3 + t3643) * t1858) * t1854) * t1845 + ((t1499 - t3599) * t1860 + t2988 + ((-t779 - 0.1e1 * t1302) * t1860 + t3270) * t1861) * t1859 - t3097 * t3166 + (t1396 * t2750 + t1861 * t2788 + t2358 - t2515) * t1853 + t992 * t3227 - t2269) * t3444 + (-t3268 + (t2173 - t779) * t1853) * t2925 + t1286 * t1862 * t2949;
  t1917 = ((-0.1e1 * t2024 * t1858 - 0.1e1 * t2025 * t1851 - t1852 * t2489) * t1853 + ((-t1171 * t2746 - t2492) * t1858 + (t1171 * t2745 - t2490) * t1851) * t1860) * t3444 + ((-0.1e1 * t2178 * t1853 + t2163 * t1860) * t1858 + (-0.1e1 * t2177 * t1853 + t2164 * t1860) * t1851 + t2352) * t3437;
  t70 = t1915 - t1917;
  t2139 = t133 * t1869 + t1867 * t494 + t1868 * t208 + t1870 * t70 + t1871 * t51;
  t2087 = (0.39252000000000000000e-1 * t1855 - 0.27518000000000000000e-1 * t1862) * t1857;
  t2070 = 0.680722668912e-3 * t1858 + 0.275214679872e-3 * t1851 + 0.49096519673609460000e-2;
  t1933 = ((-0.28244044800000000000e0 * t1202 + t3268) * t1852 + t2070 * t3173) * t3446 + (t1851 * t2658 + t1858 * t2657 - 0.1e1 * t2489) * t3450 + (t2597 - 0.1e1 * t2528) * t3172;
  t1949 = ((t1302 * t1852 + t828) * t1853 - t3567 * t1860) * t3446 + (-t1405 * t2749 + t1501 - t1736) * t3204 / 0.2e1 + t3504 * t1861;
  t167 = -t1933 + t1949;
  t1866 = q_state_dot(6);
  t1928 = (-0.48150000000000000000e-2 * t1859 + t2089) * t3449 - 0.1e1 * (-0.647815649e-3 * t1852 * t1858 - 0.1e1 * t1806 * t2887 + (-0.374176e-3 * t1851 - 0.925496e-3 * t1858 - 0.128686793e-3) * t1859) * t2560 + t3491 * (0.384e0 * t3169 - 0.825e-1 * t1859);
  t1951 = -t3272 / 0.2e1 + t3567 * t3448 + (-t1149 * t1851 + t1852 * t2522 + t2903) * t3440;
  t242 = t1928 + t1951;
  t2046 = t2070 * t1852;
  t447 = t3481 - 0.50000000000000000000e0 * t2046 + 0.50000000000000000000e0 * t3269;
  t1899 = ((-t3100 * t3194 - 0.1e1 * t1380 * t3211 * t1854 + (t3281 + (t1736 - 0.1e1 * t2594) * t1854 - 0.1e1 * t2522 + t1648) * t3191 + ((-0.1e1 * t1302 * t1861 + t3701 + t3600) * t1853 + (t2357 - 0.1e1 * t2378) * t1861 + (t1449 + t1617 - 0.1e1 * t2530) * t1854) * t1862) * t1852 + (-t3162 * t828 + t3192 * t830) * t1853 + ((t1991 * t3165 - t3273) * t1861 + (t3137 + t3267) * t1854 + t3273) * t1859 - t828 * t3191) * t3443 + ((-t3099 - t3535) * t1853 + t830 * t1861 - t3100 * t3167) * t2940 - (t1861 * t3100 + t3167 * t830) * t3170 / 0.2e1 + t828 * t1853 * t2916;
  t1904 = t2272 + t1860 * t2268 + ((t1854 * t2731 + t1473) * t1860 - t1032 * t2846 - t1508) * t2929 + ((t1854 * t2732 - t2374) * t1860 - t1031 * t2846 + t1507) * t2943 + (((-t1852 * t917 - t2731 * t3162) * t1860 - t772 * t1852 + t1361 * t3174 + t2731 * t3194) * t1858 + ((-t1852 * t915 - t2732 * t3162) * t1860 - t771 * t1852 + t1360 * t3174 + t2732 * t3194) * t1851 + t2270 + ((-t2446 + t2712) * t1858 + (t2445 - t2711) * t1851 + t3512) * t1859) * t3442;
  t57 = t1899 + t1904;
  t815 = -t2607 + 0.27521467987200000000e-3 * t1858 + (0.50000000000000000000e0 * t1385 + t2516) * t1851;
  t1914 = (((t2567 + 0.3127439544e-2 * t3300) * t1858 + (-t2568 - 0.7735484874e-2 * t3300) * t1851) * t1852 + ((0.68072266891200000000e-3 * t1853 + t2162) * t1858 + (0.27521467987200000000e-3 * t1853 + t2161) * t1851 + t2565) * t1859) * t3437 + (((0.16724826617837780000e-2 * t1852 + 0.68072266891200000000e-3 * t1859) * t3166 - t925 * t2846 + t1854 * t2505) * t1858 + ((-0.54835910640823200000e-3 * t1852 + 0.27521467987200000000e-3 * t1859) * t3166 - t923 * t2846 - t1854 * t2506) * t1851 + t1859 * t2351 - t1852 * t2553) * t3444;
  t1919 = (((t1302 * t1853 - t3268) * t1861 + t3599 * t1853) * t1852 + t3166 * t3575 + t828 * t3163 + ((-t1853 * t1736 - 0.1e1 * t1449 - 0.1e1 * t1617 + t3256 + t2530) * t1852 - t3269) * t1854) * t3445 + (-t3100 * t3204 + (t1853 * t830 + t2088 + t2908) * t1859 + (t1852 * t2173 - t828) * t1860) * t3438;
  t90 = t1914 + t1919;
  t2071 = -t167 * t1869 - t1866 * t815 - t1867 * t447 - t1868 * t242 + t1870 * t90 + t1871 * t57;
  t109 = t207 * t1861 + t451 * t1860 + t866 * t1854 - t2566 + 0.2438248419014880000e-3 + (t1150 * t3220 + t1859 * t501 + t1700) * t1853;
  t184 = t632 * t1861 + t1278 * t1859 + t822 * t1840 + t967 * t1854 + 0.2444829139027696e-2 + t3430;
  t1967 = t281 * t1861 + t340 * t1860 + t518 * t1859 - 0.26594038206575168000e-1 + (t1846 * t625 + t823) * t1854 + t3468 * t1853;
  t67 = 0.72089127222315021200e0 + t255 * t1847 + t155 * t1861 + t351 * t1860 + t894 * t1859 + t727 * t1854 + t3397 + t1065;
  t95 = -0.45771590927182000000e0 + t194 * t1847 + t250 * t1861 + t758 + t3052 + 0.17727845388000000000e0 * t1854 + t3611;
  t2010 = t2930 * (-0.1e1 * t67 * t1855 + t1967 * t1862) + t3456 * (-0.1e1 * t1841 + t1848) * t109 + ((-0.2e1 * t184 + 0.18097031967769686000e-1) * t3451 + t3439 * (0.2e1 * t859 - 0.2e1 * t1056 - 0.62953564459500000000e-1) + t3440 * (0.2e1 * t3312 + 0.10875022106691880000e-1 - 0.2e1 * t3375) * t1853 + t3446 * (0.2e1 * t1085 - 0.21326866492899000000e0) - 0.2e1 * t3456 * t95) * t3189;
  t1865 = q_state_dot(7);
  t1261 = t1538 * t3157;
  t1159 = 0.17515226323752810800e0 + t3102;
  t692 = t745 * t1847 + 0.90485159838848430000e-2;
  t448 = -t3269 / 0.2e1 + t2046 / 0.2e1 + t3481;
  t408 = -t1855 * t606 + t3394;
  t243 = -t1928 + t1951;
  t209 = t3061 + (t3461 + t3504) * t1860 + t1931;
  t178 = t1958 - t2045;
  t168 = t1933 + t1949;
  t134 = t1925 + t1927;
  t104 = t1940 + t1948;
  t102 = t2016 + (t3061 - t2245) * t1861 + t1926;
  t94 = t1937 + t3479;
  t89 = t1914 - t1919;
  t73 = t1934 - t1944;
  t71 = t1915 + t1917;
  t65 = -t1921 + t1941;
  t61 = t1898 + t1922;
  t59 = -0.74825343006513819400e0 + t184 * t1848 + t204 * t1847 + t251 * t1861 + t435 * t1846 + t432 * t1860 + t961 * t1840 + 0.18916511922000000000e0 * t1854 + 0.90485159838848430000e-2 * t1841 - t3611;
  t56 = -t1899 + t1904;
  t55 = t1908 + t1920;
  t53 = t95 * t1848 + t109 * t3189 + t895 * t1861 + 0.20151179342388081600e0 + (t1860 * t898 + t960) * t1854 + t3359;
  t52 = t1894 + t1896;
  t49 = -t1916 + t1923;
  t47 = -0.79667177678710400000e-2 + t67 * t1862 + t1967 * t1855;
  t46 = t1905 + t1907;
  t44 = -t1903 + t1929;
  t41 = t1893 + t1897;
  t39 = t1909 + t1913;
  t37 = t1901 + t1910;
  t34 = -t1895 + t1947;
  t32 = -t1890 + t1912;
  t31 = -t1902 + t1932;
  t26 = -t1886 + t1900;
  t22 = (t1397 * t1859 - t1079 + t1159 + t433 - t692) * t3189 + t2010;
  t19 = t1885 + t1892;
  t15 = -t1881 + t1924;
  t13 = (t3451 - t1842 / 0.2e1) * t47 + (t53 - t59) * t3182;
  t11 = t1911 - t1879;
  t10 = t1884 + t1906;
  t8 = t1887 + t1918;
  t5 = -t1880 + t1891;
  t4 = t1888 + t1889;
  t2 = t1882 - t1883;
  C(6,1) = t16 * t1869 - t1865 * t57 - t1867 * t43 - t1868 * t36 - t1870 * t9 - t3432;
  C(4,3) = t101 * t1865 + t1866 * t93 - t1867 * t74 - t2323;
  C(4,5) = t178 * t1866 + t209 * t1865 + t2202 + (-t1853 * t2091 + t1860 * t424) * t1867;
  C(7,2) = t1866 * t90 - t1867 * t70 - t1868 * t60 - t1869 * t45 - t2680;
  C(1,5) = t52 * t1865 + t44 * t1866 + (((t2957 + t3191) * t3222 + (-t1853 * t369 + (t3195 * t800 + t459) * t1860) * t1859 - t2077 * t1853 + t600 * t3169 + t2008 * t1860) * t1856 - t1863 * t1154 * t3014 + (t1185 * t3167 - t1853 * t434) * t3170 - t2166 * t3200 - t2965 * t3698 + t2057 * t3164) * t1867 + t32 * t1868 + t11 * t1869 + t8 * t1870 + t3433;
  C(5,3) = t103 * t1866 + t133 * t1865 + t1868 * t74 - t2302;
  C(2,6) = t89 * t1865 + (((t2291 * t1861 - 0.1e1 * t3296 + t2058) * t1859 - 0.1e1 * t1974 * t1852) * t1862 + (t1980 * t1859 - 0.1e1 * t2015 * t1852) * t1855 + (-0.1e1 * t3649 * t3206 + (t2093 * t1859 - 0.1e1 * t2215) * t1855) * t1854) * t1866 + t65 * t1867 + t55 * t1868 + t39 * t1869 + t2718;
  C(1,3) = t26 * t1865 + t15 * t1866 + t11 * t1867 + t5 * t1868 + ((-t1857 * t520 + t3153 * t519) * t2632 + (t3741 - t3745) * t2626 + (-t3178 * t577 + t3742) * t2630 + (t1864 * t384 - t3178 * t383) * t2636 + (-t1857 * t376 + t3153 * t377) * t2642 + (t1863 * t2734 + t1864 * t408) * t2638 + (t3153 * t408 + t2734) * t2634 + ((-t3159 * t989 + t1261) * t1857 + (t1370 + t3368) * t1864) * t2619 + (t1857 * t2660 + t3153 * t760) * t2624 + ((-t1104 * t3159 + t1261) * t1864 - t2328) * t2616 + (-t1863 * t2328 + t2326) * t2621 + (t1864 * t540 - t3178 * t541) * t2628 + ((-t1863 * t2349 + t2359) * t1854 + t2421) * t2623 + ((t1863 * t2694 - t1864 * t2835) * t1854 + t2422) * t2618 + t2417 * t2825 + (t1134 * t3178 + t1049) * t2828 + (-t1855 * t2154 + t1862 * t2155) * t2824 + (-0.1e1 * t1253 * t1864 + t2087) * t2613 + (t1863 * t2087 - t1372) * t2615 + (-t1863 * t3236 + t3115) * t2823 + ((0.1e1 * t3737 + (-0.1e1 * t699 * t2986 + t1977 * t1862) * t1860 - 0.1e1 * t562 * t3193 + t1040 * t2778 - 0.86410e-2 * t1862 + (-0.1e1 * t2523 + t3493) * t3201) * t1861 + t2787 + t3738 + t701 * t3197 - 0.1e1 * t1144 * t2979 + t1852 * t2605 * t3194 - 0.12805000000000000000e-1 * t1862 + (-0.1e1 * t370 * t1847 + (t3333 - 0.1e1 * t1387 + t2186) * t1860 - 0.1e1 * t2376 * t3212 - 0.1e1 * t1191) * t1855) * t1856) * t1869 + t2 * t1870 + t22 * t1871;
  C(5,2) = t1865 * t70 + t1866 * t64 + t1868 * t50 + t1869 * t35 - t2719;
  C(4,6) = t243 * t1865 + ((t1859 * t2283 + t1699) * t1860 + (-0.1e1 * t3698 + t3548) * t1853 + t2809) * t1866 + t178 * t1867 + t2201;
  C(1,1) = t13 * t1870 + t1865 * t28 + t1866 * t25 + t1867 * t23 + t1868 * t21 + t1869 * t22;
  C(7,3) = -t101 * t1868 - t133 * t1867 - t167 * t1866 - t2304;
  C(7,6) = t2071;
  C(5,7) = (-t3097 * t1852 + (0.680722668912e-3 * t1851 - 0.275214679872e-3 * t1858) * t1859) * t1865 + t448 * t1866 + t2139;
  C(6,3) = -t103 * t1867 + t167 * t1865 - t1868 * t93 - t2316;
  C(3,5) = t104 * t1866 + t134 * t1865 + t73 * t1868 + t2302 + ((-0.1e1 * t1154 * t3221 - 0.1e1 * t637 * t3202 + t3523 * t1853 - t3694) * t1854 - 0.1e1 * t821 * t3202 - 0.1e1 * (t2458 + t3247) * t1853 + t2288 * t3166 + ((t3490 + t3548) * t1854 + t3492) * t1860) * t1867;
  C(2,4) = t61 * t1865 + t55 * t1866 + t49 * t1867 + (((-0.1e1 * t3725 + t3480) * t3217 + (-t1854 * t3482 + t1861 * t3707 - t3315) * t1860 + (-t1852 * t2486 + t1859 * t481 + t1018 - t1075 + t3248) * t1853 - t3066 - t976 * t1854 + 0.1644487577369270e-2 * t1861) * t1855 + ((t1070 - t1087) * t1859 + t3248 - t1852 * t2487 + t1776) * t3165 + (-0.1e1 * t1146 * t3199 - 0.1e1 * t1305 * t1859 - 0.1e1 * t3466 * t1854 + (t2313 - t3304) * t1861) * t1862) * t1868 + t31 * t1869 + t2720;
  C(1,7) = ((-0.1e1 * (t1244 * t1861 + t1860 * t2453 + t3392) * t1851 + (t915 * t3173 + t3393 - 0.1e1 * t1361 * t3163) * t1858 + (-0.1e1 * (-t1860 * t2645 - t1473) * t1851 + (t1860 * t2072 + t2374) * t1858) * t1862 + (t2357 + (-0.1e1 * (-t2713 + t2751) * t1851 + (-t2714 + t2752) * t1858) * t1853 + (-0.1e1 * (-0.988270895904e-3 * t1854 - t2226) * t1851 + (0.2444413220184e-2 * t1854 + t2225) * t1858) * t1852) * t1855) * t1856 - t1945 * t3210 + t1946 * t3175) * t1865 + t56 * t1866 + t52 * t1867 + t41 * t1868 + t26 * t1869 + t19 * t1870 + t3431;
  C(1,6) = t56 * t1865 + ((-t1852 * t1957 + t1859 * t1942 - t2144 * t3204) * t1856 + t1982 * t3170 - t3200 * t3310 - t1984 * t3205) * t1866 + t44 * t1867 + t37 * t1868 + t15 * t1869 + t10 * t1870 + t3432;
  C(6,6) = t815 * t1865;
  C(3,4) = t102 * t1865 + t94 * t1866 + t73 * t1867 + ((t2208 * t1853 + t603 - 0.1e1 * t1146 * t1860 + 0.66241105529490700000e-2 - t3708) * t1861 + (-0.1e1 * t424 * t1853 - 0.1e1 * t2091 * t1860 + 0.1644487577369270e-2) * t1854) * t1868 + t2323;
  C(2,3) = t46 * t1865 + t39 * t1866 + t34 * t1867 + t31 * t1868 + ((-0.36044563611157510600e0 + t257 * t1847 + t156 * t1861 + t2064 * t1860 + t905 * t1859 + t726 * t1854 + t677 * t1852 - t1160 * t1853) * t1862 - t283 * t3190 - t642 * t3010 - t2017 * t3191 - t516 * t3192 - t842 * t3193 + t2545 * t3204 - t1853 * t2547 + 0.13297019103287584000e-1 * t1855) * t1869 + t2723;
  C(7,4) = -t1866 * t242 - t1867 * t208 - t2193;
  C(3,7) = (((-t3097 * t1859 + (t2748 - t2749) * t1794) * t1860 + t1306 * t2366 + t1851 * t2568 - t1853 * t1732) * t1854 + t1792 * t1860 * t2159 + (-t1851 * t2657 + t1858 * t2658) * t1859 + t1851 * t2371 + t1858 * t2372) * t1865 + t168 * t1866 + t134 * t1867 + t102 * t1868 + t2304;
  C(5,5) = t1865 * t494 - t1866 * t431;
  C(3,1) = -0.1e1 * t27 * t1865 - 0.1e1 * t16 * t1866 - 0.1e1 * t12 * t1867 - 0.1e1 * t6 * t1868 + t1 * t1870 + ((t1854 * t2694 + (-0.1e1 * t1854 * t2688 + t2085) * t1864 + t2421) * t2618 + t1855 * t2958 + (t1864 * t519 - 0.1e1 * t3178 * t520) * t2632 + (t1864 * t377 - 0.1e1 * t3178 * t376) * t2642 + (t1864 * t760 + t2660 * t3178) * t2624 + t2417 * t2828 + (-0.1e1 * t3745 + t3741) * t2630 + (t1857 * t2659 + t1864 * t539) * t2619 - 0.1e1 * t1397 * t2977 + (-0.1e1 * t1857 * t282 + t3426) * t2634 + (-0.1e1 * t409 * t1857 + t1863 * t3426) * t2638 - 0.1e1 * t2010 + (-0.1e1 * t2328 + t1863 * t2326) * t2621 + ((t1863 * t2359 - 0.1e1 * t2349) * t1854 + t2422) * t2623 + (-0.1e1 * t1857 * t541 + t1864 * t390) * t2628 + (-0.1e1 * t3560 - 0.1e1 * t2086) * t2613 + (-0.1e1 * t1857 * t571 + t2326) * t2616 + t3675 * t2823 + (-0.1e1 * t1857 * t2816 + t1049) * t2825 + (-0.1e1 * t1857 * t383 + t1864 * t254) * t2636 + (-0.1e1 * t1863 * t2086 + t3231) * t2615 + (-0.1e1 * t1857 * t407 + t3742) * t2626 + (t3115 + t3141) * t2824 + (t692 - 0.1e1 * t433 - 0.1e1 * t1159) * t3189) * t1871;
  C(2,1) = t18 * t1865 + t9 * t1866 + t7 * t1867 + t3 * t1868 - 0.1e1 * t1 * t1869 + (-0.1e1 * t3675 * t2677 + t2824 * t937 - 0.1e1 * (t3711 - 0.1e1 * t3338) * t2686 - 0.1e1 * t595 * t2686 + (-0.50000000000000000000e0 * t1849 + t3456) * t47 + (-0.1e1 * t53 + t59) * t3182 + (0.1e1 * t1857 * t550 - 0.1e1 * t3405 + 0.1e1 * t404) * t604 * t2797 + (-0.1e1 * t1864 * t591 + 0.1e1 * t3411 - 0.1e1 * t394) * t3746 + (-0.1e1 * t297 - 0.1e1 * t1857 * t421 + t3406) * t414 * t2796 + (t1864 * t422 - 0.1e1 * t3412 + t294) * t2687 + (-0.1e1 * t1588 + t715 + t2666 * t3156 + (-0.1e1 * t1856 * t2851 - 0.1e1 * t1863 * t2733) * t1857 - 0.1e1 * t169) * t2407 + ((-0.1e1 * t3661 + (-0.1e1 * t3408 - 0.1e1 * t879 + 0.825e-1) * t1855) * t1857 + (t1856 * t2852 + t1863 * t2251) * t1864 + t181) * t2400 - 0.1e1 * (-0.1e1 * (-0.1e1 * t3560 - 0.1e1 * t1372) * t2534 - 0.1e1 * t3675 * t2468) * t3585 + (-0.1e1 * t3712 - 0.1e1 * t1049 + t615) * t868 * t2795) * t1871;
  C(7,7) = 0.0e0;
  C(4,4) = t1865 * t253 + t1866 * t220 + t1867 * t198;
  C(6,5) = t1865 * t447 - t2140;
  C(7,1) = -t18 * t1870 + t1866 * t57 - t1867 * t51 - t1868 * t40 + t1869 * t27 - t3431;
  C(2,7) = ((-t1851 * t1959 + t1858 * t1960) * t1855 + ((-0.1e1 * t2178 * t1851 + t2177 * t1858) * t1860 + (-0.1e1 * t2163 * t1851 + t2164 * t1858) * t1853 + (-0.1e1 * t2162 * t1851 + t2161 * t1858) * t1852) * t1862) * t1865 + t89 * t1866 + t71 * t1867 + t61 * t1868 + t46 * t1869 + t2680;
  C(6,7) = -t1865 * t3100 - t2071;
  C(3,3) = t100 * t1865 + t105 * t1867 + t1866 * t97 + t1868 * t68;
  C(4,7) = (t2131 * t1860 + (t1525 * t2159 - t1859 * t2590 - t2354) * t1853 + t3505 * (t1860 * t2420 + 0.825e-1 * t1852)) * t1865 + t243 * t1866 + t209 * t1867 + t2193;
  C(1,4) = t41 * t1865 + t37 * t1866 + t32 * t1867 + ((0.1e1 * t633 * t3009 + ((t1859 * t737 + t2153) * t1861 + (t1145 * t3192 + t1488 - 0.1e1 * t1720 + ((-0.1e1 * t3391 + t2722) * t1853 - 0.1e1 * t1146) * t1862) * t1854) * t1860 + (-0.1e1 * t958 + (-0.1e1 * t2288 * t1854 + t2310 * t1861) * t1855 + ((-0.1e1 * t1070 + t614) * t1859 - 0.1e1 * t3248 + t3523 * t1861) * t1862) * t1853 + (-0.1e1 * t750 * t1854 - 0.1e1 * t2363) * t1859 - 0.1e1 * t2069 * t1854 + t2059 * t1861) * t1856 + (t2789 * t1861 + (-0.1e1 * t1089 + t3702 - t1160) * t1854) * t3164 + (-0.1e1 * t3330 * t1859 - t1271 + (-0.1e1 * t2818 - 0.1e1 * t3400) * t1854) * t3200 + t3569 * t3158 + t3497 * t1863) * t1868 + t5 * t1869 + t4 * t1870 + t3434;
  C(2,5) = t71 * t1865 + t65 * t1866 + (((t441 + t2963) * t1860 + (-t1859 * t423 - t1018 - t691) * t1853) * t1855 + ((-t446 + t1089) * t1853 + (t1859 * t430 + t3222 + t702) * t1860) * t1862) * t1867 + t49 * t1868 + t34 * t1869 + t2719;
  C(4,2) = t1865 * t60 + t1866 * t54 - t1867 * t50 - t1869 * t30 - t2720;
  C(5,4) = -t179 * t1866 + t1865 * t208 - t2202;
  C(5,1) = t12 * t1869 + t1865 * t51 + t1866 * t43 + t1868 * t33 - t1870 * t7 - t3433;
  C(6,4) = t179 * t1867 + t1865 * t242 - t2201;
  C(3,6) = t168 * t1865 + (((-t1859 * t3616 + t1699) * t1853 + t3707 * t1860) * t1854 + (t1859 * t2116 - t3247) * t1853 + t2721) * t1866 + t104 * t1867 + t94 * t1868 + t2316;
  C(6,2) = -t1865 * t90 - t1867 * t64 - t1868 * t54 - t1869 * t38 - t2718;
  C(2,2) = t14 * t1869 + t17 * t1868 + t1865 * t29 + t1866 * t24 + t1867 * t20 - t3515 * t3550 + t3550;
  C(5,6) = t448 * t1865 + (-t3696 + t2215) * t1866 + t2140;
  C(7,5) = -t1866 * t447 - t2139;
  C(1,2) = t10 * t1866 + t13 * t1871 + t19 * t1865 + t8 * t1867 + t4 * t1868 + t2 * t1869 + ((-0.1e1 * t1856 * t357 + t2852 * t3178) * t2400 + (-0.1e1 * t1856 * t395 + t2851 * t3153) * t2407 + 0.70400000000000000000e-3 * t1856 - 0.1e1 * t937 * t2677 - 0.1e1 * t285 * t3184 * t3193 + t2975 * t3284 + (-0.15015000000000000000e-1 + t307 * t1861 + t2011 * t1854) * t1863 - 0.1e1 * t1855 * t629 * t3185 + t190 * t1863 * t1848 + (t1863 * t1985 + (-0.1e1 * t3404 + 0.12805000000000000000e-1 + (-0.1e1 * t696 + 0.1e1 * t3072 - 0.1e1 * t3679 + t2373 - 0.1e1 * t1277) * t1854) * t1856) * t1862 + (t2793 * t297 + t2796 * t294) * (-0.1e1 * t1856 * t846 + t3628) + (-0.1e1 * t2318 - 0.1e1 * t3422) * t3186 + (-0.1e1 * t615 * t2791 - 0.1e1 * t595 * t2795) * t2816 + (t169 * t2472 + t181 * t2538) * (-0.1e1 * t1856 * t449 + t1863 * t2252) + (t767 * t2792 - 0.1e1 * t3675 * t2534) * t3583 + 0.22610063700000000000e-2 * t3515 * t1545 + ((t2910 + 0.1e1 * t3721 - 0.1e1 * t1834) * t2687 + (-0.1e1 * t1226 + 0.1e1 * t3117 - 0.1e1 * t3413 + t787 * t3747 - 0.1e1 * t2298) * t3746 + t3585 ^ 2 * t2468 + (-0.1e1 * t2837 * t1863 + 0.1e1 * t1552) * t2686) * t1857 + (-0.1e1 * t404 * t2794 - 0.1e1 * t394 * t2797) * (t1101 * t3747 + t820)) * t1870;
  C(4,1) = t1865 * t40 + t1866 * t36 - t1867 * t33 + t1869 * t6 - t1870 * t3 - t3434;
  C(3,2) = t1865 * t45 + t1866 * t38 - t1867 * t35 + t1868 * t30 - t2723;
end
